simulink model "finalmodel1"  (R2024b)
(part 4 of 9)

ITS220Fyz2 | Innotech Solar ITS220Myz2 | Innotech Solar ITS220Nyz2 | Innotech Solar ITS215XXXX | Innotech Solar ITS220Eyz3 | Innotech Solar ITS220Fyz3 | Innotech Solar ITS220Myz3 | Innotech Solar ITS220Nyz3 | Innotech Solar x220 | Innotech Solar ITS225XXXX | Innotech Solar x225 | Innotech Solar ITS220Eyz4 | Innotech Solar ITS220Fyz4 | Innotech Solar ITS220Mxy4 | Innotech Solar ITS220Nxy4 | Innotech Solar ITS230XXXX | Innotech Solar x230 | Innotech Solar x235 | Innotech Solar x240 | Innotech Solar x245 | Innotech Solar ITS270Eyz1 | Innotech Solar ITS270Fyz1 | Innotech Solar ITS270Myz1 | Innotech Solar ITS270Nyz1 | Innotech Solar x250 | Innotech Solar x255 | Innotech Solar ITS270Eyz2 | Innotech Solar ITS270Fyz2 | Innotech Solar ITS270Myz2 | Innotech Solar ITS270Nyz2 | Innotech Solar x260 | Innotech Solar x265 | Innotech Solar ITS270Eyz3 | Innotech Solar ITS270Fyz3 | Innotech Solar ITS270Myz3 | Innotech Solar ITS270Nyz3 | Innovosolar International TEM165M | Innovosolar International TEM170M | Innovosolar International TEM175M | Innovosolar International TEM180M | Instalaciones Pevafersa IP-VA180 | Instalaciones Pevafersa IP-VAP210 | Instalaciones Pevafersa IP-220 GG | Instalaciones Pevafersa IP-225 GG | Instalaciones Pevafersa IP-230 GG | Instalaciones Pevafersa IP-VAP230 | Instalaciones Pevafersa IP-235 GG | Integrated Power IPC175M01 | Integrated Power IPC175M01-US | Integrated Power IPC175P01 | Integrated Power IPC175P01-US | Integrated Power IPC180M01 | Integrated Power IPC180M01-US | Integrated Power IPC180P01 | Integrated Power IPC180P01-US | Integrated Power IPC185M01 | Integrated Power IPC185M01-US | Integrated Power IPC185P01 | Integrated Power IPC185P01-US | Integrated Power IPC190P01 | Integrated Power IPC190P01-US | Integrated Power IPC200P01 | Integrated Power IPC200P01-US | Integrated Power IPC205P01 | Integrated Power IPC205P01-US | Integrated Power IPC210P01 | Integrated Power IPC210P01-US | Integrated Power IPC215P01 | Integrated Power IPC215P01-US | Integrated Power IPC220P01 | Integrated Power IPC220P01-US | Integrated Power IPC225P01 | Integrated Power IPC225P01-US | Integrated Power IPC230P01 | Integrated Power IPC230P01-US | Integrated Power IPC235P01 | Integrated Power IPC235P01-US | Integrated Power IPC240P01 | Integrated Power IPC240P01-US | Integrated Power IPC245P01 | Integrated Power IPC245P01-US | Integrated Power IPC250P01 | Integrated Power IPC250P01-US | Integrated Power IPC255P01 | Integrated Power IPC255P01-US | Integrated Power IPC260P01 | Integrated Power IPC260P01-US | Integrated Power IPC265P01 | Integrated Power IPC265P01-US | Integrated Power IPC270P01 | Integrated Power IPC270P01-US | Integrated Power IPC275P01 | Integrated Power IPC275P01-US | Integrated Power IPC280P01 | Integrated Power IPC280P01-US | Integrated Solar Technology STT-64M-B4U | Integrated Solar Technology STT-67M-B4U | Integrated Solar Technology STT-70M-B4U | Integrated Solar Technology STS-95M-B4U | Integrated Solar Technology STS-100M-B4U | Integrated Solar Technology STS-105M-B4U | Inventec Energy IECS-6P66-125 | Inventec Energy IECS-6M66-130 | Inventec Energy IECS-6P66-130 | Inventec Energy IECS-6M66-135 | Inventec Energy IECS-6P66-135 | Inventec Energy IECS-6M66-140 | Inventec Energy IECS-6P66-140 | Inventec Energy IECS-6M66-145 | Inventec Energy IECS-6P66-145 | Inventec Energy IECS-6P67-145 | Inventec Energy IECS-6M66-150 | Inventec Energy IECS-6M67-150 | Inventec Energy IECS-6P67-150 | Inventec Energy IECS-6M67-155 | Inventec Energy IECS-6P67-155 | Inventec Energy IECS-6M67-160 | Inventec Energy IECS-6P67-160 | Inventec Energy IECS-6M67-165 | Inventec Energy IECS-6P67-165 | Inventec Energy IECS-6P68-165 | Inventec Energy IECS-6M67-170 | Inventec Energy IECS-6M68-170 | Inventec Energy IECS-6P67-170 | Inventec Energy IECS-6P68-170 | Inventec Energy IECS-6M67-175 | Inventec Energy IECS-6M68-175 | Inventec Energy IECS-6P67-175 | Inventec Energy IECS-6P68-175 | Inventec Energy IECS-6M68-180 | Inventec Energy IECS-6M68-185 | Inventec Energy IECS-6P68-185 | Inventec Energy IECS-6M68-190 | Inventec Energy IECS-6P68-190 | Inventec Energy IECS-6P69-190 | Inventec Energy IECS-6M68-195 | Inventec Energy IECS-6P68-195 | Inventec Energy IECS-6P69-195 | Inventec Energy IECS-6M69-200 | Inventec Energy IECS-6P68-200 | Inventec Energy IECS-6P69-200 | Inventec Energy IECS-6M69-205 | Inventec Energy IECS-6P68-205 | Inventec Energy IECS-6P69-205 | Inventec Energy IECS-6M69-210 | Inventec Energy IECS-6P69-210 | Inventec Energy IECS-6P6A-210 | Inventec Energy IECS-6M6A-215 | Inventec Energy IECS-6P69-215 | Inventec Energy IECS-6P6A-215 | Inventec Energy IECS-6M6A-220 | Inventec Energy IECS-6P69-220 | Inventec Energy IECS-6P6A-220 | Inventec Energy IECS-6M6A-225 | Inventec Energy IECS-6P69-225 | Inventec Energy IECS-6P6A-225 | Inventec Energy IECS-6M6A-230 | Inventec Energy IECS-6P69-230 | Inventec Energy IECS-6P6A-230 | Inventec Energy IECS-6M6A-235 | Inventec Energy IECS-6P6A-235 | Inventec Energy IECS-6M6A-240 | Inventec Energy IECS-6P6A-240 | Inventec Energy IECS-6M6A-245 | Inventec Energy IECS-6P6A-245 | Inventec Energy IECS-6M6A-250 | Inventec Energy IECS-6P6A-250 | Inventec Energy IECS-6M6A-255 | Inventec Energy IECS-6P6A-255 | Inventec Energy IECS-6M6A-260 | Inventec Energy IECS-6M6A-265 | Inventec Energy IECS-6M6A-270 | Inventec Energy IECS-6M6A-275 | Inventec Energy IECS-6P6C-275 | Inventec Energy IECS-6P6C-280 | Inventec Energy IECS-6M6C-285 | Inventec Energy IECS-6P6C-285 | Inventec Energy IECS-6M6C-290 | Inventec Energy IECS-6P6C-290 | Inventec Energy IECS-6M6C-295 | Inventec Energy IECS-6P6C-295 | Inventec Energy IECS-6M6C-300 | Inventec Energy IECS-6P6C-300 | Inventec Energy IECS-6M6C-305 | Inventec Energy IECS-6M6C-310 | Inventec Energy IECS-6M6C-315 | Inventec Energy IECS-6M6C-320 | Inventec Energy IECS-6M6C-325 | Inventec Energy IECS-6M6C-330 | Isofoton IS-210/32 | Isofoton IS-215/32 | Isofoton IS-220/32 | Isofoton ISF-235 | Isofoton ISF-240 | Isofoton ISFP-240 Black | Isofoton ISFP-240 White | Isofoton ISF-245 | Isofoton ISF-245 Black | Isofoton ISF-245 Clear | Isofoton ISFP-245 Black | Isofoton ISFP-245 White | Isofoton ISFT-245 | Isofoton ISF-250 | Isofoton ISF-250 Black | Isofoton ISF-250 Clear | Isofoton ISFP-250 Black | Isofoton ISFP-250 White | Isofoton ISFT-250 | Isofoton ISF-255 | Isofoton ISF-255 Black | Isofoton ISF-255 Clear | Isofoton ISFP-255 Black | Isofoton ISFP-255 White | Isofoton ISFT-255 | Isofoton ISFP-260 Black | Isofoton ISFP-260 White | Isofoton ISFP-265 Black | Isofoton ISFP-265 White | Isofoton ISFP-270 Black | Isofoton ISFP-270 White | Itek Energy LLC iT-220 | Itek Energy LLC iT-225 | Itek Energy LLC iT-230 | Itek Energy LLC iT-235 | Itek Energy LLC iT-240 | Itek Energy LLC P18y250 | Itek Energy LLC S18y250 | Itek Energy LLC P18y255 | Itek Energy LLC S18y255 | Itek Energy LLC iT-260-HE | Itek Energy LLC P18y260 | Itek Energy LLC S18y260 | Itek Energy LLC iT-265-HE | Itek Energy LLC P18Y265 | Itek Energy LLC S18y265 | Itek Energy LLC iT-270-HE | Itek Energy LLC S19Y270 | Itek Energy LLC S79y270 | Itek Energy LLC iT-275-HE | Itek Energy LLC iT-275-SE | Itek Energy LLC P19Y275 | Itek Energy LLC S19y275 | Itek Energy LLC S79y275 | Itek Energy LLC iT-280-HE | Itek Energy LLC iT-280-SE | Itek Energy LLC S19y280 | Itek Energy LLC S59y280 | Itek Energy LLC S79y280 | Itek Energy LLC iT-285-HE | Itek Energy LLC iT-285-SE | Itek Energy LLC P19Y285 | Itek Energy LLC S19y285 | Itek Energy LLC S59y285 | Itek Energy LLC S79y285 | Itek Energy LLC iT-290-HE | Itek Energy LLC iT-290-SE | Itek Energy LLC P19Y290 | Itek Energy LLC S19y290 | Itek Energy LLC S59y290 | Itek Energy LLC S79Y290 | Itek Energy LLC iT-295-HE | Itek Energy LLC iT-295-SE | Itek Energy LLC P19Y295 | Itek Energy LLC S19Y295 | Itek Energy LLC S59Y295 | Itek Energy LLC S79Y295 | Itek Energy LLC iT-300-HE | Itek Energy LLC iT-300-SE | Itek Energy LLC P19Y300 | Itek Energy LLC S19Y300 | Itek Energy LLC S59Y300 | Itek Energy LLC S79Y300 | Itek Energy LLC iT-305-SE | Itek Energy LLC P19Y305 | Itek Energy LLC S19Y305 | Itek Energy LLC S59Y305 | Itek Energy LLC S79Y305 | Itek Energy LLC P19Y310 | Itek Energy LLC S19Y310 | Itek Energy LLC S59Y310 | Itek Energy LLC iT-335-SE-72 | Itek Energy LLC iT-340-SE-72 | Itek Energy LLC iT-345-SE-72 | Itek Energy LLC iT-350-SE-72 | Itek Energy LLC iT-355-SE-72 | Itek Energy LLC iT-360-SE-72 | Itek Energy LLC iT-365-SE-72 | Itek Energy LLC iT-370-SE-72 | Itek Energy LLC iT-375-SE-72 | JA Solar JAM5-72-165 | JA Solar JAM5-72-170 | JA Solar JAM5-72-175 | JA Solar JAM5(L)(BK)-72-180/SI | JA Solar JAM5(L)-72-180/SI | JA Solar JAM5-72-180 | JA Solar JAM5(L)(BK)-72-185/SI | JA Solar JAM5(L)-72-185/SI | JA Solar JAM5-72-185 | JA Solar JAM5(L)(BK)-72-190/SI | JA Solar JAM5(L)-72-190/SI | JA Solar JAM5-72-190 | JA Solar JAM5(L)(BK)-72-195/SI | JA Solar JAM5(L)-72-195/SI | JA Solar JAM5-72-195 | JA Solar JAM5(L)(BK)-72-200/SI | JA Solar JAM5(L)-72-200/SI | JA Solar JAM6-60-200 | JA Solar JAP6-60-200 | JA Solar JAM5(L)(BK)-72-205/SI | JA Solar JAM5(L)-72-205/SI | JA Solar JAM6-60-205 | JA Solar JAP6-60-205 | JA Solar JAM5(L)(BK)-72-210/SI | JA Solar JAM5(L)-72-210/SI | JA Solar JAM6-60-210 | JA Solar JAP6-60-210 | JA Solar JAM6-60-215 | JA Solar JAP6(BK)-60-215 | JA Solar JAM6-60-220 | JA Solar JAP6(BK)-60-220 | JA Solar JAM6-60-225 | JA Solar JAP6(BK)-60-225 | JA Solar JAP6-60-225/MP | JA Solar JAM6-60-230 | JA Solar JAP6(BK)-60-230 | JA Solar JAP6-60-230/MP | JA Solar JAM6-60-235 | JA Solar JAM6-60-235/SI | JA Solar JAP6(BK)-60-235 | JA Solar JAP6-60-235/MP | JA Solar JAM6-60-240 | JA Solar JAM6-60-240/SI | JA Solar JAP6(BK)-60-240 | JA Solar JAP6-60-240/MP | JA Solar JAM6-60-245/SI | JA Solar JAP6(BK)-60-245 | JA Solar JAP6-60-245 | JA Solar JAP6-60-245/3BB | JA Solar JAP6-60-245/MP | JA Solar JAM6-60-250/SI | JA Solar JAP6(BK)-60-250 | JA Solar JAP6-60-250 | JA Solar JAP6-60-250/3BB | JA Solar JAP6-60-250/MP | JA Solar JAP6-72-250 | JA Solar JAM6-60-255/SI | JA Solar JAM6-72-255 | JA Solar JAP6(k)-60-255/4BB | JA Solar JAP6-60-255/3BB | JA Solar JAP6-60-255/4BB | JA Solar JAP6-60-255/MP | JA Solar JAP6-72-255 | JA Solar JAM6-60-260/SI | JA Solar JAM6-72-260 | JA Solar JAP6(k)-60-260/4BB | JA Solar JAP6-60-260/3BB | JA Solar JAP6-60-260/4BB | JA Solar JAP6-60-260/4BB/RE | JA Solar JAP6-60-260/MP | JA Solar JAP6-72-260 | JA Solar JAM6(k)-60-265/4BB | JA Solar JAM6-60-265/SI | JA Solar JAM6-72-265 | JA Solar JAP6(BK)-72-265 | JA Solar JAP6(k)-60-265/4BB | JA Solar JAP6-60-265/3BB | JA Solar JAP6-60-265/4BB | JA Solar JAP6-60-265/4BB/RE | JA Solar JAM6(k)-60-270/4BB | JA Solar JAM6-60-270/SI | JA Solar JAM6-72-270 | JA Solar JAP6(BK)-72-270 | JA Solar JAP6(k)-60-270/4BB | JA Solar JAP6-60-270/3BB | JA Solar JAP6-60-270/4BB | JA Solar JAP6-60-270/4BB/RE | JA Solar JAM6(k)-60-275/4BB | JA Solar JAM6-60-275/SI | JA Solar JAM6-72-275 | JA Solar JAP6(BK)-72-275 | JA Solar JAP6(k)-60-275/4BB | JA Solar JAP6-60-275/3BB | JA Solar JAP6-60-275/4BB | JA Solar JAP6-60-275/4BB/RE | JA Solar JAP6-72-275/3BB | JA Solar JAM6(k)(BK)-60-280/PR | JA Solar JAM6(k)-60-280/4BB | JA Solar JAM6(k)-60-280/PR | JA Solar JAM60S01-280/PR | JA Solar JAM60S02-280/PR | JA Solar JAM6-60-280/SI | JA Solar JAM6-72-280 | JA Solar JAP6(BK)-72-280 | JA Solar JAP6(BK)-72-280/MP | JA Solar JAP6-60-280/4BB/RE | JA Solar JAP6-72-280/3BB | JA Solar JAP6-72-280/MP | JA Solar JAM6(BK)-72-285/SI | JA Solar JAM6(k)(BK)-60-285/PR | JA Solar JAM6(k)-60-285/4BB | JA Solar JAM6(k)-60-285/PR | JA Solar JAM60S01-285/PR | JA Solar JAM60S02-285/PR | JA Solar JAM6-72-285 | JA Solar JAM6-72-285/SI | JA Solar JAP6(BK)-72-285 | JA Solar JAP6(BK)-72-285/MP | JA Solar JAP6-72-285/3BB | JA Solar JAP6-72-285/MP | JA Solar JAM6(BK)-72-290/SI | JA Solar JAM6(k)(BK)-60-290/PR | JA Solar JAM6(k)-60-290/PR | JA Solar JAM60S01-290/PR | JA Solar JAM60S02-290/PR | JA Solar JAM6-72-290 | JA Solar JAM6-72-290/SI | JA Solar JAP6(BK)-72-290 | JA Solar JAP6(BK)-72-290/MP | JA Solar JAP6-72-290/3BB | JA Solar JAP6-72-290/MP | JA Solar JAM6(BK)-72-295/SI | JA Solar JAM6(k)(BK)-60-295/PR | JA Solar JAM6(k)-60-295/PR | JA Solar JAM60S01-295/PR | JA Solar JAM6-72-295 | JA Solar JAM6-72-295/SI | JA Solar JAP6(BK)-72-295 | JA Solar JAP6(BK)-72-295/MP | JA Solar JAP6-72-295 | JA Solar JAP6-72-295/3BB | JA Solar JAP6-72-295/MP | JA Solar JAM6(BK)-72-300/SI | JA Solar JAM6(k)(BK)-60-300/PR | JA Solar JAM6(k)-60-300/PR | JA Solar JAM60S01-300/PR | JA Solar JAM60S02-300/PR | JA Solar JAM6-72-300 | JA Solar JAM6-72-300/SI | JA Solar JAP6(BK)-72-300 | JA Solar JAP6(BK)-72-300/MP | JA Solar JAP6-72-300 | JA Solar JAP6-72-300/3BB | JA Solar JAP6-72-300/MP | JA Solar JAM6(BK)-72-305/SI | JA Solar JAM60S01-305/PR | JA Solar JAM6-72-305/SI | JA Solar JAP6(BK)-72-305/MP | JA Solar JAP6(k)-72-305/4BB | JA Solar JAP6-72-305 | JA Solar JAP6-72-305/3BB | JA Solar JAP6-72-305/4BB | JA Solar JAP6-72-305/4BB/RE | JA Solar JAP6-72-305/MP | JA Solar JAP72S01-305/SC | JA Solar JAM6(BK)-72-310/SI | JA Solar JAM6-72-310/SI | JA Solar JAP6(BK)-72-310/MP | JA Solar JAP6(k)-72-310/4BB | JA Solar JAP6-72-310 | JA Solar JAP6-72-310/3BB | JA Solar JAP6-72-310/4BB | JA Solar JAP6-72-310/4BB/RE | JA Solar JAP6-72-310/MP | JA Solar JAP72S01-310/SC | JA Solar JAM6(BK)-72-315/SI | JA Solar JAM6-72-315/SI | JA Solar JAP6(BK)-72-315/MP | JA Solar JAP6(k)-72-315/4BB | JA Solar JAP6-72-315 | JA Solar JAP6-72-315/3BB | JA Solar JAP6-72-315/4BB | JA Solar JAP6-72-315/4BB/RE | JA Solar JAP6-72-315/MP | JA Solar JAP72S01-315/SC | JA Solar JAM6(k)-72-320/4BB | JA Solar JAM6-72-320/SI | JA Solar JAP6(k)-72-320/4BB | JA Solar JAP6-72-320/3BB | JA Solar JAP6-72-320/4BB | JA Solar JAP6-72-320/4BB/RE | JA Solar JAP72S01-320/SC | JA Solar JAM6(k)-72-325/4BB | JA Solar JAM6-72-325/SI | JA Solar JAP6(k)-72-325/4BB | JA Solar JAP6-72-325/3BB | JA Solar JAP6-72-325/4BB | JA Solar JAP6-72-325/4BB/RE | JA Solar JAP72S01-325/SC | JA Solar JAM6(k)-72-330/4BB | JA Solar JAM6(k)-72-330/PR | JA Solar JAM6-72-330/SI | JA Solar JAP6-72-330/3BB | JA Solar JAP6-72-330/4BB | JA Solar JAP6-72-330/4BB/RE | JA Solar JAP72S01-330/SC | JA Solar JAM6(k)-72-335/4BB | JA Solar JAM6(k)-72-335/PR | JA Solar JAM6-72-335/SI | JA Solar JAM72S01-335/PR | JA Solar JAP6-72-335/4BB/RE | JA Solar JAM6(k)-72-340/4BB | JA Solar JAM6(k)-72-340/PR | JA Solar JAM72S01-340/PR | JA Solar JAM6(k)-72-345/PR | JA Solar JAM72S01-345/PR | JA Solar JAM6(k)-72-350/PR | JA Solar JAM72S01-350/PR | JA Solar JAM6(k)-72-355/PR | JA Solar JAM72S01-355/PR | JA Solar JAM6(k)-72-360/PR | JA Solar JAM72S01-360/PR | JA Solar JAM72S01-365/PR | Japan Solar (Infini Co._ Ltd) JS-170M-TCI72 | Japan Solar (Infini Co._ Ltd) JS-175M-CI72 | Japan Solar (Infini Co._ Ltd) JS-175M-TCI72 | Japan Solar (Infini Co._ Ltd) JS-180M-CI72 | Japan Solar (Infini Co._ Ltd) JS-180M-TCI72 | Japan Solar (Infini Co._ Ltd) JS-185M-CI72 | Japan Solar (Infini Co._ Ltd) JS-185M-TCI72 | Japan Solar (Infini Co._ Ltd) JS-190M-CI72 | Japan Solar (Infini Co._ Ltd) JS-190M-TCI72 | Japan Solar (Infini Co._ Ltd) JS-215M-CI54 | Japan Solar (Infini Co._ Ltd) JS-215M-CI54-BB | Japan Solar (Infini Co._ Ltd) JS-215M-TCI54 | Japan Solar (Infini Co._ Ltd) JS-215M-TCI54-BB | Japan Solar (Infini Co._ Ltd) JS-220M-CI54 | Japan Solar (Infini Co._ Ltd) JS-220M-CI54-BB | Japan Solar (Infini Co._ Ltd) JS-220M-CI60 | Japan Solar (Infini Co._ Ltd) JS-220M-TCI54 | Japan Solar (Infini Co._ Ltd) JS-220M-TCI54-BB | Japan Solar (Infini Co._ Ltd) JS-220M-TCI60 | Japan Solar (Infini Co._ Ltd) JS-220U-CI60 | Japan Solar (Infini Co._ Ltd) JS-220U-TCI60 | Japan Solar (Infini Co._ Ltd) JS-225M-CI54 | Japan Solar (Infini Co._ Ltd) JS-225M-CI54-BB | Japan Solar (Infini Co._ Ltd) JS-225M-CI60 | Japan Solar (Infini Co._ Ltd) JS-225M-TCI54 | Japan Solar (Infini Co._ Ltd) JS-225M-TCI54-BB | Japan Solar (Infini Co._ Ltd) JS-225M-TCI60 | Japan Solar (Infini Co._ Ltd) JS-225U-CI60 | Japan Solar (Infini Co._ Ltd) JS-225U-TCI60 | Japan Solar (Infini Co._ Ltd) JS-230M-CI60 | Japan Solar (Infini Co._ Ltd) JS-230M-TCI60 | Japan Solar (Infini Co._ Ltd) JS-230U-CI60 | Japan Solar (Infini Co._ Ltd) JS-230U-TCI60 | Japan Solar (Infini Co._ Ltd) JS-235M-CI60 | Japan Solar (Infini Co._ Ltd) JS-235M-CI60-BB | Japan Solar (Infini Co._ Ltd) JS-235M-TCI60 | Japan Solar (Infini Co._ Ltd) JS-235M-TCI60-BB | Japan Solar (Infini Co._ Ltd) JS-235U-CI60 | Japan Solar (Infini Co._ Ltd) JS-235U-CI60-BW | Japan Solar (Infini Co._ Ltd) JS-235U-TCI60-BW | Japan Solar (Infini Co._ Ltd) JS-240M-CI54 | Japan Solar (Infini Co._ Ltd) JS-240M-CI60 | Japan Solar (Infini Co._ Ltd) JS-240M-CI60-BB | Japan Solar (Infini Co._ Ltd) JS-240M-TCI54 | Japan Solar (Infini Co._ Ltd) JS-240M-TCI60 | Japan Solar (Infini Co._ Ltd) JS-240M-TCI60-BB | Japan Solar (Infini Co._ Ltd) JS-240U-CI60 | Japan Solar (Infini Co._ Ltd) JS-240U-CI60-BW | Japan Solar (Infini Co._ Ltd) JS-240U-TCI60 | Japan Solar (Infini Co._ Ltd) JS-240U-TCI60-BW | Japan Solar (Infini Co._ Ltd) JS-245M-CI60 | Japan Solar (Infini Co._ Ltd) JS-245M-CI60-BB | Japan Solar (Infini Co._ Ltd) JS-245M-CI60-BW | Japan Solar (Infini Co._ Ltd) JS-245M-TCI60 | Japan Solar (Infini Co._ Ltd) JS-245M-TCI60-BB | Japan Solar (Infini Co._ Ltd) JS-245M-TCI60-BW | Japan Solar (Infini Co._ Ltd) JS-245M-TCI72 | Japan Solar (Infini Co._ Ltd) JS-245U-CI60 | Japan Solar (Infini Co._ Ltd) JS-245U-CI60-BW | Japan Solar (Infini Co._ Ltd) JS-245U-TCI60 | Japan Solar (Infini Co._ Ltd) JS-245U-TCI60-BW | Japan Solar (Infini Co._ Ltd) JS-250M-CI60 | Japan Solar (Infini Co._ Ltd) JS-250M-CI60-BW | Japan Solar (Infini Co._ Ltd) JS-250M-TCI60 | Japan Solar (Infini Co._ Ltd) JS-250M-TCI60-BB | Japan Solar (Infini Co._ Ltd) JS-250M-TCI72 | Japan Solar (Infini Co._ Ltd) JS-250U-CI60 | Japan Solar (Infini Co._ Ltd) JS-250U-CI60-BW | Japan Solar (Infini Co._ Ltd) JS-250U-LI60 | Japan Solar (Infini Co._ Ltd) JS-250U-PI60 | Japan Solar (Infini Co._ Ltd) JS-250U-TCI60 | Japan Solar (Infini Co._ Ltd) JS-250U-TCI60-BW | Japan Solar (Infini Co._ Ltd) JS-255M-CI60 | Japan Solar (Infini Co._ Ltd) JS-255M-CI60-BW | Japan Solar (Infini Co._ Ltd) JS-255M-LI60 | Japan Solar (Infini Co._ Ltd) JS-255M-TCI60 | Japan Solar (Infini Co._ Ltd) JS-255M-TCI60-BB | Japan Solar (Infini Co._ Ltd) JS-255U-CI60 | Japan Solar (Infini Co._ Ltd) JS-255U-CI60-BW | Japan Solar (Infini Co._ Ltd) JS-255U-LI60 | Japan Solar (Infini Co._ Ltd) JS-255U-PI60 | Japan Solar (Infini Co._ Ltd) JS-255U-RI60 | Japan Solar (Infini Co._ Ltd) JS-255U-RJI60 | Japan Solar (Infini Co._ Ltd) JS-255U-TCI60 | Japan Solar (Infini Co._ Ltd) JS-255U-TCI60-BW | Japan Solar (Infini Co._ Ltd) JS-260M-CI60 | Japan Solar (Infini Co._ Ltd) JS-260M-CI60-BW | Japan Solar (Infini Co._ Ltd) JS-260M-LI60 | Japan Solar (Infini Co._ Ltd) JS-260M-PI60 | Japan Solar (Infini Co._ Ltd) JS-260M-TCI60 | Japan Solar (Infini Co._ Ltd) JS-260M-TCI60-BB | Japan Solar (Infini Co._ Ltd) JS-260U-CI60 | Japan Solar (Infini Co._ Ltd) JS-260U-LI60 | Japan Solar (Infini Co._ Ltd) JS-260U-PI60 | Japan Solar (Infini Co._ Ltd) JS-260U-RI60 | Japan Solar (Infini Co._ Ltd) JS-260U-RJI60 | Japan Solar (Infini Co._ Ltd) JS-260U-TCI60 | Japan Solar (Infini Co._ Ltd) JS-265M-CI60 | Japan Solar (Infini Co._ Ltd) JS-265M-CI60-BW | Japan Solar (Infini Co._ Ltd) JS-265M-CI72 | Japan Solar (Infini Co._ Ltd) JS-265M-LI60 | Japan Solar (Infini Co._ Ltd) JS-265M-PI60 | Japan Solar (Infini Co._ Ltd) JS-265M-TCI60 | Japan Solar (Infini Co._ Ltd) JS-265M-TCI60-BB | Japan Solar (Infini Co._ Ltd) JS-265M-TCI72 | Japan Solar (Infini Co._ Ltd) JS-265U-LI60 | Japan Solar (Infini Co._ Ltd) JS-265U-PI60 | Japan Solar (Infini Co._ Ltd) JPS-270P-60-A | Japan Solar (Infini Co._ Ltd) JS-270M-CI60 | Japan Solar (Infini Co._ Ltd) JS-270M-CI72 | Japan Solar (Infini Co._ Ltd) JS-270M-LI60 | Japan Solar (Infini Co._ Ltd) JS-270M-PI60 | Japan Solar (Infini Co._ Ltd) JS-270M-TCI60 | Japan Solar (Infini Co._ Ltd) JS-270M-TCI72 | Japan Solar (Infini Co._ Ltd) JS-270U-LI60 | Japan Solar (Infini Co._ Ltd) JS-270U-PI60 | Japan Solar (Infini Co._ Ltd) JPS-275P-60-A | Japan Solar (Infini Co._ Ltd) JS-275M-CI60 | Japan Solar (Infini Co._ Ltd) JS-275M-CI72 | Japan Solar (Infini Co._ Ltd) JS-275M-LI60 | Japan Solar (Infini Co._ Ltd) JS-275M-PI60 | Japan Solar (Infini Co._ Ltd) JS-275M-TCI60 | Japan Solar (Infini Co._ Ltd) JS-275M-TCI72 | Japan Solar (Infini Co._ Ltd) JS-275U-CI72 | Japan Solar (Infini Co._ Ltd) JS-275U-PI60 | Japan Solar (Infini Co._ Ltd) JS-275U-TCI72 | Japan Solar (Infini Co._ Ltd) JS-280M-60-BB | Japan Solar (Infini Co._ Ltd) JS-280M-CI60 | Japan Solar (Infini Co._ Ltd) JS-280M-CI72 | Japan Solar (Infini Co._ Ltd) JS-280M-CI72-BB | Japan Solar (Infini Co._ Ltd) JS-280M-LI60 | Japan Solar (Infini Co._ Ltd) JS-280M-PI60 | Japan Solar (Infini Co._ Ltd) JS-280M-TCI60 | Japan Solar (Infini Co._ Ltd) JS-280M-TCI72 | Japan Solar (Infini Co._ Ltd) JS-280M-TCI72-BB | Japan Solar (Infini Co._ Ltd) JS-280U-CI72 | Japan Solar (Infini Co._ Ltd) JS-280U-PI60 | Japan Solar (Infini Co._ Ltd) JS-280U-TCI72 | Japan Solar (Infini Co._ Ltd) JS-285M-60 | Japan Solar (Infini Co._ Ltd) JS-285M-60-BB | Japan Solar (Infini Co._ Ltd) JS-285M-CI72 | Japan Solar (Infini Co._ Ltd) JS-285M-CI72-BB | Japan Solar (Infini Co._ Ltd) JS-285M-LI60 | Japan Solar (Infini Co._ Ltd) JS-285M-PI60 | Japan Solar (Infini Co._ Ltd) JS-285M-TCI72 | Japan Solar (Infini Co._ Ltd) JS-285M-TCI72-BB | Japan Solar (Infini Co._ Ltd) JS-285U-CI72 | Japan Solar (Infini Co._ Ltd) JS-285U-PI60 | Japan Solar (Infini Co._ Ltd) JS-285U-TCI72 | Japan Solar (Infini Co._ Ltd) JS-290M-60 | Japan Solar (Infini Co._ Ltd) JS-290M-60-BB | Japan Solar (Infini Co._ Ltd) JS-290M-CI72 | Japan Solar (Infini Co._ Ltd) JS-290M-CI72-BB | Japan Solar (Infini Co._ Ltd) JS-290M-PI60 | Japan Solar (Infini Co._ Ltd) JS-290M-TCI72 | Japan Solar (Infini Co._ Ltd) JS-290M-TCI72-BB | Japan Solar (Infini Co._ Ltd) JS-290U-CI72 | Japan Solar (Infini Co._ Ltd) JS-290U-TCI72 | Japan Solar (Infini Co._ Ltd) JS-295M-60 | Japan Solar (Infini Co._ Ltd) JS-295M-60-BB | Japan Solar (Infini Co._ Ltd) JS-295M-CI72 | Japan Solar (Infini Co._ Ltd) JS-295M-CI72-BB | Japan Solar (Infini Co._ Ltd) JS-295M-PI60 | Japan Solar (Infini Co._ Ltd) JS-295M-TCI72 | Japan Solar (Infini Co._ Ltd) JS-295M-TCI72-BB | Japan Solar (Infini Co._ Ltd) JS-295U-PI72 | Japan Solar (Infini Co._ Ltd) JS-295U-TCI72 | Japan Solar (Infini Co._ Ltd) JPS-300M-60-A | Japan Solar (Infini Co._ Ltd) JPS-300M-60-A-BB | Japan Solar (Infini Co._ Ltd) JS-300M-60 | Japan Solar (Infini Co._ Ltd) JS-300M-CI72 | Japan Solar (Infini Co._ Ltd) JS-300M-TCI72 | Japan Solar (Infini Co._ Ltd) JS-300U-LI72 | Japan Solar (Infini Co._ Ltd) JS-300U-PI72 | Japan Solar (Infini Co._ Ltd) JS-300U-RI72 | Japan Solar (Infini Co._ Ltd) JS-300U-TCI72 | Japan Solar (Infini Co._ Ltd) JS-305M-CI72 | Japan Solar (Infini Co._ Ltd) JS-305M-TCI72 | Japan Solar (Infini Co._ Ltd) JS-305U-LI72 | Japan Solar (Infini Co._ Ltd) JS-305U-PI72 | Japan Solar (Infini Co._ Ltd) JS-305U-RI72 | Japan Solar (Infini Co._ Ltd) JS-305U-TCI72 | Japan Solar (Infini Co._ Ltd) JS-310M-CI72 | Japan Solar (Infini Co._ Ltd) JS-310M-LI72 | Japan Solar (Infini Co._ Ltd) JS-310M-TCI72 | Japan Solar (Infini Co._ Ltd) JS-310U-LI72 | Japan Solar (Infini Co._ Ltd) JS-310U-PI72 | Japan Solar (Infini Co._ Ltd) JS-310U-RI72 | Japan Solar (Infini Co._ Ltd) JS-310U-TCI72 | Japan Solar (Infini Co._ Ltd) JS-315M-CI72 | Japan Solar (Infini Co._ Ltd) JS-315M-LI72 | Japan Solar (Infini Co._ Ltd) JS-315M-PI72 | Japan Solar (Infini Co._ Ltd) JS-315M-TCI72 | Japan Solar (Infini Co._ Ltd) JS-315U-LI72 | Japan Solar (Infini Co._ Ltd) JS-315U-PI72 | Japan Solar (Infini Co._ Ltd) JS-315U-RI72 | Japan Solar (Infini Co._ Ltd) JS-315U-TCI72 | Japan Solar (Infini Co._ Ltd) JS-320M-CI72 | Japan Solar (Infini Co._ Ltd) JS-320M-LI72 | Japan Solar (Infini Co._ Ltd) JS-320M-PI72 | Japan Solar (Infini Co._ Ltd) JS-320M-TCI72 | Japan Solar (Infini Co._ Ltd) JS-320U-LI72 | Japan Solar (Infini Co._ Ltd) JS-320U-PI72 | Japan Solar (Infini Co._ Ltd) JS-325M-CI72 | Japan Solar (Infini Co._ Ltd) JS-325M-LI72 | Japan Solar (Infini Co._ Ltd) JS-325M-PI72 | Japan Solar (Infini Co._ Ltd) JS-325M-TCI72 | Japan Solar (Infini Co._ Ltd) JS-325U-LI72 | Japan Solar (Infini Co._ Ltd) JS-325U-PI72 | Japan Solar (Infini Co._ Ltd) JS-330M-CI72 | Japan Solar (Infini Co._ Ltd) JS-330M-LI72 | Japan Solar (Infini Co._ Ltd) JS-330M-PI72 | Japan Solar (Infini Co._ Ltd) JS-330M-TCI72 | Japan Solar (Infini Co._ Ltd) JS-330U-PI72 | Japan Solar (Infini Co._ Ltd) JS-335M-LI72 | Japan Solar (Infini Co._ Ltd) JS-335M-PI72 | Japan Solar (Infini Co._ Ltd) JS-335U-PI72 | Japan Solar (Infini Co._ Ltd) JS-340M-PI72 | Japan Solar (Infini Co._ Ltd) JS-340U-PI72 | Japan Solar (Infini Co._ Ltd) JS-345M-PI72 | Japan Solar (Infini Co._ Ltd) JS-350M-PI72 | Japan Solar (Infini Co._ Ltd) JPS-355M-72-A | Japan Solar (Infini Co._ Ltd) JS-355M-PI72 | Japan Solar (Infini Co._ Ltd) JPS-360M-72-A | Japan Solar (Infini Co._ Ltd) JS-360M-PI72 | Japan Solar Factory JB250P-60 | Japan Solar Factory JB255P-60 | Japan Solar Factory JB260M-60 | Japan Solar Factory JB260P-60 | Japan Solar Factory JB265M-60 | Japan Solar Factory JB265P-60 | Japan Solar Factory JB270M-60 | Japan Solar Factory JB270P-60 | Japan Solar Factory JB275M-60 | Japan Solar Factory JB280M-60 | Japan Solar Factory JB300P-72 | Japan Solar Factory JB305P-72 | Japan Solar Factory JB310M-72 | Japan Solar Factory JB310P-72 | Japan Solar Factory JB315M-72 | Japan Solar Factory JB315P-72 | Japan Solar Factory JB320M-72 | Japan Solar Factory JB320P-72 | Japan Solar Factory JB325M-72 | Japan Solar Factory JB325P-72 | Japan Solar Factory JB330M-72 | Japan Solar Factory JB335M-72 | Jetion Science & Technology Co JT250PLg | Jetion Science & Technology Co JT255PLg | Jetion Science & Technology Co JT260PLg | Jetion Science & Technology Co JT265PLg | Jetion Science & Technology Co JT270PLg | Jetion Science & Technology Co JT300PMg | Jetion Science & Technology Co JT305PMg | Jetion Science & Technology Co JT310PMg | Jetion Science & Technology Co JT315PMg | Jetion Science & Technology Co JT320PMg | Jetion Solar (China) JT175SAb | Jetion Solar (China) JT175SAb(Black) | Jetion Solar (China) JT180SAb | Jetion Solar (China) JT180SAb(Black) | Jetion Solar (China) JT185SAb | Jetion Solar (China) JT185SAb(Black) | Jetion Solar (China) JT190SAb | Jetion Solar (China) JT195SAb | Jetion Solar (China) JT220PCe | Jetion Solar (China) JT220PCe(Black) | Jetion Solar (China) JT225PCe | Jetion Solar (China) JT225PCe(Black) | Jetion Solar (China) JT230PCe | Jetion Solar (China) JT230PCe(Black) | Jetion Solar (China) JT230SCc | Jetion Solar (China) JT230SCc(Black) | Jetion Solar (China) JT235PCe | Jetion Solar (China) JT235PCe(Black) | Jetion Solar (China) JT235SCc | Jetion Solar (China) JT235SCc(Black) | Jetion Solar (China) JT240PCe | Jetion Solar (China) JT240PCe(Black) | Jetion Solar (China) JT240SCc | Jetion Solar (China) JT240SCc(Black) | Jetion Solar (China) JT245SCc | Jetion Solar (China) JT245SCc(Black) | Jetion Solar (China) JT250PPg | Jetion Solar (China) JT250SCc | Jetion Solar (China) JT255PPg | Jetion Solar (China) JT260PPg | Jetion Solar (China) JT265PPg | Jetion Solar (China) JT270PAe | Jetion Solar (China) JT270PAe(Black) | Jetion Solar (China) JT270PPg | Jetion Solar (China) JT270SAc | Jetion Solar (China) JT270SAc(Black) | Jetion Solar (China) JT275PAe | Jetion Solar (China) JT275PAe(Black) | Jetion Solar (China) JT275SAc | Jetion Solar (China) JT275SAc(Black) | Jetion Solar (China) JT280PAe | Jetion Solar (China) JT280PAe(Black) | Jetion Solar (China) JT280SAc | Jetion Solar (China) JT280SAc(Black) | Jetion Solar (China) JT285PAe | Jetion Solar (China) JT285PAe(Black) | Jetion Solar (China) JT285SAc | Jetion Solar (China) JT285SAc(Black) | Jetion Solar (China) JT290PAe | Jetion Solar (China) JT290PAe(Black) | Jetion Solar (China) JT290SAc | Jetion Solar (China) JT290SAc(Black) | Jetion Solar (China) JT300PAg | Jetion Solar (China) JT305PAg | Jetion Solar (China) JT310PAg | Jetion Solar (China) JT315PAg | Jetion Solar (China) JT320PAg | Jiangsu Aide Solar Energy Technology AD160M5-Aa | Jiangsu Aide Solar Energy Technology AD165M5-Aa | Jiangsu Aide Solar Energy Technology AD170M5-Aa | Jiangsu Aide Solar Energy Technology AD175M5-Aa | Jiangsu Aide Solar Energy Technology AD180M5-Aa | Jiangsu Aide Solar Energy Technology AD185M5-Aa | Jiangsu Aide Solar Energy Technology AD190M5-Aa | Jiangsu Aide Solar Energy Technology AD190P6-Ac | Jiangsu Aide Solar Energy Technology AD195M5-Aa | Jiangsu Aide Solar Energy Technology AD195P6-Ac | Jiangsu Aide Solar Energy Technology AD200M5-Aa | Jiangsu Aide Solar Energy Technology AD200P6-Ac | Jiangsu Aide Solar Energy Technology AD205P6-Ac | Jiangsu Aide Solar Energy Technology AD210P6-Ac | Jiangsu Aide Solar Energy Technology AD210P6-Bc | Jiangsu Aide Solar Energy Technology AD215P6-Ab | Jiangsu Aide Solar Energy Technology AD220P6-Ab | Jiangsu Aide Solar Energy Technology AD220P6-Bb | Jiangsu Aide Solar Energy Technology AD225P6-Ab | Jiangsu Aide Solar Energy Technology AD230M6-Ab | Jiangsu Aide Solar Energy Technology AD230P6-Ab | Jiangsu Aide Solar Energy Technology AD230P6-Bb | Jiangsu Aide Solar Energy Technology AD235M6-Ab | Jiangsu Aide Solar Energy Technology AD235P6-Ab | Jiangsu Aide Solar Energy Technology AD235P6-Bb | Jiangsu Aide Solar Energy Technology AD240M6-Ab | Jiangsu Aide Solar Energy Technology AD240P6-Ab | Jiangsu Aide Solar Energy Technology AD240P6-Bb | Jiangsu Aide Solar Energy Technology AD245M6-Ab | Jiangsu Aide Solar Energy Technology AD245P6-Ab | Jiangsu Aide Solar Energy Technology AD250M6-Ab | Jiangsu Aide Solar Energy Technology AD250P6-Ab | Jiangsu Aide Solar Energy Technology AD255M6-Ab | Jiangsu Aide Solar Energy Technology AD255P6-Ab | Jiangsu Aide Solar Energy Technology AD260M6-Ab | Jiangsu Aide Solar Energy Technology AD260P6-Ab | Jiangsu Aide Solar Energy Technology AD265M6-Ab | Jiangsu Aide Solar Energy Technology AD275M6-Aa | Jiangsu Aide Solar Energy Technology AD275P6-Aa | Jiangsu Aide Solar Energy Technology AD280M6-Aa | Jiangsu Aide Solar Energy Technology AD280P6-Aa | Jiangsu Aide Solar Energy Technology AD285M6-Aa | Jiangsu Aide Solar Energy Technology AD285P6-Aa | Jiangsu Aide Solar Energy Technology AD290M6-Aa | Jiangsu Aide Solar Energy Technology AD290P6-Aa | Jiangsu Aide Solar Energy Technology AD295M6-Aa | Jiangsu Aide Solar Energy Technology AD295P6-Aa | Jiangsu Aide Solar Energy Technology AD300M6-Aa | Jiangsu Aide Solar Energy Technology AD300P6-Aa | Jiangsu Aide Solar Energy Technology AD305M6-Aa | Jiangsu Aide Solar Energy Technology AD305P6-Aa | Jiangsu Aide Solar Energy Technology AD310M6-Aa | Jiangsu Aide Solar Energy Technology AD310P6-Aa | Jiangsu Aide Solar Energy Technology AD315M6-Aa | Jiangsu Best Solar High-Tech BEST-170D-24 | Jiangsu Best Solar High-Tech BEST-175D-24 | Jiangsu Best Solar High-Tech BEST-180D-24 | Jiangsu Best Solar High-Tech BEST-190P-18 | Jiangsu Best Solar High-Tech BEST-200P-18 | Jiangsu Best Solar High-Tech BEST-210P-18 | Jiangsu Best Solar High-Tech BEST-210P-20 | Jiangsu Best Solar High-Tech BEST-220D-20 | Jiangsu Best Solar High-Tech BEST-220P-20 | Jiangsu Best Solar High-Tech BEST-230P-20 | Jiangsu Best Solar High-Tech BEST-260P-24 | Jiangsu Best Solar High-Tech BEST-270P-24 | Jiangsu Best Solar High-Tech BEST-280P-24 | Jiangsu Green Power PV GPM175-A-72 | Jiangsu Green Power PV GPM175-B-48 | Jiangsu Green Power PV GPM175P-B-48 | Jiangsu Green Power PV GPM180-A-72 | Jiangsu Green Power PV GPM180-B-48 | Jiangsu Green Power PV GPM180P-B-48 | Jiangsu Green Power PV GPM185-A-72 | Jiangsu Green Power PV GPM185-B-48 | Jiangsu Green Power PV GPM185P-B-48 | Jiangsu Green Power PV GPM190-B-54 | Jiangsu Green Power PV GPM190P-B-54 | Jiangsu Green Power PV GPM195-B-54 | Jiangsu Green Power PV GPM195P-B-54 | Jiangsu Green Power PV GPM200-B-54 | Jiangsu Green Power PV GPM200P-B-54 | Jiangsu Green Power PV GPM205-B-54 | Jiangsu Green Power PV GPM205P-B-54 | Jiangsu Green Power PV GPM210-B-54 | Jiangsu Green Power PV GPM210P-B-54 | Jiangsu Green Power PV GPM210P-B-60 | Jiangsu Green Power PV GPM215P-B-60 | Jiangsu Green Power PV GPM220-B-60 | Jiangsu Green Power PV GPM220P-B-60 | Jiangsu Green Power PV GPM225-B-60 | Jiangsu Green Power PV GPM225P-B-60 | Jiangsu Green Power PV GPM230-B-60 | Jiangsu Green Power PV GPM230P-B-60 | Jiangsu Green Power PV GPM235-B-60 | Jiangsu Green Power PV GPM240-B-60 | Jiangsu JiaSheng Photovoltaic Technology JS140M36-12V | Jiangsu JiaSheng Photovoltaic Technology JS140P36-12V | Jiangsu JiaSheng Photovoltaic Technology JS145M36-12V | Jiangsu JiaSheng Photovoltaic Technology JS145P36-12V | Jiangsu JiaSheng Photovoltaic Technology JS180D72-24V | Jiangsu JiaSheng Photovoltaic Technology JS185D72-24V | Jiangsu JiaSheng Photovoltaic Technology JS190D72-24V | Jiangsu JiaSheng Photovoltaic Technology JS195D72-24V | Jiangsu JiaSheng Photovoltaic Technology JS220P60-24V | Jiangsu JiaSheng Photovoltaic Technology JS225P60-24V | Jiangsu JiaSheng Photovoltaic Technology JS230M60-24V | Jiangsu JiaSheng Photovoltaic Technology JS230P60-24V | Jiangsu JiaSheng Photovoltaic Technology JS235M60-24V | Jiangsu JiaSheng Photovoltaic Technology JS235P60-24V | Jiangsu JiaSheng Photovoltaic Technology JS240M60-24V | Jiangsu JiaSheng Photovoltaic Technology JS240P60-24V | Jiangsu JiaSheng Photovoltaic Technology JS245M60-24V | Jiangsu JiaSheng Photovoltaic Technology JS250M60-24V | Jiangsu JiaSheng Photovoltaic Technology JS255M60-24V | Jiangsu JiaSheng Photovoltaic Technology JS255P72-24V | Jiangsu JiaSheng Photovoltaic Technology JS260M60-24V | Jiangsu JiaSheng Photovoltaic Technology JS260M72-24V | Jiangsu JiaSheng Photovoltaic Technology JS260P72-24V | Jiangsu JiaSheng Photovoltaic Technology JS265M72-24V | Jiangsu JiaSheng Photovoltaic Technology JS265P72-24V | Jiangsu JiaSheng Photovoltaic Technology JS270M72-24V | Jiangsu JiaSheng Photovoltaic Technology JS270P72-24V | Jiangsu JiaSheng Photovoltaic Technology JS275M72-24V | Jiangsu JiaSheng Photovoltaic Technology JS275P72-24V | Jiangsu JiaSheng Photovoltaic Technology JS280M72-24V | Jiangsu JiaSheng Photovoltaic Technology JS280P72-24V | Jiangsu JiaSheng Photovoltaic Technology JS290M72-24V | Jiangsu JiaSheng Photovoltaic Technology JS290P72-24V | Jiangsu JiaSheng Photovoltaic Technology JS300M72-24V | Jiangsu JiaSheng Photovoltaic Technology JS300P72-24V | Jiangsu Prefersolar Photovoltaic PS-175M | Jiangsu Prefersolar Photovoltaic PS-180M | Jiangsu Prefersolar Photovoltaic PS-185M | Jiangsu Prefersolar Photovoltaic PS-230M | Jiangsu Prefersolar Photovoltaic PS-235M | Jiangsu Prefersolar Photovoltaic PS-240M | Jiangsu Prefersolar Photovoltaic PS-245M | Jiangsu Prefersolar Photovoltaic PS-250M | Jiangsu Runda PV RS185M-72 | Jiangsu Runda PV RS190M-72 | Jiangsu Runda PV RS215P-60 | Jiangsu Runda PV RS220P-60 | Jiangsu Runda PV RS225P-60 | Jiangsu Runda PV RS230M-96 | Jiangsu Runda PV RS230P-60 | Jiangsu Runda PV RS235M-96 | Jiangsu Runda PV RS235P-60 | Jiangsu Runda PV RS240M-96 | Jiangsu Runda PV RS245M-96 | Jiangsu Runda PV RS250M-96 | Jiangsu Sainty Machinery GES-M165 | Jiangsu Sainty Machinery GES-5M170 | Jiangsu Sainty Machinery GES-M170 | Jiangsu Sainty Machinery GES-5M175 | Jiangsu Sainty Machinery GES-M175 | Jiangsu Sainty Machinery GES-5M180 | Jiangsu Sainty Machinery GES-M180 | Jiangsu Sainty Machinery GES-5M185 | Jiangsu Sainty Machinery GES-5M190 | Jiangsu Sainty Machinery GES-6M190 | Jiangsu Sainty Machinery GES-5M195 | Jiangsu Sainty Machinery GES-6M195 | Jiangsu Sainty Machinery GES-6M200 | Jiangsu Sainty Machinery GES-P200 | Jiangsu Sainty Machinery GES-6M205 | Jiangsu Sainty Machinery GES-6M210 | Jiangsu Sainty Machinery GES-P210 | Jiangsu Sainty Machinery GES-6M220 | Jiangsu Sainty Machinery GES-P220 | Jiangsu Sainty Machinery GES-6M225 | Jiangsu Sainty Machinery GES-6P225 | Jiangsu Sainty Machinery GES-5M230 | Jiangsu Sainty Machinery GES-6M230 | Jiangsu Sainty Machinery GES-6P230 | Jiangsu Sainty Machinery GES-P230 | Jiangsu Sainty Machinery GES-5M235 | Jiangsu Sainty Machinery GES-6M235 | Jiangsu Sainty Machinery GES-6P235 | Jiangsu Sainty Machinery GES-5M240 | Jiangsu Sainty Machinery GES-6M240 | Jiangsu Sainty Machinery GES-6P240 | Jiangsu Sainty Machinery GES-5M245 | Jiangsu Sainty Machinery GES-6M245 | Jiangsu Sainty Machinery GES-6P245 | Jiangsu Sainty Machinery GES-5M250 | Jiangsu Sainty Machinery GES-6M250 | Jiangsu Sainty Machinery GES-6P250 | Jiangsu Sainty Machinery GES-P250 | Jiangsu Sainty Machinery GES-5M255 | Jiangsu Sainty Machinery GES-6M255 | Jiangsu Sainty Machinery GES-6P255 | Jiangsu Sainty Machinery GES-6M260 | Jiangsu Sainty Machinery GES-6P260 | Jiangsu Sainty Machinery GES-P260 | Jiangsu Sainty Machinery GES-6M265 | Jiangsu Sainty Machinery GES-6P265 | Jiangsu Sainty Machinery GES-6M270 | Jiangsu Sainty Machinery GES-6P270 | Jiangsu Sainty Machinery GES-P270 | Jiangsu Sainty Machinery GES-6M275 | Jiangsu Sainty Machinery GES-6P275 | Jiangsu Sainty Machinery GES-6M280 | Jiangsu Sainty Machinery GES-6P280 | Jiangsu Sainty Machinery GES-P280 | Jiangsu Sainty Machinery GES-6M285 | Jiangsu Sainty Machinery GES-6P285 | Jiangsu Sainty Machinery GES-6M290 | Jiangsu Sainty Machinery GES-6P290 | Jiangsu Sainty Machinery GES-6M295 | Jiangsu Sainty Machinery GES-6P295 | Jiangsu Sainty Machinery GES-6M300 | Jiangsu Sainty Machinery GES-6P300 | Jiangsu Sainty Machinery GES-6M305 | Jiangsu Sainty Machinery GES-6P305 | Jiangsu Sainty Machinery GES-6M310 | Jiangsu Sainty Machinery GES-6M315 | Jiangsu Shunda PV-Tech SDM-170/(165)-72M | Jiangsu Shunda PV-Tech SDM-170/(170)-72M | Jiangsu Shunda PV-Tech SDM-170/(175)-72M | Jiangsu Shunda PV-Tech SDM-170/(180)-72M | Jiangsu Shunda PV-Tech SDM-170/(185)-72M | Jiangsu SunLink PV Technology SL180-24M170 | Jiangsu SunLink PV Technology SL180-24M175 | Jiangsu SunLink PV Technology SL180-24M180 | Jiangsu SunLink PV Technology SL180-24M185 | Jiangsu SunLink PV Technology SL180-24M190 | Jiangsu SunLink PV Technology SL180-24M195 | Jiangsu SunLink PV Technology SL220-20M200 | Jiangsu SunLink PV Technology SL220-20P200 | Jiangsu SunLink PV Technology SL220-20M205 | Jiangsu SunLink PV Technology SL220-20P205 | Jiangsu SunLink PV Technology SL220-20M210 | Jiangsu SunLink PV Technology SL220-20P210 | Jiangsu SunLink PV Technology SL220-20M215 | Jiangsu SunLink PV Technology SL220-20P215 | Jiangsu SunLink PV Technology SL220-20M220 | Jiangsu SunLink PV Technology SL220-20P220 | Jiangsu SunLink PV Technology SL240-32M220 | Jiangsu SunLink PV Technology SL220-20M225 | Jiangsu SunLink PV Technology SL220-20P225 | Jiangsu SunLink PV Technology SL240-32M225 | Jiangsu SunLink PV Technology SL220-20M230 | Jiangsu SunLink PV Technology SL220-20P230 | Jiangsu SunLink PV Technology SL240-32M230 | Jiangsu SunLink PV Technology SL220-20M235 | Jiangsu SunLink PV Technology SL220-20P235 | Jiangsu SunLink PV Technology SL240-32M235 | Jiangsu SunLink PV Technology SL220-20M240 | Jiangsu SunLink PV Technology SL220-20P240 | Jiangsu SunLink PV Technology SL240-32M240 | Jiangsu SunLink PV Technology SL220-20M245 | Jiangsu SunLink PV Technology SL240-32M245 | Jiangsu SunLink PV Technology SL220-20M250 | Jiangsu SunLink PV Technology SL240-32M250 | Jiangsu SunLink PV Technology SL220-20M255 | Jiangsu SunLink PV Technology SL240-32M255 | Jiangsu SunLink PV Technology SL220-20M260 | Jiangsu SunLink PV Technology SL280-24M260 | Jiangsu SunLink PV Technology SL280-24P260 | Jiangsu SunLink PV Technology SL280-24M265 | Jiangsu SunLink PV Technology SL280-24P265 | Jiangsu SunLink PV Technology SL280-24M270 | Jiangsu SunLink PV Technology SL280-24P270 | Jiangsu SunLink PV Technology SL280-24M275 | Jiangsu SunLink PV Technology SL280-24P275 | Jiangsu SunLink PV Technology SL280-24M280 | Jiangsu SunLink PV Technology SL280-24P280 | Jiangsu SunLink PV Technology SL280-24M285 | Jiangsu SunLink PV Technology SL280-24P285 | Jiangsu SunLink PV Technology SL280-24M290 | Jiangsu SunLink PV Technology SL280-24P290 | Jiangsu SunLink PV Technology SL280-24M295 | Jiangsu SunLink PV Technology SL280-24P295 | Jiangsu Wanfeng PV WF175M-01E | Jiangsu Wanfeng PV WF180M-01E | Jiangsu Wanfeng PV WF185M-01E | Jiangsu Wanfeng PV WF200P-02B | Jiangsu Wanfeng PV WF205P-02B | Jiangsu Wanfeng PV WF210P-02B | Jiangsu Wanfeng PV WF215P-02B | Jiangsu Wanfeng PV WF220P-02B | Jiangsu Wanfeng PV WF225P-02B | Jiangsu Wanfeng PV WF230P-02B | Jiangsu Wanfeng PV WF240P-02A | Jiangsu Wanfeng PV WF245P-02A | Jiangsu Wanfeng PV WF250P-02A | Jiangsu Wanfeng PV WF255P-02A | Jiangsu Wanfeng PV WF260P-02A | Jiangsu Wanfeng PV WF265P-02A | Jiangsu Wanfeng PV WF270P-02A | Jiangsu Wanfeng PV WF275P-02A | Jiangsu Wanfeng PV WF280P-02A | Jiangxi Best Solar High-Tech BEST-170D-24 | Jiangxi Best Solar High-Tech BEST-175D-24 | Jiangxi Best Solar High-Tech BEST-180D-24 | Jiangxi Best Solar High-Tech BEST-190P-18 | Jiangxi Best Solar High-Tech BEST-200P-18 | Jiangxi Best Solar High-Tech BEST-210P-18 | Jiangxi Best Solar High-Tech BEST-210P-20 | Jiangxi Best Solar High-Tech BEST-220D-20 | Jiangxi Best Solar High-Tech BEST-220P-20 | Jiangxi Best Solar High-Tech BEST-230P-20 | Jiangxi Best Solar High-Tech BEST-260P-24 | Jiangxi Best Solar High-Tech BEST-270P-24 | Jiangxi Best Solar High-Tech BEST-280P-24 | Jiangyin Hareon Power HR-115W/17V | Jiangyin Hareon Power HR-120W/17V | Jiangyin Hareon Power HR-125W/17V | Jiangyin Hareon Power HR-160W/24V | Jiangyin Hareon Power HR-165W/24V | Jiangyin Hareon Power HR-170W/24V | Jiangyin Hareon Power HR-175W/24V | Jiangyin Hareon Power HR-180W/24V | Jiangyin Hareon Power HR-185W/24V | Jiangyin Hareon Power HR-190W/24V | Jiangyin Hareon Power HR-195W/24V | Jiangyin Hareon Power HR-200W/18V | Jiangyin Hareon Power HR-200W/24V | Jiangyin Hareon Power HR-205W/18V | Jiangyin Hareon Power HR-210W/18V | Jiangyin Hareon Power HR-215W/18V | Jiangyin Hareon Power HR220D6P-3 | Jiangyin Hareon Power HR-220W/18V | Jiangyin Hareon Power HR225D6P-3 | Jiangyin Hareon Power HR-225P-18/Bb | Jiangyin Hareon Power HR-225P-18/Bbp | Jiangyin Hareon Power HR-225W/18V | Jiangyin Hareon Power HR230D6P-3 | Jiangyin Hareon Power HR-230P-18/Bb | Jiangyin Hareon Power HR-230P-18/Bbp | Jiangyin Hareon Power HR-230W/18V | Jiangyin Hareon Power HR235D6P-3 | Jiangyin Hareon Power HR-235P-18/Bb | Jiangyin Hareon Power HR-235P-18/Bbp | Jiangyin Hareon Power HR-235W/18V | Jiangyin Hareon Power HR-240P-18/Bb | Jiangyin Hareon Power HR-240P-18/Bbp | Jiangyin Hareon Power HR-240P-AC/Bb | Jiangyin Hareon Power HR-240P-AC/BbP | Jiangyin Hareon Power HR-240W/18V | Jiangyin Hareon Power HR-245P-18/Bb | Jiangyin Hareon Power HR-245P-18/Bbp | Jiangyin Hareon Power HR-245P-AC/Bb | Jiangyin Hareon Power HR-245P-AC/BbP | Jiangyin Hareon Power HR-250-18/Cb | Jiangyin Hareon Power HR-250-AC/Cb | Jiangyin Hareon Power HR-250P-18/Bb | Jiangyin Hareon Power HR-250P-18/Bbp | Jiangyin Hareon Power HR-250P-AC/Bb | Jiangyin Hareon Power HR-250P-AC/BbP | Jiangyin Hareon Power HRA-250P-18/Bb | Jiangyin Hareon Power HR-255-18/Cb | Jiangyin Hareon Power HR-255-AC/Cb | Jiangyin Hareon Power HR-255P-18/Bb | Jiangyin Hareon Power HR-255P-18/Bbp | Jiangyin Hareon Power HR-255P-AC/Bb | Jiangyin Hareon Power HR-255P-AC/BbP | Jiangyin Hareon Power HRA-255P-18/Bb | Jiangyin Hareon Power HR-260-18/Cb | Jiangyin Hareon Power HR-260-AC/Cb | Jiangyin Hareon Power HR-260P-18/Bb | Jiangyin Hareon Power HR-260P-18/Bbp | Jiangyin Hareon Power HR-260P-AC/Bb | Jiangyin Hareon Power HR-260P-AC/BbP | Jiangyin Hareon Power HRA-260P-18/Bb | Jiangyin Hareon Power HR-265-18/Cb | Jiangyin Hareon Power HR-265-AC/Cb | Jiangyin Hareon Power HR-265P-18/Bb | Jiangyin Hareon Power HR-265P-18/Bbp | Jiangyin Hareon Power HRA-265P-18/Bb-1 | Jiangyin Hareon Power HR-270-18/Cb | Jiangyin Hareon Power HR-270-AC/Cb | Jiangyin Hareon Power HR-270P-24/Ba | Jiangyin Hareon Power HR-270P-24/Bap | Jiangyin Hareon Power HRA-270-18/Cb | Jiangyin Hareon Power HRA-270-19/Cb | Jiangyin Hareon Power HR-275P-24/Ba | Jiangyin Hareon Power HR-275P-24/Bap | Jiangyin Hareon Power HR-280P-24/Ba | Jiangyin Hareon Power HR-280P-24/Bap | Jiangyin Hareon Power HRA-280-18/Cb-1 | Jiangyin Hareon Power HR-285P-24/Ba | Jiangyin Hareon Power HR-285P-24/Bap | Jiangyin Hareon Power HRA-285-18/Cb-1 | Jiangyin Hareon Power HR-290P-24/Ba | Jiangyin Hareon Power HR-290P-24/Bap | Jiangyin Hareon Power HR-295-24/Ca | Jiangyin Hareon Power HR-295P-24/Ba | Jiangyin Hareon Power HR-295P-24/Bap | Jiangyin Hareon Power HRA-295-18/Cb-1 | Jiangyin Hareon Power HR-300-24/Ca | Jiangyin Hareon Power HR-300P-24/Ba | Jiangyin Hareon Power HR-300P-24/Bap | Jiangyin Hareon Power HRA-300-18/Cb-1 | Jiangyin Hareon Power HRA-300P-24/Ba | Jiangyin Hareon Power HR-305-24/Ca | Jiangyin Hareon Power HR-305P-24/Ba | Jiangyin Hareon Power HR-305P-24/Bap | Jiangyin Hareon Power HRA-305P-24/Ba | Jiangyin Hareon Power HR-310-24/Ca | Jiangyin Hareon Power HR-310P-24/Ba | Jiangyin Hareon Power HR-310P-24/Bap | Jiangyin Hareon Power HRA-310P-24/Ba | Jiangyin Hareon Power HR-315-24/Ca | Jiangyin Hareon Power HR-315P-24/Ba | Jiangyin Hareon Power HR-315P-24/Bap | Jiangyin Hareon Power HRA-315-24/Ca | Jiangyin Hareon Power HRA-315P-24/Ba | Jiangyin Hareon Power HR-320P-24/Ba | Jiangyin Hareon Power HR-320P-24/Bap | Jiangyin Hareon Power HRA-320-24/Ca | Jiangyin Hareon Power HRA-320P-24/Ba-1 | Jiangyin Hareon Power HRA-335-24/Ca-1 | Jiangyin Hareon Power HRA-340-24/Ca-1 | Jiangyin Hareon Power HRA-350-24/Ca-1 | Jiangyin Hareon Power HRA-355-24/Ca-1 | Jiangyin Jetion Science and Technology JT210PCe | Jiangyin Jetion Science and Technology JT215PCe | Jiawei Solarchina (Shenzhen) JW-G2300/MD6660P-1 | Jiawei Solarchina (Shenzhen) JW-G2300/QC6660P-1 | Jingao Solar JAM5(L)-175 | Jingao Solar JAM5(L)-180 | Jingao Solar JAM5(L)-185 | Jingao Solar JAM6-200 | Jingao Solar JAP6-200 | Jingao Solar JAM6-205 | Jingao Solar JAP6-205 | Jingao Solar JAM6-210 | Jingao Solar JAP6-210 | Jingao Solar JAM6-215 | Jingao Solar JAP6-215 | Jingao Solar JAM6-220 | Jingao Solar JAP6-220 | Jingao Solar JAM6-225 | Jingao Solar JAP6-225 | Jingao Solar JAM6-230 | Jingao Solar JAP6-230 | Jingao Solar JAM6-235 | Jingao Solar JAP6-235 | Jingao Solar JAM6-240 | Jingao Solar JAP6-240 | Jinko Solar Co._ Ltd JKM170M-72B | Jinko Solar Co._ Ltd JKM175M-72 | Jinko Solar Co._ Ltd JKM175M-72B | Jinko Solar Co._ Ltd JKM180M-72 | Jinko Solar Co._ Ltd JKM180M-72B | Jinko Solar Co._ Ltd JKM185M-72 | Jinko Solar Co._ Ltd JKM185M-72B | Jinko Solar Co._ Ltd JKM190M-72 | Jinko Solar Co._ Ltd JKM190M-72B | Jinko Solar Co._ Ltd JKM195M-72 | Jinko Solar Co._ Ltd JKM195M-72B | Jinko Solar Co._ Ltd JKM200M-60B | Jinko Solar Co._ Ltd JKM200M-72 | Jinko Solar Co._ Ltd JKM200M-72B | Jinko Solar Co._ Ltd JKM200P-60B | Jinko Solar Co._ Ltd JKM205M-60B | Jinko Solar Co._ Ltd JKM205M-72 | Jinko Solar Co._ Ltd JKM205M-72B | Jinko Solar Co._ Ltd JKM205P-60B | Jinko Solar Co._ Ltd JKM210M-60B | Jinko Solar Co._ Ltd JKM210P-60B | Jinko Solar Co._ Ltd JKM215M-60B | Jinko Solar Co._ Ltd JKM215P-60B | Jinko Solar Co._ Ltd JKM220M-60 | Jinko Solar Co._ Ltd JKM220M-60B | Jinko Solar Co._ Ltd JKM220P-60 | Jinko Solar Co._ Ltd JKM220P-60B | Jinko Solar Co._ Ltd JKM225M-60 | Jinko Solar Co._ Ltd JKM225M-60B | Jinko Solar Co._ Ltd JKM225P-60 | Jinko Solar Co._ Ltd JKM225P-60B | Jinko Solar Co._ Ltd JKM230M-60 | Jinko Solar Co._ Ltd JKM230M-60B | Jinko Solar Co._ Ltd JKM230P-60 | Jinko Solar Co._ Ltd JKM230P-60B | Jinko Solar Co._ Ltd JKM235M-60 | Jinko Solar Co._ Ltd JKM235M-60B | Jinko Solar Co._ Ltd JKM235P-60 | Jinko Solar Co._ Ltd JKM235P-60B | Jinko Solar Co._ Ltd JKM240M-60 | Jinko Solar Co._ Ltd JKM240M-60B | Jinko Solar Co._ Ltd JKM240P-60 | Jinko Solar Co._ Ltd JKM240P-60B | Jinko Solar Co._ Ltd JKM240PP-60B | Jinko Solar Co._ Ltd JKM245M-60 | Jinko Solar Co._ Ltd JKM245M-60B | Jinko Solar Co._ Ltd JKM245P-60 | Jinko Solar Co._ Ltd JKM245P-60B | Jinko Solar Co._ Ltd JKM245PP-60(Plus) | Jinko Solar Co._ Ltd JKM245PP-60B | Jinko Solar Co._ Ltd JKMS245P-60 | Jinko Solar Co._ Ltd JKMS245PP-60 | Jinko Solar Co._ Ltd JKM250M-60 | Jinko Solar Co._ Ltd JKM250M-72B | Jinko Solar Co._ Ltd JKM250P-60 | Jinko Solar Co._ Ltd JKM250P-60B | Jinko Solar Co._ Ltd JKM250P-60-J4 | Jinko Solar Co._ Ltd JKM250P-60-V | Jinko Solar Co._ Ltd JKM250P-72 | Jinko Solar Co._ Ltd JKM250P-72B | Jinko Solar Co._ Ltd JKM250PP-60 | Jinko Solar Co._ Ltd JKM250PP-60(Plus) | Jinko Solar Co._ Ltd JKM250PP-60B | Jinko Solar Co._ Ltd JKM250PP-60-J4 | Jinko Solar Co._ Ltd JKM250PP-60-V | Jinko Solar Co._ Ltd JKMS250P-60 | Jinko Solar Co._ Ltd JKMS250PP-60 | Jinko Solar Co._ Ltd JKM255M-60 | Jinko Solar Co._ Ltd JKM255M-72B | Jinko Solar Co._ Ltd JKM255M-96 | Jinko Solar Co._ Ltd JKM255P-60 | Jinko Solar Co._ Ltd JKM255P-60B | Jinko Solar Co._ Ltd JKM255P-60-J4 | Jinko Solar Co._ Ltd JKM255P-60-V | Jinko Solar Co._ Ltd JKM255P-72 | Jinko Solar Co._ Ltd JKM255P-72B | Jinko Solar Co._ Ltd JKM255PP-60 | Jinko Solar Co._ Ltd JKM255PP-60(Plus) | Jinko Solar Co._ Ltd JKM255PP-60B | Jinko Solar Co._ Ltd JKM255PP-60-J4 | Jinko Solar Co._ Ltd JKM255PP-60-V | Jinko Solar Co._ Ltd JKMS255P-60 | Jinko Solar Co._ Ltd JKMS255PP-60 | Jinko Solar Co._ Ltd JKM260M-60B | Jinko Solar Co._ Ltd JKM260M-72B | Jinko Solar Co._ Ltd JKM260M-96 | Jinko Solar Co._ Ltd JKM260P-60 | Jinko Solar Co._ Ltd JKM260P-60B | Jinko Solar Co._ Ltd JKM260P-60-J4 | Jinko Solar Co._ Ltd JKM260P-60-V | Jinko Solar Co._ Ltd JKM260P-72 | Jinko Solar Co._ Ltd JKM260P-72B | Jinko Solar Co._ Ltd JKM260PP-60 | Jinko Solar Co._ Ltd JKM260PP-60(Plus) | Jinko Solar Co._ Ltd JKM260PP-60B | Jinko Solar Co._ Ltd JKM260PP-60-J4 | Jinko Solar Co._ Ltd JKM260PP-60-V | Jinko Solar Co._ Ltd JKMS260M-60 | Jinko Solar Co._ Ltd JKMS260M-60B-EP | Jinko Solar Co._ Ltd JKMS260P-60 | Jinko Solar Co._ Ltd JKMS260PP-60 | Jinko Solar Co._ Ltd JKM265M-60B | Jinko Solar Co._ Ltd JKM265M-72B | Jinko Solar Co._ Ltd JKM265M-96 | Jinko Solar Co._ Ltd JKM265P-60 | Jinko Solar Co._ Ltd JKM265P-60B | Jinko Solar Co._ Ltd JKM265P-60-J4 | Jinko Solar Co._ Ltd JKM265P-60-V | Jinko Solar Co._ Ltd JKM265P-72 | Jinko Solar Co._ Ltd JKM265P-72B | Jinko Solar Co._ Ltd JKM265PP-60 | Jinko Solar Co._ Ltd JKM265PP-60(Plus) | Jinko Solar Co._ Ltd JKM265PP-60B | Jinko Solar Co._ Ltd JKM265PP-60-J4 | Jinko Solar Co._ Ltd JKM265PP-60-V | Jinko Solar Co._ Ltd JKMS265M-60 | Jinko Solar Co._ Ltd JKMS265M-60B-EP | Jinko Solar Co._ Ltd JKMS265P-60 | Jinko Solar Co._ Ltd JKMS265PP-60 | Jinko Solar Co._ Ltd JKM270M-60B | Jinko Solar Co._ Ltd JKM270M-60-V | Jinko Solar Co._ Ltd JKM270M-72 | Jinko Solar Co._ Ltd JKM270M-72B | Jinko Solar Co._ Ltd JKM270M-96 | Jinko Solar Co._ Ltd JKM270P-60 | Jinko Solar Co._ Ltd JKM270P-60-J4 | Jinko Solar Co._ Ltd JKM270P-60-V | Jinko Solar Co._ Ltd JKM270P-72 | Jinko Solar Co._ Ltd JKM270P-72B | Jinko Solar Co._ Ltd JKM270PP-60 | Jinko Solar Co._ Ltd JKM270PP-60-J4 | Jinko Solar Co._ Ltd JKM270PP-60-V | Jinko Solar Co._ Ltd JKMS270M-60 | Jinko Solar Co._ Ltd JKMS270M-60B-EP | Jinko Solar Co._ Ltd JKMS270M-60-J4 | Jinko Solar Co._ Ltd JKM275M-60 | Jinko Solar Co._ Ltd JKM275M-60B | Jinko Solar Co._ Ltd JKM275M-60B-J4 | Jinko Solar Co._ Ltd JKM275M-60-J4 | Jinko Solar Co._ Ltd JKM275M-60-V | Jinko Solar Co._ Ltd JKM275M-72 | Jinko Solar Co._ Ltd JKM275M-72B | Jinko Solar Co._ Ltd JKM275M-96 | Jinko Solar Co._ Ltd JKM275P-60 | Jinko Solar Co._ Ltd JKM275P-72 | Jinko Solar Co._ Ltd JKM275P-72B | Jinko Solar Co._ Ltd JKM275PP-60 | Jinko Solar Co._ Ltd JKM275PP-60H | Jinko Solar Co._ Ltd JKM275PP-60H-V | Jinko Solar Co._ Ltd JKM275PP-60-J4 | Jinko Solar Co._ Ltd JKM275PP-60-V | Jinko Solar Co._ Ltd JKMS275M-60 | Jinko Solar Co._ Ltd JKMS275M-60B-EP | Jinko Solar Co._ Ltd JKMS275M-60-EP | Jinko Solar Co._ Ltd JKMS275M-60-J4 | Jinko Solar Co._ Ltd JKMS275PP-60 | Jinko Solar Co._ Ltd JKMS275PP-60-J4 | Jinko Solar Co._ Ltd JKM280M-60 | Jinko Solar Co._ Ltd JKM280M-60B | Jinko Solar Co._ Ltd JKM280M-60B-J4 | Jinko Solar Co._ Ltd JKM280M-60H | Jinko Solar Co._ Ltd JKM280M-60HB | Jinko Solar Co._ Ltd JKM280M-60HB-V | Jinko Solar Co._ Ltd JKM280M-60H-V | Jinko Solar Co._ Ltd JKM280M-60-J4 | Jinko Solar Co._ Ltd JKM280M-60-V | Jinko Solar Co._ Ltd JKM280M-72 | Jinko Solar Co._ Ltd JKM280M-72B | Jinko Solar Co._ Ltd JKM280M-96 | Jinko Solar Co._ Ltd JKM280P-60 | Jinko Solar Co._ Ltd JKM280P-72 | Jinko Solar Co._ Ltd JKM280P-72B | Jinko Solar Co._ Ltd JKM280PP-60 | Jinko Solar Co._ Ltd JKM280PP-60H | Jinko Solar Co._ Ltd JKM280PP-60H-V | Jinko Solar Co._ Ltd JKM280PP-60-J4 | Jinko Solar Co._ Ltd JKM280PP-60-V | Jinko Solar Co._ Ltd JKMS280M-60 | Jinko Solar Co._ Ltd JKMS280M-60B-EP | Jinko Solar Co._ Ltd JKMS280M-60-EP | Jinko Solar Co._ Ltd JKMS280M-60-J4 | Jinko Solar Co._ Ltd JKM285M-60 | Jinko Solar Co._ Ltd JKM285M-60B | Jinko Solar Co._ Ltd JKM285M-60B-J4 | Jinko Solar Co._ Ltd JKM285M-60H | Jinko Solar Co._ Ltd JKM285M-60HB | Jinko Solar Co._ Ltd JKM285M-60HB-V | Jinko Solar Co._ Ltd JKM285M-60H-V | Jinko Solar Co._ Ltd JKM285M-60-J4 | Jinko Solar Co._ Ltd JKM285M-60-V | Jinko Solar Co._ Ltd JKM285M-72 | Jinko Solar Co._ Ltd JKM285M-72B | Jinko Solar Co._ Ltd JKM285P-60 | Jinko Solar Co._ Ltd JKM285P-72 | Jinko Solar Co._ Ltd JKM285P-72B | Jinko Solar Co._ Ltd JKM285PP-60 | Jinko Solar Co._ Ltd JKM285PP-60H | Jinko Solar Co._ Ltd JKM285PP-60H-V | Jinko Solar Co._ Ltd JKM285PP-60-J4 | Jinko Solar Co._ Ltd JKM285PP-60-V | Jinko Solar Co._ Ltd JKMS285M-60 | Jinko Solar Co._ Ltd JKMS285M-60B-EP | Jinko Solar Co._ Ltd JKMS285M-60-EP | Jinko Solar Co._ Ltd JKMS285M-60-J4 | Jinko Solar Co._ Ltd JKM290M-60 | Jinko Solar Co._ Ltd JKM290M-60B | Jinko Solar Co._ Ltd JKM290M-60B-J4 | Jinko Solar Co._ Ltd JKM290M-60H | Jinko Solar Co._ Ltd JKM290M-60HB | Jinko Solar Co._ Ltd JKM290M-60HB-V | Jinko Solar Co._ Ltd JKM290M-60H-V | Jinko Solar Co._ Ltd JKM290M-60-J4 | Jinko Solar Co._ Ltd JKM290M-60-V | Jinko Solar Co._ Ltd JKM290M-72 | Jinko Solar Co._ Ltd JKM290M-72B | Jinko Solar Co._ Ltd JKM290P-60 | Jinko Solar Co._ Ltd JKM290P-72 | Jinko Solar Co._ Ltd JKM290P-72B | Jinko Solar Co._ Ltd JKM290PP-60 | Jinko Solar Co._ Ltd JKM290PP-60-J4 | Jinko Solar Co._ Ltd JKM290PP-60-V | Jinko Solar Co._ Ltd JKM290PP-72(Plus) | Jinko Solar Co._ Ltd JKM290PP-72B | Jinko Solar Co._ Ltd JKMS290M-60 | Jinko Solar Co._ Ltd JKMS290M-60B-EP | Jinko Solar Co._ Ltd JKMS290M-60-EP | Jinko Solar Co._ Ltd JKMS290M-60-J4 | Jinko Solar Co._ Ltd JKMS290M-72 | Jinko Solar Co._ Ltd JKMS290P-72 | Jinko Solar Co._ Ltd JKMS290PP-72 | Jinko Solar Co._ Ltd JKM295M-60 | Jinko Solar Co._ Ltd JKM295M-60B | Jinko Solar Co._ Ltd JKM295M-60B-J4 | Jinko Solar Co._ Ltd JKM295M-60H | Jinko Solar Co._ Ltd JKM295M-60HB | Jinko Solar Co._ Ltd JKM295M-60HB-V | Jinko Solar Co._ Ltd JKM295M-60H-V | Jinko Solar Co._ Ltd JKM295M-60-J4 | Jinko Solar Co._ Ltd JKM295M-60-V | Jinko Solar Co._ Ltd JKM295M-72 | Jinko Solar Co._ Ltd JKM295M-72B | Jinko Solar Co._ Ltd JKM295P-72 | Jinko Solar Co._ Ltd JKM295P-72B | Jinko Solar Co._ Ltd JKM295PP-72 | Jinko Solar Co._ Ltd JKM295PP-72(Plus) | Jinko Solar Co._ Ltd JKM295PP-72B | Jinko Solar Co._ Ltd JKMS295M-60B-EP | Jinko Solar Co._ Ltd JKMS295M-60-EP | Jinko Solar Co._ Ltd JKMS295M-72 | Jinko Solar Co._ Ltd JKMS295P-72 | Jinko Solar Co._ Ltd JKMS295PP-72 | Jinko Solar Co._ Ltd JKM300M-60 | Jinko Solar Co._ Ltd JKM300M-60B | Jinko Solar Co._ Ltd JKM300M-60BL | Jinko Solar Co._ Ltd JKM300M-60HB-V | Jinko Solar Co._ Ltd JKM300M-60-V | Jinko Solar Co._ Ltd JKM300M-72 | Jinko Solar Co._ Ltd JKM300M-72B | Jinko Solar Co._ Ltd JKM300P-72 | Jinko Solar Co._ Ltd JKM300P-72B | Jinko Solar Co._ Ltd JKM300PP-72 | Jinko Solar Co._ Ltd JKM300PP-72(Plus) | Jinko Solar Co._ Ltd JKM300PP-72B | Jinko Solar Co._ Ltd JKMS300M-60-EP | Jinko Solar Co._ Ltd JKMS300M-72 | Jinko Solar Co._ Ltd JKMS300P-72 | Jinko Solar Co._ Ltd JKMS300PP-72 | Jinko Solar Co._ Ltd JKM305M-60 | Jinko Solar Co._ Ltd JKM305M-60B | Jinko Solar Co._ Ltd JKM305M-60BL | Jinko Solar Co._ Ltd JKM305M-60HB-V | Jinko Solar Co._ Ltd JKM305M-60H-V | Jinko Solar Co._ Ltd JKM305M-60L | Jinko Solar Co._ Ltd JKM305M-60-V | Jinko Solar Co._ Ltd JKM305M-72 | Jinko Solar Co._ Ltd JKM305M-72B | Jinko Solar Co._ Ltd JKM305P-72 | Jinko Solar Co._ Ltd JKM305P-72B | Jinko Solar Co._ Ltd JKM305P-72-J4 | Jinko Solar Co._ Ltd JKM305P-72-V | Jinko Solar Co._ Ltd JKM305PP-72 | Jinko Solar Co._ Ltd JKM305PP-72(Plus) | Jinko Solar Co._ Ltd JKM305PP-72B | Jinko Solar Co._ Ltd JKM305PP-72-J4 | Jinko Solar Co._ Ltd JKM305PP-72-V | Jinko Solar Co._ Ltd JKMS305M-72 | Jinko Solar Co._ Ltd JKMS305P-72 | Jinko Solar Co._ Ltd JKMS305PP-72 | Jinko Solar Co._ Ltd JKM310M-60 | Jinko Solar Co._ Ltd JKM310M-60B | Jinko Solar Co._ Ltd JKM310M-60BL | Jinko Solar Co._ Ltd JKM310M-60HB-V | Jinko Solar Co._ Ltd JKM310M-60L | Jinko Solar Co._ Ltd JKM310M-72 | Jinko Solar Co._ Ltd JKM310M-72B | Jinko Solar Co._ Ltd JKM310P-72 | Jinko Solar Co._ Ltd JKM310P-72B | Jinko Solar Co._ Ltd JKM310P-72-J4 | Jinko Solar Co._ Ltd JKM310P-72-V | Jinko Solar Co._ Ltd JKM310PP-72 | Jinko Solar Co._ Ltd JKM310PP-72(Plus) | Jinko Solar Co._ Ltd JKM310PP-72B | Jinko Solar Co._ Ltd JKM310PP-72-J4 | Jinko Solar Co._ Ltd JKM310PP-72-V | Jinko Solar Co._ Ltd JKMS310M-72 | Jinko Solar Co._ Ltd JKMS310P-72 | Jinko Solar Co._ Ltd JKMS310PP-72 | Jinko Solar Co._ Ltd JKM315M-60 | Jinko Solar Co._ Ltd JKM315M-60B | Jinko Solar Co._ Ltd JKM315M-60BL | Jinko Solar Co._ Ltd JKM315M-60HB | Jinko Solar Co._ Ltd JKM315M-60L | Jinko Solar Co._ Ltd JKM315M-72B | Jinko Solar Co._ Ltd JKM315P-72 | Jinko Solar Co._ Ltd JKM315P-72B | Jinko Solar Co._ Ltd JKM315P-72-J4 | Jinko Solar Co._ Ltd JKM315P-72-V | Jinko Solar Co._ Ltd JKM315PP-72 | Jinko Solar Co._ Ltd JKM315PP-72(Plus) | Jinko Solar Co._ Ltd JKM315PP-72B | Jinko Solar Co._ Ltd JKM315PP-72-J4 | Jinko Solar Co._ Ltd JKM315PP-72-V | Jinko Solar Co._ Ltd JKMS315M-72 | Jinko Solar Co._ Ltd JKMS315P-72 | Jinko Solar Co._ Ltd JKMS315PP-72 | Jinko Solar Co._ Ltd JKM320M-60 | Jinko Solar Co._ Ltd JKM320M-60B | Jinko Solar Co._ Ltd JKM320M-60BL | Jinko Solar Co._ Ltd JKM320M-60HB | Jinko Solar Co._ Ltd JKM320M-60HB-V | Jinko Solar Co._ Ltd JKM320M-60L | Jinko Solar Co._ Ltd JKM320M-72B | Jinko Solar Co._ Ltd JKM320P-72 | Jinko Solar Co._ Ltd JKM320P-72B | Jinko Solar Co._ Ltd JKM320P-72-J4 | Jinko Solar Co._ Ltd JKM320P-72-V | Jinko Solar Co._ Ltd JKM320PP-72 | Jinko Solar Co._ Ltd JKM320PP-72(Plus) | Jinko Solar Co._ Ltd JKM320PP-72B | Jinko Solar Co._ Ltd JKM320PP-72-J4 | Jinko Solar Co._ Ltd JKM320PP-72-V | Jinko Solar Co._ Ltd JKMS320M-72 | Jinko Solar Co._ Ltd JKMS320P-72 | Jinko Solar Co._ Ltd JKMS320PP-72 | Jinko Solar Co._ Ltd JKMS320PP-72-J4 | Jinko Solar Co._ Ltd JKM325M-60BL | Jinko Solar Co._ Ltd JKM325M-60L | Jinko Solar Co._ Ltd JKM325M-72 | Jinko Solar Co._ Ltd JKM325M-72-J4 | Jinko Solar Co._ Ltd JKM325P-72 | Jinko Solar Co._ Ltd JKM325P-72-J4 | Jinko Solar Co._ Ltd JKM325P-72-V | Jinko Solar Co._ Ltd JKM325PP-72 | Jinko Solar Co._ Ltd JKM325PP-72-J4 | Jinko Solar Co._ Ltd JKM325PP-72-V | Jinko Solar Co._ Ltd JKMS325M-72 | Jinko Solar Co._ Ltd JKMS325M-72-J4 | Jinko Solar Co._ Ltd JKMS325PP-72 | Jinko Solar Co._ Ltd JKMS325PP-72-J4 | Jinko Solar Co._ Ltd JKM330M-60L | Jinko Solar Co._ Ltd JKM330M-72 | Jinko Solar Co._ Ltd JKM330M-72-J4 | Jinko Solar Co._ Ltd JKM330M-72-V | Jinko Solar Co._ Ltd JKM330P-72 | Jinko Solar Co._ Ltd JKM330P-72-J4 | Jinko Solar Co._ Ltd JKM330P-72-V | Jinko Solar Co._ Ltd JKM330PP-72 | Jinko Solar Co._ Ltd JKM330PP-72H | Jinko Solar Co._ Ltd JKM330PP-72H-V | Jinko Solar Co._ Ltd JKM330PP-72-J4 | Jinko Solar Co._ Ltd JKM330PP-72-V | Jinko Solar Co._ Ltd JKMS330M-72 | Jinko Solar Co._ Ltd JKMS330M-72-J4 | Jinko Solar Co._ Ltd JKMS330PP-72 | Jinko Solar Co._ Ltd JKMS330PP-72-J4 | Jinko Solar Co._ Ltd JKM335M-72 | Jinko Solar Co._ Ltd JKM335M-72B | Jinko Solar Co._ Ltd JKM335M-72B-J4 | Jinko Solar Co._ Ltd JKM335M-72H | Jinko Solar Co._ Ltd JKM335M-72HB | Jinko Solar Co._ Ltd JKM335M-72HB-V | Jinko Solar Co._ Ltd JKM335M-72H-V | Jinko Solar Co._ Ltd JKM335M-72-J4 | Jinko Solar Co._ Ltd JKM335M-72-V | Jinko Solar Co._ Ltd JKM335P-72 | Jinko Solar Co._ Ltd JKM335PP-72 | Jinko Solar Co._ Ltd JKM335PP-72H-V | Jinko Solar Co._ Ltd JKM335PP-72-J4 | Jinko Solar Co._ Ltd JKM335PP-72-V | Jinko Solar Co._ Ltd JKMS335M-72 | Jinko Solar Co._ Ltd JKMS335M-72-J4 | Jinko Solar Co._ Ltd JKM340M-72 | Jinko Solar Co._ Ltd JKM340M-72B | Jinko Solar Co._ Ltd JKM340M-72B-J4 | Jinko Solar Co._ Ltd JKM340M-72H | Jinko Solar Co._ Ltd JKM340M-72HB | Jinko Solar Co._ Ltd JKM340M-72HB-V | Jinko Solar Co._ Ltd JKM340M-72H-V | Jinko Solar Co._ Ltd JKM340M-72-J4 | Jinko Solar Co._ Ltd JKM340M-72-V | Jinko Solar Co._ Ltd JKM340PP-72H-V | Jinko Solar Co._ Ltd JKM340PP-72-V | Jinko Solar Co._ Ltd JKMS340M-72 | Jinko Solar Co._ Ltd JKMS340M-72-J4 | Jinko Solar Co._ Ltd JKM340P-72 | Jinko Solar Co._ Ltd JKM340PP-72 | Jinko Solar Co._ Ltd JKM340PP-72-J4 | Jinko Solar Co._ Ltd JKM345M-72 | Jinko Solar Co._ Ltd JKM345M-72B | Jinko Solar Co._ Ltd JKM345M-72B-J4 | Jinko Solar Co._ Ltd JKM345M-72H | Jinko Solar Co._ Ltd JKM345M-72HB | Jinko Solar Co._ Ltd JKM345M-72HB-V | Jinko Solar Co._ Ltd JKM345M-72H-V | Jinko Solar Co._ Ltd JKM345M-72-J4 | Jinko Solar Co._ Ltd JKM345M-72-V | Jinko Solar Co._ Ltd JKM345P-72 | Jinko Solar Co._ Ltd JKM345PP-72 | Jinko Solar Co._ Ltd JKM345PP-72-J4 | Jinko Solar Co._ Ltd JKM345PP-72-V | Jinko Solar Co._ Ltd JKMS345M-72 | Jinko Solar Co._ Ltd JKMS345M-72-J4 | Jinko Solar Co._ Ltd JKM350M-72 | Jinko Solar Co._ Ltd JKM350M-72B | Jinko Solar Co._ Ltd JKM350M-72B-J4 | Jinko Solar Co._ Ltd JKM350M-72HB | Jinko Solar Co._ Ltd JKM350M-72HB-V | Jinko Solar Co._ Ltd JKM350M-72H-V | Jinko Solar Co._ Ltd JKM350M-72-J4 | Jinko Solar Co._ Ltd JKM350M-72-V | Jinko Solar Co._ Ltd JKM350P-72 | Jinko Solar Co._ Ltd JKM350PP-72 | Jinko Solar Co._ Ltd JKM350PP-72-J4 | Jinko Solar Co._ Ltd JKM350PP-72-V | Jinko Solar Co._ Ltd JKMS350M-72 | Jinko Solar Co._ Ltd JKMS350M-72-J4 | Jinko Solar Co._ Ltd JKM355M-72 | Jinko Solar Co._ Ltd JKM355M-72B | Jinko Solar Co._ Ltd JKM355M-72B-J4 | Jinko Solar Co._ Ltd JKM355M-72HB | Jinko Solar Co._ Ltd JKM355M-72HB-V | Jinko Solar Co._ Ltd JKM355M-72H-V | Jinko Solar Co._ Ltd JKM355M-72-J4 | Jinko Solar Co._ Ltd JKM355M-72-V | Jinko Solar Co._ Ltd JKMS355M-72 | Jinko Solar Co._ Ltd JKMS355M-72-J4 | Jinko Solar Co._ Ltd JKM360M-72 | Jinko Solar Co._ Ltd JKM360M-72HB | Jinko Solar Co._ Ltd JKM360M-72HB-V | Jinko Solar Co._ Ltd JKM360M-72H-V | Jinko Solar Co._ Ltd JKM360M-72-V | Jinko Solar Co._ Ltd JKM365M-72 | Jinko Solar Co._ Ltd JKM365M-72-V | Jinko Solar Co._ Ltd JKM370M-72 | Jinko Solar Co._ Ltd JKM370M-72L-V | Jinko Solar Co._ Ltd JKM370M-72-V | Jinko Solar Co._ Ltd JKM375M-72 | Jinko Solar Co._ Ltd JKM375M-72HB-V | Jinko Solar Co._ Ltd JKM375M-72H-V | Jinko Solar Co._ Ltd JKM375M-72L-V | Jinko Solar Co._ Ltd JKM375M-72-V | Jinko Solar Co._ Ltd JKM380M-72 | Jinko Solar Co._ Ltd JKM380M-72L-V | Jinko Solar Co._ Ltd JKM380M-72-V | Jinko Solar Co._ Ltd JKM385M-72L-V | Jinko Solar Co._ Ltd JKM385M-72-V | Jinko Solar Co._ Ltd JKM390M-72HL | Jinko Solar Co._ Ltd JKM390M-72HL-V | Jinko Solar Co._ Ltd JKM390M-72L-V | Jinko Solar Co._ Ltd JKM395M-72HL | Jinko Solar Co._ Ltd JKM395M-72HL-V | Jinko Solar Co._ Ltd JKM395M-72L-V | Jinko Solar Co._ Ltd JKM400M-72HL | Jinko Solar Co._ Ltd JKM400M-72HL-V | Jinko Solar Co._ Ltd JKM400M-72L-V | Jinneng Clean Energy Technology JNMP60-245 | Jinneng Clean Energy Technology JNMM60-250 | Jinneng Clean Energy Technology JNMP60-250 | Jinneng Clean Energy Technology JNMM60-255 | Jinneng Clean Energy Technology JNMP60-255 | Jinneng Clean Energy Technology JNMM60-260 | Jinneng Clean Energy Technology JNMP60-260 | Jinneng Clean Energy Technology JNMM60-265 | Jinneng Clean Energy Technology JNMP60-265 | Jinneng Clean Energy Technology JNMM60-270 | Jinneng Clean Energy Technology JNMP72-295 | Jinneng Clean Energy Technology JNMP72-300 | Jinneng Clean Energy Technology JNMM72-305 | Jinneng Clean Energy Technology JNMP72-305 | Jinneng Clean Energy Technology JNMM72-310 | Jinneng Clean Energy Technology JNMP72-310 | Jinneng Clean Energy Technology JNMM72-315 | Jinneng Clean Energy Technology JNMP72-315 | Jinneng Clean Energy Technology JNMM72-320 | Jinneng Clean Energy Technology JNMP72-320 | Jinneng Clean Energy Technology JNMM72-325 | Jinneng Clean Energy Technology JNMP72-325 | Jinneng Clean Energy Technology JNMM72-330 | Jinneng Clean Energy Technology JNMM72-335 | Jinzhou Jinmao Photovoltaic Technology JMPV-5M/36-85 | Jinzhou Jinmao Photovoltaic Technology JMPV-5M/36-90 | Jinzhou Jinmao Photovoltaic Technology JMPV-5M/36-95 | Jinzhou Jinmao Photovoltaic Technology JMPV-5M/72-165 | Jinzhou Jinmao Photovoltaic Technology JMPV-5M/72-170 | Jinzhou Jinmao Photovoltaic Technology JMPV-5M/72-175 | Jinzhou Jinmao Photovoltaic Technology JMPV-5M/72-180 | Jinzhou Jinmao Photovoltaic Technology JMPV-5M/72-185 | Jinzhou Jinmao Photovoltaic Technology JMPV-5M/72-190 | JSPV JSMP2404 | JSPV JSMP2454 | JSPV JSMM2504 | JSPV JSMP2504 | JSPV JSMP250A | JSPV JSMM2554 | JSPV JSMP255A | JSPV JSMM2604 | JSPV JSMP260A | JSPV JSMP265A | JSPV JSMP270A | JSPV JSMP3003 | JSPV JSMP305A | JSPV JSMP310A | JSPV JSMP315A | JSPV JSMP320A | Juli New Energy JLS155M | Juli New Energy JLS160M | Juli New Energy JLS165M | Juli New Energy JLS170M | Juli New Energy JLS175M | Juli New Energy JLS180M | Juli New Energy JLS200M | Juli New Energy JLS205M | Juli New Energy JLS210M | Juli New Energy JLS215P | Juli New Energy JLS220P | Juli New Energy JLS225P | Juli New Energy JLS230P | Juli New Energy JLS60P240WH(156) | Juli New Energy JLS60P245WH(156) | Juli New Energy JLS60M250WH(156) | Juli New Energy JLS60P250WH(156) | Juli New Energy JLS60M255WH(156) | Juli New Energy JLS60P255WH(156) | Juli New Energy JLS60M260WH(156) | Juli New Energy JLS60P260WH(156) | Juli New Energy JLS60M265WH(156) | Juli New Energy JLS72P290WH(156) | Juli New Energy JLS72P295WH(156) | Juli New Energy JLS72M300WH(156) | Juli New Energy JLS72P300WH(156) | Juli New Energy JLS72M305WH(156) | Juli New Energy JLS72P305WH(156) | Juli New Energy JLS72M310WH(156) | Juli New Energy JLS72P310WH(156) | Juli New Energy JLS72M315WH(156) | Juli New Energy JLS72M320WH(156) | Jumao Photonic (Xiamen) JMP-85W-S5-G | Jumao Photonic (Xiamen) JMP-160W-S5-G | Jumao Photonic (Xiamen) JMP-170W-S5-G | Jumao Photonic (Xiamen) JMP-210W-M6-G | Jumao Photonic (Xiamen) JMP-215W-M6-G | Jumao Photonic (Xiamen) JMP-220W-M6-G | Jumao Photonic (Xiamen) JMP-225W-M6-G | Jumao Photonic (Xiamen) JMP-230W-M6-G | Kaneka G-SA060 | Kaneka GSA221 | Kaneka U-SA105 | Kaneka U-SA110 | KD Solar KD-20012A2 | KD Solar KD-20013A2 | KD Solar KD-20512A2 | KD Solar KD-20513A2 | KD Solar KD-21012A2 | KD Solar KD-21013A2 | KD Solar KD-21512A2 | KD Solar KD-21513A2 | KD Solar KD-22012A2 | KD Solar KD-22013A2 | KD Solar KD-22512A2 | KD Solar KD-22513A2 | KD Solar KD-23012A2 | KD Solar KD-23013A2 | KD Solar KD-23512A2 | KD Solar KD-24012A2 | Kenmec Mechanical Engineering TKSE-13001 | Kenmec Mechanical Engineering TKSE-13501 | Kenmec Mechanical Engineering TKSE-14001 | Kenmec Mechanical Engineering TKSD-15001 | Kenmec Mechanical Engineering TKSD-15501 | Kenmec Mechanical Engineering TKSD-16001 | Kenmec Mechanical Engineering TKSD-16501 | Kenmec Mechanical Engineering TKSC-17001 | Kenmec Mechanical Engineering TKSC-17501 | Kenmec Mechanical Engineering TKSC-18001 | Kenmec Mechanical Engineering TKSC-18501 | Kenmec Mechanical Engineering TKSC-19001 | Kenmec Mechanical Engineering TKSB-20001 | Kenmec Mechanical Engineering TKSB-20501 | Kenmec Mechanical Engineering TKSB-21001 | Kenmec Mechanical Engineering TKSB-21501 | Kenmec Mechanical Engineering TKSA-22001 | Kenmec Mechanical Engineering TKSB-22001 | Kenmec Mechanical Engineering TKSA-22501 | Kenmec Mechanical Engineering TKSA-23001 | Kenmec Mechanical Engineering TKSA-23501 | Kenmec Mechanical Engineering TKSA-24001 | Kenmec Mechanical Engineering TKSA-24501 | Kenmec Mechanical Engineering TKSA-25001 | Kenmec Mechanical Engineering TKSG-25001 | Kenmec Mechanical Engineering TKSA-25501 | Kenmec Mechanical Engineering TKSG-25501 | Kenmec Mechanical Engineering TKSA-26001 | Kenmec Mechanical Engineering TKSG-26001 | Kenmec Mechanical Engineering TKSG-26501 | Kenmec Mechanical Engineering TKSG-27001 | Kenmec Mechanical Engineering TKSG-27501 | Kenmec Mechanical Engineering TKSG-28001 | Kenmec Mechanical Engineering TKSG-28501 | Kenmec Mechanical Engineering TKSG-29001 | Kenmec Mechanical Engineering TKSG-29501 | Kenmec Mechanical Engineering TKSG-30001 | Kenmec Mechanical Engineering TKSG-30501 | Kenmec Mechanical Engineering TKSG-31001 | Kenmec Mechanical Engineering TKSG-31501 | Kenmos Photovoltaic aTT-50W-02 | Kinve Solar Power KV170-72M | Kinve Solar Power KV175-72M | Kinve Solar Power KV180-72M | KISCO S91E | KISCO S92E | KISCO S93E | KISCO S94E | KISCO S95E | KISCO S96E | KISCO S97E | KISCO S98E | KISCO S99E | KISCO S100E | KISCO S101E | KISCO GETWATT 224P-A1U | KISCO GETWATT 225P-A1U | KISCO GETWATT 226P-A1U | KISCO GETWATT 227P-A1U | KISCO GETWATT 228P-A1U | KISCO GETWATT 229P-A1U | KISCO GETWATT 230P-A1U | KISCO GETWATT 231P-A1U | KISCO GETWATT 232P-A1U | KISCO GETWATT 233P-A1U | KISCO GETWATT 234P-A1U | KISCO GETWATT 235P-A1U | KISCO GETWATT 236P-A1U | KISCO GETWATT 237P-A1U | KISCO GETWATT 238M-A1U | KISCO GETWATT 238P-A1U | KISCO GETWATT 239M-A1U | KISCO GETWATT 239P-A1U | KISCO GETWATT 240M-A1U | KISCO GETWATT 240M-C1U | KISCO GETWATT 240P-A1U | KISCO GETWATT 241M-A1U | KISCO GETWATT 241M-C1U | KISCO GETWATT 241P-A1U | KISCO GETWATT 242M-A1U | KISCO GETWATT 242M-C1U | KISCO GETWATT 242P-A1U | KISCO GETWATT 243M-A1U | KISCO GETWATT 243M-C1U | KISCO GETWATT 243P-A1U | KISCO GETWATT 244M-A1U | KISCO GETWATT 244M-C1U | KISCO GETWATT 244P-A1U | KISCO GETWATT 245M-A1U | KISCO GETWATT 245M-C1U | KISCO GETWATT 245P-A1U | KISCO GETWATT 246M-A1U | KISCO GETWATT 246M-C1U | KISCO GETWATT 247M-A1U | KISCO GETWATT 247M-C1U | KISCO GETWATT 248M-A1U | KISCO GETWATT 248M-C1U | KISCO GETWATT 249M-A1U | KISCO GETWATT 249M-C1U | KISCO GETWATT 250M-A1U | KISCO GETWATT 250M-C1U | KISCO GETWATT 251M-A1U | KISCO GETWATT 251M-C1U | KISCO GETWATT 252M-A1U | KISCO GETWATT 252M-C1U | KISCO GETWATT 253M-A1U | KISCO GETWATT 253M-C1U | KISCO GETWATT 254M-A1U | KISCO GETWATT 254M-C1U | KISCO GETWATT 255M-A1U | KISCO GETWATT 255M-C1U | KISCO GETWATT 256M-A1U | KISCO GETWATT 257M-A1U | KISCO GETWATT 258M-A1U | KISCO GETWATT 259M-A1U | KISCO GETWATT 260M-A1U | KISCO GETWATT 261M-A1U | KISCO GETWATT 262M-A1U | Konca Solar Cell KC5M-170a | Konca Solar Cell KC5M-175a | Konca Solar Cell KC5M-180a | Konca Solar Cell KC6P-215b | Konca Solar Cell KC6P-220b | Konca Solar Cell KC6P-225b | Konca Solar Cell KC6P-230b | Konca Solar Cell KC6P-235b | Kosol Hiramrut Energies KE225 | Kosol Hiramrut Energies KE230 | Kosol Hiramrut Energies KE235 | Kosol Hiramrut Energies KE240 | Kosol Hiramrut Energies KE245 | Kosol Hiramrut Energies KE250 | Kyocera Solar SU53BU | Kyocera Solar KC130GT | Kyocera Solar KC130TM | Kyocera Solar KD130GX-L | Kyocera Solar KD130GX-LFBS | Kyocera Solar KD130GX-LP | Kyocera Solar KD135GX-L | Kyocera Solar KD135GX-LFBS | Kyocera Solar KD135GX-LP | Kyocera Solar KD135GX-LPU | Kyocera Solar KD140GX-LFBS | Kyocera Solar KC175GT | Kyocera Solar KD180GX-L | Kyocera Solar KD180GX-LFBS | Kyocera Solar KD180GX-LP | Kyocera Solar KD185GX-LFBS | Kyocera Solar KD185GX-LPU | Kyocera Solar KD190GX-LFBS | Kyocera Solar KC200GT | Kyocera Solar KD200GX-LPU | Kyocera Solar KD205GX-L | Kyocera Solar KD205GX-LFBS | Kyocera Solar KD205GX-LP | Kyocera Solar KD205GX-LPU | Kyocera Solar KD210GX-L | Kyocera Solar KD210GX-LFBS | Kyocera Solar KD210GX-LP | Kyocera Solar KD210GX-LPU | Kyocera Solar KD215GX-LFBS | Kyocera Solar KD215GX-LPU | Kyocera Solar KD220GX-LFBS | Kyocera Solar KD225GX-LFB | Kyocera Solar KD225GX-LFBS | Kyocera Solar KD225GX-LPB | Kyocera Solar KD230GX-LFB | Kyocera Solar KD230GX-LPB | Kyocera Solar KD235GX-LFB | Kyocera Solar KD235GX-LPB | Kyocera Solar KD240GX-LFB | Kyocera Solar KD240GX-LFB2 | Kyocera Solar KD240GX-LPB | Kyocera Solar KD240GX-LPB2 | Kyocera Solar KD245GX-LFB | Kyocera Solar KD245GX-LFB2 | Kyocera Solar KD245GX-LPB | Kyocera Solar KD245GX-LPB2 | Kyocera Solar KU245-6BCA | Kyocera Solar KD250GX-LFB | Kyocera Solar KD250GX-LFB2 | Kyocera Solar KD250GX-LFB3 | Kyocera Solar KD250GX-LPB | Kyocera Solar KD250GX-LPB2 | Kyocera Solar KD250GX-LPB3 | Kyocera Solar KU250-6BCA | Kyocera Solar KU250-6BPA | Kyocera Solar KU250-6ZPE | Kyocera Solar KD255GX-LFB2 | Kyocera Solar KD255GX-LFB3 | Kyocera Solar KD255GX-LFM | Kyocera Solar KD255GX-LPB2 | Kyocera Solar KD255GX-LPB3 | Kyocera Solar KD255GX-LPM | Kyocera Solar KU255-6BCA | Kyocera Solar KU255-6BPA | Kyocera Solar KU255-6MCA | Kyocera Solar KU255-6MCB | Kyocera Solar KU255-6MPA | Kyocera Solar KU255-6MPB | Kyocera Solar KU255-6XCA | Kyocera Solar KU255-6XPA | Kyocera Solar KU255-6ZCA | Kyocera Solar KU255-6ZPA | Kyocera Solar KU255-6ZPB | Kyocera Solar KU255-6ZPE | Kyocera Solar KD260GX-LFB2 | Kyocera Solar KD260GX-LFM | Kyocera Solar KD260GX-LPB2 | Kyocera Solar KD260GX-LPM | Kyocera Solar KU260-6BCA | Kyocera Solar KU260-6BPA | Kyocera Solar KU260-6MCA | Kyocera Solar KU260-6MCB | Kyocera Solar KU260-6MPA | Kyocera Solar KU260-6MPB | Kyocera Solar KU260-6XCA | Kyocera Solar KU260-6XPA | Kyocera Solar KU260-6ZCA | Kyocera Solar KU260-6ZPA | Kyocera Solar KU260-6ZPB | Kyocera Solar KU260-6ZPC | Kyocera Solar KU260-6ZPE | Kyocera Solar KD265GX-LFB2 | Kyocera Solar KD265GX-LFM | Kyocera Solar KD265GX-LPB2 | Kyocera Solar KD265GX-LPM | Kyocera Solar KU265-6BCA | Kyocera Solar KU265-6BPA | Kyocera Solar KU265-6MCA | Kyocera Solar KU265-6MCB | Kyocera Solar KU265-6MPA | Kyocera Solar KU265-6MPB | Kyocera Solar KU265-6XCA | Kyocera Solar KU265-6XPA | Kyocera Solar KU265-6ZCA | Kyocera Solar KU265-6ZPA | Kyocera Solar KU265-6ZPB | Kyocera Solar KU265-6ZPC | Kyocera Solar KU265-6ZPE | Kyocera Solar KD270GX-LFB2 | Kyocera Solar KD270GX-LFM | Kyocera Solar KD270GX-LPB2 | Kyocera Solar KD270GX-LPM | Kyocera Solar KU270-6BCA | Kyocera Solar KU270-6BPA | Kyocera Solar KU270-6MCA | Kyocera Solar KU270-6MCB | Kyocera Solar KU270-6MPA | Kyocera Solar KU270-6MPB | Kyocera Solar KU270-6XCA | Kyocera Solar KU270-6XPA | Kyocera Solar KU270-6ZCA | Kyocera Solar KU270-6ZPA | Kyocera Solar KU270-6ZPB | Kyocera Solar KU270-6ZPC | Kyocera Solar KU270-6ZPE | Kyocera Solar KD300GX-LFB | Kyocera Solar KD300GX-LPB | Kyocera Solar KD305GX-LFB | Kyocera Solar KD305GX-LPB | Kyocera Solar KD310GX-LFB | Kyocera Solar KD310GX-LPB | Kyocera Solar KD315GX-LFB | Kyocera Solar KD315GX-LPB | Kyocera Solar KU315-7ZCA | Kyocera Solar KU315-7ZPA | Kyocera Solar KD320GX-LFB | Kyocera Solar KD320GX-LPB | Kyocera Solar KU320-7ZCA | Kyocera Solar KU320-7ZPA | Kyocera Solar KU320-8BCA | Kyocera Solar KD325GX-LFB | Kyocera Solar KD325GX-LPB | Kyocera Solar KU325-7ZCA | Kyocera Solar KU325-7ZPA | Kyocera Solar KU325-8BCA | Kyocera Solar KU325-8BPA | Kyocera Solar KD330GX-LFB | Kyocera Solar KD330GX-LPB | Kyocera Solar KU330-7ZCA | Kyocera Solar KU330-7ZPA | Kyocera Solar KU330-8BCA | Kyocera Solar KU330-8BPA | Kyocera Solar KD335GX-LFB | Kyocera Solar KD335GX-LPB | Kyocera Solar KU335-7ZCA | Kyocera Solar KU335-7ZPA | Kyocera Solar KU335-8BCA | Kyocera Solar KU335-8BPA | Kyocera Solar KD340GX-LFB | Kyocera Solar KU340-8BCA | Kyung Won KWL-210 S | Kyung Won KWL-220 S | Kyung Won KWL-230 S | Kyung Won KWL-240 S | Kyung Won KWL-250 S | LDK Solar LDK-170D-24 | LDK Solar LDK-175D-24 | LDK Solar LDK-180D-24 | LDK Solar LDK-180P-24(S) | LDK Solar LDK-185P-24(S) | LDK Solar LDK-190D-24(S) | LDK Solar LDK-190P-18 | LDK Solar LDK-190P-24(S) | LDK Solar LDK-195D-24(S) | LDK Solar LDK-200D-24(S) | LDK Solar LDK-200P-18 | LDK Solar LDK-210P-18 | LDK Solar LDK-210P-20 | LDK Solar LDK-220D-20 | LDK Solar LDK-220P-20 | LDK Solar LDK-225P-20 | LDK Solar LDK-230D-20 | LDK Solar LDK-230P-20 | LDK Solar LDK-235D-20 | LDK Solar LDK-235P-20 | LDK Solar LDK-240P-20 | LDK Solar LDK-245P-20 | LDK Solar LDK245PABB | LDK Solar LDK245PABW | LDK Solar LDK245PAFB | LDK Solar LDK245PAFW | LDK Solar LDK-250P-20 | LDK Solar LDK250PABB | LDK Solar LDK250PABW | LDK Solar LDK250PAFB | LDK Solar LDK250PAFW | LDK Solar LDK-255D-20 | LDK Solar LDK-255P-20 | LDK Solar LDK255PABB | LDK Solar LDK255PABW | LDK Solar LDK255PAFB | LDK Solar LDK255PAFW | LDK Solar LDK-260P-24 | LDK Solar LDK260PABB | LDK Solar LDK260PABW | LDK Solar LDK260PAFB | LDK Solar LDK260PAFW | LDK Solar LDK-270P-24 | LDK Solar LDK-275P-24 | LDK Solar LDK-280P-24 | LDK Solar LDK-285P-24 | LDK Solar LDK-290P-24 | LDK Solar LDK-295P-24 | LERRI Solar Technology Co. LR6-72-315M | LERRI Solar Technology Co. LR6-72-320M | LERRI Solar Technology Co. LR6-72-325M | LERRI Solar Technology Co. LR6-72-330M | LERRI Solar Technology Co. LR6-72-335M | LERRI Solar Technology Co. LR6-72-340M | LERRI Solar Technology Co. LR6-72-345M | LG Electronics Inc. LG210P1C-G2 | LG Electronics Inc. LG210P1W-G1 | LG Electronics Inc. LG215P1C-G2 | LG Electronics Inc. LG215P1W | LG Electronics Inc. LG215P1W-G1 | LG Electronics Inc. LG220M1C-G2 | LG Electronics Inc. LG220P1C-G2 | LG Electronics Inc. LG220P1W | LG Electronics Inc. LG220P1W-G1 | LG Electronics Inc. LG220R1C-G2 | LG Electronics Inc. LG220R1W-G2 | LG Electronics Inc. LG225M1C-G2 | LG Electronics Inc. LG225P1C-G2 | LG Electronics Inc. LG225P1W | LG Electronics Inc. LG225P1W-G1 | LG Electronics Inc. LG225R1C-G2 | LG Electronics Inc. LG225R1W-G2 | LG Electronics Inc. LG230M1C-G2 | LG Electronics Inc. LG230N8K-G4 | LG Electronics Inc. LG230P1C-G2 | LG Electronics Inc. LG230P1W | LG Electronics Inc. LG230P1W-G1 | LG Electronics Inc. LG230R1C-G2 | LG Electronics Inc. LG230R1W-G2 | LG Electronics Inc. LG235M1C-G2 | LG Electronics Inc. LG235N8K-G4 | LG Electronics Inc. LG235P1W | LG Electronics Inc. LG235R1C-G2 | LG Electronics Inc. LG235R1W-G2 | LG Electronics Inc. LG240M1C-G2 | LG Electronics Inc. LG240N8K-G4 | LG Electronics Inc. LG240R1C-G2 | LG Electronics Inc. LG240R1W-G2 | LG Electronics Inc. LG240S1C-G2 | LG Electronics Inc. LG240S1K-G3 | LG Electronics Inc. LG245M1C-G2 | LG Electronics Inc. LG245M1W-G2 | LG Electronics Inc. LG245N8K-G4 | LG Electronics Inc. LG245S1C-G2 | LG Electronics Inc. LG245S1C-G3 | LG Electronics Inc. LG245S1K-G3 | LG Electronics Inc. LG250N8K-G4 | LG Electronics Inc. LG250S1C-G2 | LG Electronics Inc. LG250S1C-G3 | LG Electronics Inc. LG250S1K-A3 | LG Electronics Inc. LG250S1K-B3 | LG Electronics Inc. LG250S1K-G3 | LG Electronics Inc. LG255S1C-A3 | LG Electronics Inc. LG255S1C-B3 | LG Electronics Inc. LG255S1C-G2 | LG Electronics Inc. LG255S1C-G3 | LG Electronics Inc. LG255S1K-A3 | LG Electronics Inc. LG255S1K-B3 | LG Electronics Inc. LG255S1K-G3 | LG Electronics Inc. LG255S1W-A3 | LG Electronics Inc. LG255S1W-B3 | LG Electronics Inc. LG260N9K-G4 | LG Electronics Inc. LG260S1C-A3 | LG Electronics Inc. LG260S1C-B3 | LG Electronics Inc. LG260S1C-G2 | LG Electronics Inc. LG260S1C-G3 | LG Electronics Inc. LG260S1K-A3 | LG Electronics Inc. LG260S1K-B3 | LG Electronics Inc. LG260S1K-G3 | LG Electronics Inc. LG260S1W-A3 | LG Electronics Inc. LG260S1W-B3 | LG Electronics Inc. LG260S1W-G2 | LG Electronics Inc. LG260S1W-G3 | LG Electronics Inc. LG265N9K-G4 | LG Electronics Inc. LG265S1C-A3 | LG Electronics Inc. LG265S1C-B3 | LG Electronics Inc. LG265S1C-G3 | LG Electronics Inc. LG265S1K-A3 | LG Electronics Inc. LG265S1K-B3 | LG Electronics Inc. LG265S1W-A3 | LG Electronics Inc. LG265S1W-B3 | LG Electronics Inc. LG265S1W-G3 | LG Electronics Inc. LG270N1C-G3 | LG Electronics Inc. LG270N1W-G3 | LG Electronics Inc. LG270N9K-G4 | LG Electronics Inc. LG270S1C-A3 | LG Electronics Inc. LG270S1C-B3 | LG Electronics Inc. LG270S1C-G3 | LG Electronics Inc. LG270S1C-G4 | LG Electronics Inc. LG270S1C-L4 | LG Electronics Inc. LG270S1K-B3 | LG Electronics Inc. LG270S1W-A3 | LG Electronics Inc. LG270S1W-B3 | LG Electronics Inc. LG270S1W-G3 | LG Electronics Inc. LG270S1W-G4 | LG Electronics Inc. LG270S1W-L4 | LG Electronics Inc. LG275N1C-G3 | LG Electronics Inc. LG275N1K-A3 | LG Electronics Inc. LG275N1K-B3 | LG Electronics Inc. LG275N1W-G3 | LG Electronics Inc. LG275N9K-G4 | LG Electronics Inc. LG275S1C-B3 | LG Electronics Inc. LG275S1C-G4 | LG Electronics Inc. LG275S1C-L4 | LG Electronics Inc. LG275S1K-B3 | LG Electronics Inc. LG275S1W-B3 | LG Electronics Inc. LG275S1W-G4 | LG Electronics Inc. LG275S1W-L4 | LG Electronics Inc. LG280N1C-G3 | LG Electronics Inc. LG280N1K-A3 | LG Electronics Inc. LG280N1K-B3 | LG Electronics Inc. LG280N1W-G3 | LG Electronics Inc. LG280N9K-G4 | LG Electronics Inc. LG280S1C-A5 | LG Electronics Inc. LG280S1C-B3 | LG Electronics Inc. LG280S1C-G4 | LG Electronics Inc. LG280S1C-L4 | LG Electronics Inc. LG280S1W-A5 | LG Electronics Inc. LG280S1W-B3 | LG Electronics Inc. LG280S1W-G4 | LG Electronics Inc. LG280S1W-L4 | LG Electronics Inc. LG285N1C-A3 | LG Electronics Inc. LG285N1C-B3 | LG Electronics Inc. LG285N1C-G3 | LG Electronics Inc. LG285N1K-A3 | LG Electronics Inc. LG285N1K-B3 | LG Electronics Inc. LG285N1W-A3 | LG Electronics Inc. LG285N1W-B3 | LG Electronics Inc. LG285N1W-G3 | LG Electronics Inc. LG285S1C-A5 | LG Electronics Inc. LG285S1C-G4 | LG Electronics Inc. LG285S1C-L4 | LG Electronics Inc. LG285S1W-A5 | LG Electronics Inc. LG285S1W-G4 | LG Electronics Inc. LG285S1W-L4 | LG Electronics Inc. LG290N1C-A3 | LG Electronics Inc. LG290N1C-B3 | LG Electronics Inc. LG290N1C-G3 | LG Electronics Inc. LG290N1K-A3 | LG Electronics Inc. LG290N1K-B3 | LG Electronics Inc. LG290N1K-Z4 | LG Electronics Inc. LG290N1T-A4 | LG Electronics Inc. LG290N1W-A3 | LG Electronics Inc. LG290N1W-B3 | LG Electronics Inc. LG290N1W-G3 | LG Electronics Inc. LG290S1C-A5 | LG Electronics Inc. LG290S1C-G4 | LG Electronics Inc. LG290S1C-L4 | LG Electronics Inc. LG290S1W-A5 | LG Electronics Inc. LG290S1W-G4 | LG Electronics Inc. LG290S1W-L4 | LG Electronics Inc. LG295A1C-B3 | LG Electronics Inc. LG295A1W-B3 | LG Electronics Inc. LG295N1C-A3 | LG Electronics Inc. LG295N1C-B3 | LG Electronics Inc. LG295N1C-G3 | LG Electronics Inc. LG295N1C-G4 | LG Electronics Inc. LG295N1K-A3 | LG Electronics Inc. LG295N1K-B3 | LG Electronics Inc. LG295N1K-G4 | LG Electronics Inc. LG295N1K-Z4 | LG Electronics Inc. LG295N1T-A4 | LG Electronics Inc. LG295N1W-A3 | LG Electronics Inc. LG295N1W-B3 | LG Electronics Inc. LG295N1W-G3 | LG Electronics Inc. LG295N1W-G4 | LG Electronics Inc. LG295S1C-A5 | LG Electronics Inc. LG295S1C-G4 | LG Electronics Inc. LG295S1W-A5 | LG Electronics Inc. LG295S1W-G4 | LG Electronics Inc. LG300A1C-B3 | LG Electronics Inc. LG300A1W-B3 | LG Electronics Inc. LG300N1C-A3 | LG Electronics Inc. LG300N1C-B3 | LG Electronics Inc. LG300N1C-G3 | LG Electronics Inc. LG300N1C-G4 | LG Electronics Inc. LG300N1C-Z4 | LG Electronics Inc. LG300N1K-G4 | LG Electronics Inc. LG300N1K-Z4 | LG Electronics Inc. LG300N1T-A4 | LG Electronics Inc. LG300N1W-A3 | LG Electronics Inc. LG300N1W-B3 | LG Electronics Inc. LG300N1W-G3 | LG Electronics Inc. LG300N1W-G4 | LG Electronics Inc. LG300S1C-A5 | LG Electronics Inc. LG300S1W-A5 | LG Electronics Inc. LG305A1C-B3 | LG Electronics Inc. LG305A1W-B3 | LG Electronics Inc. LG305N1C-B3 | LG Electronics Inc. LG305N1C-G4 | LG Electronics Inc. LG305N1C-Z4 | LG Electronics Inc. LG305N1K-G4 | LG Electronics Inc. LG305N1K-Z4 | LG Electronics Inc. LG305N1T-A4 | LG Electronics Inc. LG305N1T-A5 | LG Electronics Inc. LG305N1W-B3 | LG Electronics Inc. LG305N1W-G4 | LG Electronics Inc. LG305S1C-A5 | LG Electronics Inc. LG305S1W-A5 | LG Electronics Inc. LG310N1C-B3 | LG Electronics Inc. LG310N1C-G4 | LG Electronics Inc. LG310N1C-Z4 | LG Electronics Inc. LG310N1K-A5 | LG Electronics Inc. LG310N1K-G4 | LG Electronics Inc. LG310N1K-Z4 | LG Electronics Inc. LG310N1T-A4 | LG Electronics Inc. LG310N1T-A5 | LG Electronics Inc. LG310N1W-B3 | LG Electronics Inc. LG310N1W-G4 | LG Electronics Inc. LG315E1K-A5 | LG Electronics Inc. LG315N1C-G4 | LG Electronics Inc. LG315N1C-Z4 | LG Electronics Inc. LG315N1K-A5 | LG Electronics Inc. LG315N1K-G4 | LG Electronics Inc. LG315N1K-V5 | LG Electronics Inc. LG315N1K-Z4 | LG Electronics Inc. LG315N1T-A4 | LG Electronics Inc. LG315N1T-A5 | LG Electronics Inc. LG315N1W-G4 | LG Electronics Inc. LG320E1K-A5 | LG Electronics Inc. LG320N1C-A5 | LG Electronics Inc. LG320N1C-G4 | LG Electronics Inc. LG320N1C-Z4 | LG Electronics Inc. LG320N1C-Z5 | LG Electronics Inc. LG320N1K-A5 | LG Electronics Inc. LG320N1K-G4 | LG Electronics Inc. LG320N1K-V5 | LG Electronics Inc. LG320N1K-Z4 | LG Electronics Inc. LG320N1T-A5 | LG Electronics Inc. LG320N1W-A5 | LG Electronics Inc. LG320N1W-G4 | LG Electronics Inc. LG320S2C-G4 | LG Electronics Inc. LG320S2W-G4 | LG Electronics Inc. LG325E1C-A5 | LG Electronics Inc. LG325E1K-A5 | LG Electronics Inc. LG325N1C-A5 | LG Electronics Inc. LG325N1C-G4 | LG Electronics Inc. LG325N1C-V5 | LG Electronics Inc. LG325N1C-Z4 | LG Electronics Inc. LG325N1C-Z5 | LG Electronics Inc. LG325N1K-A5 | LG Electronics Inc. LG325N1K-V5 | LG Electronics Inc. LG325N1T-A5 | LG Electronics Inc. LG325N1W-A5 | LG Electronics Inc. LG325N1W-G4 | LG Electronics Inc. LG325N1W-V5 | LG Electronics Inc. LG325S2C-G4 | LG Electronics Inc. LG325S2W-G4 | LG Electronics Inc. LG330E1C-A5 | LG Electronics Inc. LG330N1C-A5 | LG Electronics Inc. LG330N1C-V5 | LG Electronics Inc. LG330N1C-Z4 | LG Electronics Inc. LG330N1C-Z5 | LG Electronics Inc. LG330N1K-A5 | LG Electronics Inc. LG330N1T-A5 | LG Electronics Inc. LG330N1W-A5 | LG Electronics Inc. LG330N1W-V5 | LG Electronics Inc. LG330Q1K-A5 | LG Electronics Inc. LG330S2C-G4 | LG Electronics Inc. LG330S2W-G4 | LG Electronics Inc. LG333N1C-A5 | LG Electronics Inc. LG333N1W-A5 | LG Electronics Inc. LG335E1C-A5 | LG Electronics Inc. LG335N1C-A5 | LG Electronics Inc. LG335N1C-V5 | LG Electronics Inc. LG335N1C-Z5 | LG Electronics Inc. LG335N1K-A5 | LG Electronics Inc. LG335N1T-A5 | LG Electronics Inc. LG335N1W-A5 | LG Electronics Inc. LG335N1W-V5 | LG Electronics Inc. LG335Q1K-A5 | LG Electronics Inc. LG335S2C-G4 | LG Electronics Inc. LG335S2W-G4 | LG Electronics Inc. LG340N1C-A5 | LG Electronics Inc. LG340N1C-V5 | LG Electronics Inc. LG340N1C-Z5 | LG Electronics Inc. LG340N1W-A5 | LG Electronics Inc. LG340N1W-V5 | LG Electronics Inc. LG340Q1C-A5 | LG Electronics Inc. LG340Q1K-A5 | LG Electronics Inc. LG340S2C-G4 | LG Electronics Inc. LG340S2W-A5 | LG Electronics Inc. LG340S2W-G4 | LG Electronics Inc. LG345N1C-A5 | LG Electronics Inc. LG345N1C-Z5 | LG Electronics Inc. LG345N1W-A5 | LG Electronics Inc. LG345Q1C-A5 | LG Electronics Inc. LG345Q1K-A5 | LG Electronics Inc. LG345S2C-G4 | LG Electronics Inc. LG345S2W-A5 | LG Electronics Inc. LG345S2W-G4 | LG Electronics Inc. LG350N2C-B3 | LG Electronics Inc. LG350N2T-A4 | LG Electronics Inc. LG350N2W-B3 | LG Electronics Inc. LG350Q1C-A5 | LG Electronics Inc. LG350Q1K-A5 | LG Electronics Inc. LG350S2W-A5 | LG Electronics Inc. LG355A1C-A5 | LG Electronics Inc. LG355N2C-B3 | LG Electronics Inc. LG355N2T-A4 | LG Electronics Inc. LG355N2W-B3 | LG Electronics Inc. LG355Q1C-A5 | LG Electronics Inc. LG355Q1K-A5 | LG Electronics Inc. LG355S2W-A5 | LG Electronics Inc. LG360A1C-A5 | LG Electronics Inc. LG360N2C-B3 | LG Electronics Inc. LG360N2C-G4 | LG Electronics Inc. LG360N2K-G4 | LG Electronics Inc. LG360N2T-A4 | LG Electronics Inc. LG360N2W-B3 | LG Electronics Inc. LG360N2W-G4 | LG Electronics Inc. LG360Q1C-A5 | LG Electronics Inc. LG360Q1K-A5 | LG Electronics Inc. LG360S2W-A5 | LG Electronics Inc. LG365A1C-A5 | LG Electronics Inc. LG365N2C-B3 | LG Electronics Inc. LG365N2C-G4 | LG Electronics Inc. LG365N2K-G4 | LG Electronics Inc. LG365N2T-A4 | LG Electronics Inc. LG365N2W-B3 | LG Electronics Inc. LG365N2W-G4 | LG Electronics Inc. LG365Q1C-A5 | LG Electronics Inc. LG365S2W-A5 | LG Electronics Inc. LG370A1C-A5 | LG Electronics Inc. LG370N2C-B3 | LG Electronics Inc. LG370N2C-G4 | LG Electronics Inc. LG370N2K-G4 | LG Electronics Inc. LG370N2T-A4 | LG Electronics Inc. LG370N2T-A5 | LG Electronics Inc. LG370N2W-B3 | LG Electronics Inc. LG370N2W-G4 | LG Electronics Inc. LG370Q1C-A5 | LG Electronics Inc. LG370S2W-A5 | LG Electronics Inc. LG375N2C-B3 | LG Electronics Inc. LG375N2C-G4 | LG Electronics Inc. LG375N2K-A5 | LG Electronics Inc. LG375N2K-G4 | LG Electronics Inc. LG375N2T-A4 | LG Electronics Inc. LG375N2T-A5 | LG Electronics Inc. LG375N2W-B3 | LG Electronics Inc. LG375N2W-G4 | LG Electronics Inc. LG380N2C-A5 | LG Electronics Inc. LG380N2C-G4 | LG Electronics Inc. LG380N2K-A5 | LG Electronics Inc. LG380N2K-G4 | LG Electronics Inc. LG380N2T-A4 | LG Electronics Inc. LG380N2T-A5 | LG Electronics Inc. LG380N2W-A5 | LG Electronics Inc. LG380N2W-G4 | LG Electronics Inc. LG385N2C-A5 | LG Electronics Inc. LG385N2C-G4 | LG Electronics Inc. LG385N2K-A5 | LG Electronics Inc. LG385N2T-A5 | LG Electronics Inc. LG385N2W-A5 | LG Electronics Inc. LG385N2W-G4 | LG Electronics Inc. LG390N2C-A5 | LG Electronics Inc. LG390N2K-A5 | LG Electronics Inc. LG390N2T-A5 | LG Electronics Inc. LG390N2W-A5 | LG Electronics Inc. LG390N2W-V5 | LG Electronics Inc. LG395N2C-A5 | LG Electronics Inc. LG395N2K-A5 | LG Electronics Inc. LG395N2T-A5 | LG Electronics Inc. LG395N2W-A5 | LG Electronics Inc. LG395N2W-V5 | LG Electronics Inc. LG400N2C-A5 | LG Electronics Inc. LG400N2K-A5 | LG Electronics Inc. LG400N2T-A5 | LG Electronics Inc. LG400N2W-A5 | LG Electronics Inc. LG400N2W-V5 | LG Electronics Inc. LG405N2C-A5 | LG Electronics Inc. LG405N2K-A5 | LG Electronics Inc. LG405N2W-A5 | LG Electronics Inc. LG405N2W-V5 | LG Electronics Inc. LG410N2C-A5 | LG Electronics Inc. LG410N2W-A5 | Lifeline Energy LL60B-245-P3 | Lifeline Energy LFUS-250M | Lifeline Energy LL60B-250-P3 | Lifeline Energy LL60C-250-P3 | Lifeline Energy LF60C-255-M3 | Lifeline Energy LL60B-255-P3 | Lifeline Energy LL60C-255-P3 | Lifeline Energy LF60C-260-M3 | Lifeline Energy LL60B-260-P3 | Lifeline Energy LL60C-260-P3 | Lifeline Energy LF60C-265-M3 | Lifeline Energy LL60B-265-P3 | Lifeline Energy LL60C-265-P3 | Lifeline Energy LF60C-270-M3 | Lifeline Energy LL60B-270-P3 | Lifeline Energy LL60C-270-P3 | Lifeline Energy LFUS-300M | Lifeline Energy LL72C-300-P3 | Lifeline Energy LL72C-305-P3 | Lifeline Energy LL72C-310-P3 | Lifeline Energy LL72C-315-P3 | Lifeline Energy LL72C-320-P3 | Lifeline Energy LL72C-325-P3 | Lifeline Energy LL72C-330-P3 | Lifeline Energy International LF-165WP | Lifeline Energy International LF-170WP | Lifeline Energy International LLE-5M170 | Lifeline Energy International LF-175WP | Lifeline Energy International LLE-5M175 | Lifeline Energy International LF-180WP | Lifeline Energy International LLE-5M180 | Lifeline Energy International LLE-5M185 | Lifeline Energy International LLE-5M190 | Lifeline Energy International LLE-5M195 | Lifeline Energy International LF-200WP | Lifeline Energy International LLE-6M205 | Lifeline Energy International LF-210WP | Lifeline Energy International LLE-6M210 | Lifeline Energy International LF-220WP | Lifeline Energy International LLE-6M220 | Lifeline Energy International LLE-6M225 | Lifeline Energy International LF-230WP | Lifeline Energy International LLE-6M230 | Lifeline Energy International LLE-6M235 | Lifeline Energy International LLE-6M240 | Lifeline Energy International LLE-6M245 | Lifeline Energy International LF-250WP | Lifeline Energy International LLE-6M250 | Lifeline Energy International LLE-6M255 | Lifeline Energy International LLE-6P255 | Lifeline Energy International LF-260WP | Lifeline Energy International LLE-6M260 | Lifeline Energy International LLE-6P260 | Lifeline Energy International LLE-6P265 | Lifeline Energy International LF-270WP | Lifeline Energy International LLE-6P270 | Lifeline Energy International LLE-6P275 | Lifeline Energy International LF-280WP | Lifeline Energy International LLE-6M280 | Lifeline Energy International LLE-6P280 | Lifeline Energy International LLE-6M285 | Lifeline Energy International LLE-6P285 | Lifeline Energy International LLE-6M290 | Lifeline Energy International LLE-6P290 | Lifeline Energy International LLE-6M295 | Lifeline Energy International LLE-6M300 | Lifeline Energy International LLE-6M305 | Lifeline Energy International LLE-6M310 | Lifeline Energy International LLE-6M315 | Lifeline Energy USA LFUS-200-p | Lifeline Energy USA LFUS-205-p | Lightway Green New Energy LW165(23)P1310x990 | Lightway Green New Energy LW170(23)P1310x990 | Lightway Green New Energy LW175(23)P1310x990 | Lightway Green New Energy LW180(23)P1310x990 | Lightway Green New Energy LW185(23)P1310x990 | Lightway Green New Energy LW190(23)P1310x990 | Lightway Green New Energy LW200(29)P1650x990 | Lightway Green New Energy LW205(29)P1650x990 | Lightway Green New Energy LW210(29)P1650x990 | Lightway Green New Energy LW215(29)P1650x990 | Lightway Green New Energy LW220(29)P1650x990 | Lightway Green New Energy LW225(29)P1650x990 | Lightway Green New Energy LW230(29)P1650x990 | Lightway Green New Energy LW235(29)P1650x990 | Lightway Green New Energy LW240(29)P1640x990 | Lightway Green New Energy LW240(29)P1650x990 | Lightway Green New Energy LW245(29)P1640x990 | Lightway Green New Energy LW245(29)P1650x990 | Lightway Green New Energy LW250(29)P1640x990 | Lightway Green New Energy LW250(29)P1650x990 | Lightway Green New Energy LW255(29)P1640x990 | Lightway Green New Energy LW255(29)P1650x990 | Lightway Green New Energy LW260(29)P1640x990 | Lightway Green New Energy LW260(29)P1650x990 | Lightway Green New Energy LW265(29)P1640x990 | Lightway Green New Energy LW265(29)P1650x990 | Lightway Green New Energy LW280(35)P1970x990 | Lightway Green New Energy LW285(35)P1970x990 | Lightway Green New Energy LW290(35)P1960x990 | Lightway Green New Energy LW290(35)P1970x990 | Lightway Green New Energy LW295(35)P1960x990 | Lightway Green New Energy LW295(35)P1970x990 | Lightway Green New Energy LW300(35)P1960x990 | Lightway Green New Energy LW300(35)P1970x990 | Lightway Green New Energy LW305(35)P1960x990 | Lightway Green New Energy LW305(35)P1970x990 | Lightway Green New Energy LW310(35)P1960x990 | Lightway Green New Energy LW310(35)P1970x990 | Lightway Green New Energy LW315(35)P1960x990 | Lightway Green New Energy LW315(35)P1970x990 | Ligitek Photovoltaic LG052BB00 | Ligitek Photovoltaic LM175AA00 | Ligitek Photovoltaic LM175BB00 | Ligitek Photovoltaic LM180AA00 | Ligitek Photovoltaic LM180BB00 | Ligitek Photovoltaic LM185AA00 | Ligitek Photovoltaic LM185BB00 | Ligitek Photovoltaic LM210BB00 | Ligitek Photovoltaic LM215BB00 | Ligitek Photovoltaic LM220BB00 | Ligitek Photovoltaic LM225BB00 | Ligitek Photovoltaic LM230BB00 | Ligitek Photovoltaic LM235BB00 | Ligitek Photovoltaic LM240BB00 | Ligitek Photovoltaic LM265BB02 | Ligitek Photovoltaic LM270BB02 | Ligitek Photovoltaic LM275BB02 | Ligitek Photovoltaic LM280BB02 | Ligitek Photovoltaic LM285BB02 | LONGi Green Energy Technology Co._ Ltd. LR6-60-270M | LONGi Green Energy Technology Co._ Ltd. LR6-60-275M | LONGi Green Energy Technology Co._ Ltd. LR6-60-280M | LONGi Green Energy Technology Co._ Ltd. LR6-60PB-280M | LONGi Green Energy Technology Co._ Ltd. LR6-60PE-280M | LONGi Green Energy Technology Co._ Ltd. LR6-60-285M | LONGi Green Energy Technology Co._ Ltd. LR6-60PB-285M | LONGi Green Energy Technology Co._ Ltd. LR6-60PE-285M | LONGi Green Energy Technology Co._ Ltd. LR6-60-290M | LONGi Green Energy Technology Co._ Ltd. LR6-60PB-290M | LONGi Green Energy Technology Co._ Ltd. LR6-60PE-290M | LONGi Green Energy Technology Co._ Ltd. LR6-60-295M | LONGi Green Energy Technology Co._ Ltd. LR6-60PB-295M | LONGi Green Energy Technology Co._ Ltd. LR6-60PE-295M | LONGi Green Energy Technology Co._ Ltd. LR6-60PB-300M | LONGi Green Energy Technology Co._ Ltd. LR6-60PE-300M | LONGi Green Energy Technology Co._ Ltd. LR6-60PE-305M | LONGi Green Energy Technology Co._ Ltd. LR6-72-320M | LONGi Green Energy Technology Co._ Ltd. LR6-72HV-320M | LONGi Green Energy Technology Co._ Ltd. LR6-72-325M | LONGi Green Energy Technology Co._ Ltd. LR6-72HV-325M | LONGi Green Energy Technology Co._ Ltd. LR6-72-330M | LONGi Green Energy Technology Co._ Ltd. LR6-72HV-330M | LONGi Green Energy Technology Co._ Ltd. LR6-72-335M | LONGi Green Energy Technology Co._ Ltd. LR6-72HV-335M | LONGi Green Energy Technology Co._ Ltd. LR6-72-340M | LONGi Green Energy Technology Co._ Ltd. LR6-72HV-340M | LONGi Green Energy Technology Co._ Ltd. LR6-72PE-340M | LONGi Green Energy Technology Co._ Ltd. LR6-72PH-340M | LONGi Green Energy Technology Co._ Ltd. LR6-72-345M | LONGi Green Energy Technology Co._ Ltd. LR6-72HV-345M | LONGi Green Energy Technology Co._ Ltd. LR6-72PE-345M | LONGi Green Energy Technology Co._ Ltd. LR6-72PH-345M | LONGi Green Energy Technology Co._ Ltd. LR6-72BP-350M | LONGi Green Energy Technology Co._ Ltd. LR6-72HV-350M | LONGi Green Energy Technology Co._ Ltd. LR6-72PE-350M | LONGi Green Energy Technology Co._ Ltd. LR6-72PH-350M | LONGi Green Energy Technology Co._ Ltd. LR6-72BP-355M | LONGi Green Energy Technology Co._ Ltd. LR6-72PE-355M | LONGi Green Energy Technology Co._ Ltd. LR6-72PH-355M | LONGi Green Energy Technology Co._ Ltd. LR6-72BP-360M | LONGi Green Energy Technology Co._ Ltd. LR6-72PE-360M | LONGi Green Energy Technology Co._ Ltd. LR6-72PH-360M | LONGi Green Energy Technology Co._ Ltd. LR6-72BP-365M | LONGi Green Energy Technology Co._ Ltd. LR6-72PE-365M | LONGi Green Energy Technology Co._ Ltd. LR6-72PH-365M | LONGi Green Energy Technology Co._ Ltd. LR6-72BP-370M | LONGi Green Energy Technology Co._ Ltd. LR6-72PE-370M | LONGi Green Energy Technology Co._ Ltd. LR6-72PH-370M | LONGi Green Energy Technology Co._ Ltd. LR6-72PH-375M | LS Industrial Systems PVM S228 | LS Industrial Systems PVM S229 | LS Industrial Systems PVM S230 | LS Industrial Systems PVM S231 | LS Industrial Systems PVM S232 | LS Industrial Systems PVM S233 | LS Industrial Systems PVM S234 | LS Industrial Systems PVM S235 | LS Industrial Systems PVM S236 | LS Industrial Systems PVM S237 | LS Industrial Systems PVM S238 | LS Industrial Systems PVM S239 | LS Industrial Systems PVM S240 | LS Industrial Systems PVM S241 | LS Industrial Systems PVM S242 | LS Industrial Systems PVM S243 | LS Industrial Systems PVM S244 | LS Industrial Systems PVM S245 | Lubi Electronics LE18P230 | Lubi Electronics LE18P240 | Lubi Electronics LE18P250 | Lucky Power Technology LPS-6P6A-220-B | Lucky Power Technology LPS-6P6A-225-B | Lucky Power Technology LPS-6P6A-230-B | Lucky Power Technology LPS-6P6A-235-B | Lucky Power Technology LPS-6P6A-240-B | LUMA Resources LRSS | Lumeta LEF028B | Lumeta LES028B | Lumeta LPP-165 | Lumeta LPP-170 | Lumeta LPP-175 | Lumeta LPP-175T | Lumeta LPP-180 | Lumeta LPP-180T | Lumeta LPP-185T | Lumeta LPP-190T | Lumeta LPP-195T | Lumeta LPP400A | Lumos LS175-72M-J | Lumos LSX175-72M-B | Lumos LSX175-72M-C | Lumos LSX175-72M-W | Lumos LS180-72M-J | Lumos LSX180-72M-B | Lumos LSX180-72M-C | Lumos LSX180-72M-W | Lumos LS185-72M | Lumos LS185-72M-J | Lumos LSX185-72M-B | Lumos LSX185-72M-C | Lumos LSX185-72M-W | Lumos LS190-72M | Lumos LS190-72M-J | Lumos LSX190-72M-B | Lumos LSX190-72M-C | Lumos LSX190-72M-W | Lumos LS195-72M-B | Lumos LS195-72M-J | Lumos LSX195-72M-B | Lumos LSX195-72M-C | Lumos LSX195-72M-W | Lumos LS200-72M-B | Lumos LS200-72M-J | Lumos LSX200-72M-B | Lumos LSX200-72M-C | Lumos LSX200-72M-W | Lumos LS205-72M-J | Lumos SST215-54M | Lumos SST215-54M-BB | Lumos LS220-60M | Lumos LS220-60M-J | Lumos LS220-60P-J | Lumos SST220-54M | Lumos SST220-54M-BB | Lumos SST220-60P | Lumos LS225-60M | Lumos LS225-60M-J | Lumos LS225-60P-J | Lumos LSX225-60M-B | Lumos LSX225-60M-C | Lumos LSX225-60M-W | Lumos SST225-54M | Lumos SST225-54M-BB | Lumos SST225-60P | Lumos LS230-60M | Lumos LS230-60M-J | Lumos LS230-60P-J | Lumos LSX230-60M-B | Lumos LSX230-60M-C | Lumos LSX230-60M-W | Lumos SST230-60P | Lumos LCX235-60M-B | Lumos LCX235-60M-C | Lumos LS235-60M | Lumos LS235-60M-J | Lumos LS235-60P-J | Lumos LS235PB | Lumos LS235PC | Lumos LSX235-60M-B | Lumos LSX235-60M-C | Lumos LSX235-60M-W | Lumos SST235-60M-BB | Lumos SST235-60P | Lumos LCX240-60M-B | Lumos LCX240-60M-C | Lumos LS240-60M | Lumos LS240-60M-B | Lumos LS240-60M-J | Lumos LS240-60P-B | Lumos LS240-60P-J | Lumos LS240PB | Lumos LS240PC | Lumos LSX240-60M-B | Lumos LSX240-60M-C | Lumos LSX240-60M-W | Lumos SST240-60M-BB | Lumos SST240-60P | Lumos LCX245-60M-B | Lumos LCX245-60M-C | Lumos LS245-60M | Lumos LS245-60M-A1 | Lumos LS245-60M-J | Lumos LS245-60P-J | Lumos LS245-60P-SF | Lumos LS245-60P-SFS | Lumos LS245PB | Lumos LS245PC | Lumos LSX245-60M-B | Lumos LSX245-60M-C | Lumos LSX245-60M-W | Lumos SST245-60M-BB | Lumos LCX250-60M-C | Lumos LS250-60M | Lumos LS250-60M-A1 | Lumos LS250-60M-B | Lumos LS250-60M-J | Lumos LS250-60P-SF | Lumos LS250-60P-SFS | Lumos LS250-72P-J | Lumos LSX250-60M-B | Lumos LSX250-60M-C | Lumos LSX250-60M-W | Lumos LCX255-60M-C | Lumos LS255-60P-SF | Lumos LS255-60P-SFS | Lumos LS255-72P-J | Lumos LSX255-60M-B | Lumos LSX255-60M-C | Lumos GSX260-60M | Lumos LCX260-60M-C | Lumos LS260-60M-SF | Lumos LS260-60M-SFS | Lumos LS260-60P-SF | Lumos LS260-60P-SFS | Lumos LS260-72P-J | Lumos LSX260-60M-C | Lumos LS265-60M-SF | Lumos LS265-60M-SFS | Lumos LS265-60P-SF | Lumos LS265-60P-SFS | Lumos LS265-72M | Lumos LS265-72P-J | Lumos GSX270-60M | Lumos LS270-60M-SF | Lumos LS270-60M-SFS | Lumos LS270-72M | Lumos LS270-72M-J | Lumos LS270-72P-J | Lumos GSX275-60M | Lumos LS275-60M-SF | Lumos LS275-60M-SFS | Lumos LS275-72M | Lumos LS275-72M-J | Lumos LS275-72P | Lumos LS275-72P-J | Lumos GSX280-60M | Lumos LS280-60M-SF | Lumos LS280-60M-SFS | Lumos LS280-72M | Lumos LS280-72M-J | Lumos LS280-72P | Lumos LS280-72P-B | Lumos LS280-72P-J | Lumos LSX280-60M-C | Lumos SST280-72M-BB | Lumos GSX285-60M | Lumos LS285-60M-SF | Lumos LS285-60M-SFS | Lumos LS285-72M | Lumos LS285-72M-J | Lumos LS285-72P | Lumos LS285-72P-J | Lumos LSX285-60M-C | Lumos SST285-72M-BB | Lumos GSX290-60M | Lumos LS290-72M | Lumos LS290-72M-B | Lumos LS290-72M-J | Lumos LS290-72P | Lumos LS290-72P-J | Lumos LS290-72P-SF | Lumos LS290-72P-SFS | Lumos LSX290-60M-C | Lumos SST290-72M-BB | Lumos GSX295-60M | Lumos LS295-72M | Lumos LS295-72M-A1 | Lumos LS295-72M-J | Lumos LS295-72P-J | Lumos LS295-72P-SF | Lumos LS295-72P-SFS | Lumos LSX295-60M-C | Lumos SST295-72M-BB | Lumos GSX300-60M | Lumos LS300-72M | Lumos LS300-72M-A1 | Lumos LS300-72M-B | Lumos LS300-72M-J | Lumos LS300-72P-SF | Lumos LS300-72P-SFS | Lumos LSX300-60M-C | Lumos GSX305-60M | Lumos LS305-72M-B | Lumos LS305-72M-J | Lumos LS305-72P-SF | Lumos LS305-72P-SFS | Lumos LSX305-60M-C | Lumos LS310-72P-SF | Lumos LS310-72P-SFS | Lumos LS315-72M-SF | Lumos LS315-72M-SFS | Lumos LS315-72P-SF | Lumos LS315-72P-SFS | Lumos LS320-72M-SF | Lumos LS320-72M-SFS | Lumos LS320-72P-SF | Lumos LS320-72P-SFS | Lumos LS325-72M-SF | Lumos LS325-72M-SFS | Lumos LS330-72M-SF | Lumos LS330-72M-SFS | Lumos LS335-72M-SF | Lumos LS335-72M-SFS | Lumos GSX340-72M | Lumos GSX345-72M | Lumos GSX350-72M | Lumos GSX355-72M | Lumos GSX360-72M | Lumos GSX365-72M | Luxco LXP-3J240W | Luxco LXP-3J245W | Luxco LXP-3J250W | Luxco LXP-3J255W | Luxco LXP-3J260W | Luxco LXP-2L270T | Luxco LXP-2L275T | Luxco LXP-2L280T | Luxco LXP-2L285T | Luxco LXP-3L285W | Luxco LXP-3L290W | Luxco LXP-3L295W | Luxco LXP-3L300W | Luxor Solar Solo Line 140M | Luxor Solar Solo Line 140P | Luxor Solar Solo Line 145M | Luxor Solar Solo Line 145P | Luxor Solar LX-180M/125-72+ | Luxor Solar LX-185M/125-72+ | Luxor Solar LX-190M/125-72+ | Luxor Solar LX-195M/125-72+ | Luxor Solar LX-220P/156-60+ | Luxor Solar LX-225P/156-60+ | Luxor Solar LX-230M/156-60+ | Luxor Solar LX-230P/156-60+ | Luxor Solar LX-235M/156-60+ | Luxor Solar LX-235P/156-60+ | Luxor Solar LX-240M/156-60+ | Luxor Solar LX-240P/156-60+ | Luxor Solar LX-245M/156-60+ | Luxor Solar LX-250M/156-60+ | Luxor Solar LX-255M/156-60+ | Luxor Solar LX-260M/156-60+ | Luxor Solar LX-260M/156-72+ | Luxor Solar LX-260P/156-72+ | Luxor Solar LX-265M/156-60+ | Luxor Solar LX-265M/156-72+ | Luxor Solar LX-265P/156-72+ | Luxor Solar LX-270M/156-60+ | Luxor Solar LX-270M/156-72+ | Luxor Solar LX-270P/156-72+ | Luxor Solar LX-275M/156-60+ | Luxor Solar LX-275M/156-72+ | Luxor Solar LX-275P/156-72+ | Luxor Solar LX-280M/156-60+ | Luxor Solar LX-280M/156-72+ | Luxor Solar LX-280P/156-72+ | Luxor Solar LX-285M/156-60+ | Luxor Solar LX-290M/156-72+ | Luxor Solar LX-290P/156-72+ | Luxor Solar LX-300M/156-72+ | Luxor Solar LX-300P/156-72+ | Luxor Solar LX-320M/156-72+ | Luxor Solar LX-325M/156-72+ | Luxor Solar LX-330M/156-72+ | Luxor Solar LX-335M/156-72+ | Mage Solar Powertec Plus 180/5 ME | Mage Solar Powertec Plus 185/5 MH | Mage Solar Powertec Plus 185/5MJB | Mage Solar 190/5 MR | Mage Solar Powertec Plus 190/5MH | Mage Solar Powertec Plus 190/5MI | Mage Solar Powertec Plus 195/5MH | Mage Solar Powertec Plus 200/5MH | Mage Solar Powertec Plus 220/6 PH | Mage Solar Powertec Plus 220/6PI | Mage Solar Powertec Plus 225/6PH | Mage Solar Powertec Plus 230/6MI | Mage Solar Powertec Plus 230/6MO | Mage Solar Powertec Plus 230/6PE | Mage Solar Powertec Plus 230/6PF | Mage Solar Powertec Plus 230/6PH | Mage Solar Powertec Plus 230/6PI | Mage Solar Powertec Plus 230/6PJ | Mage Solar Powertec Plus 230/6PO | Mage Solar 235/6 PR | Mage Solar Powertec Plus 235/6MF | Mage Solar Powertec Plus 235/6MI | Mage Solar Powertec Plus 235/6MO | Mage Solar Powertec Plus 235/6PE | Mage Solar Powertec Plus 235/6PH | Mage Solar Powertec Plus 235/6PJ | Mage Solar Powertec Plus 235/6PO | Mage Solar POWERTEC Plus 240 / 6 PL US | Mage Solar POWERTEC Plus 240 / 6 PL US AC | Mage Solar Powertec Plus 240/6MF | Mage Solar Powertec Plus 240/6MI | Mage Solar Powertec Plus 240/6MO | Mage Solar Powertec Plus 240/6PE | Mage Solar Powertec Plus 240/6PH | Mage Solar Powertec Plus 240/6PJ | Mage Solar Powertec Plus 240/6PO | Mage Solar 245/5 MR | Mage Solar POWERTEC Plus 245 / 6 PL US AC | Mage Solar POWERTEC Plus 245 / 6PL US | Mage Solar Powertec Plus 245/6 PL | Mage Solar 250/5 MR | Mage Solar POWERTEC Plus 250 / 6 MN US | Mage Solar Powertec Plus 250/6 MH | Mage Solar Powertec Plus 250/6 ML | Mage Solar Powertec Plus 250/6 PL | Mage Solar Powertec Plus 255/6 PL | Mage Solar Powertec Plus 275/6 PL | Mage Solar Powertec Plus 280/6 PL | Mage Solar Powertec Plus 285/6 PL | Mage Solar Powertec Plus 290/6 PL | Mage Solar Powertec Plus 290/6-72 PH | Mage Solar Powertec Plus 295/6 PL | Mage Solar Powertec Plus 300/6-72 MH | Mage Solar USA Powertec Plus 190/5 MH-US | Mage Solar USA Powertec Plus 195/5MH-US | Mage Solar USA Powertec Plus 230/6 PH-US | Mage Solar USA Powertec Plus 230/6 PL | Mage Solar USA Powertec Plus 235/6 ML | Mage Solar USA Powertec Plus 235/6 PL | Mage Solar USA Powertec Plus 235/6PH-US | Mage Solar USA Powertec Plus 240/6 ML | Mage Solar USA Powertec Plus 240/6 PL | Mage Solar USA Powertec Plus 240/6 PNS | Mage Solar USA Powertec Plus 245/6 ML | Mage Solar USA Powertec Plus 245/6 MNBS | Mage Solar USA Powertec Plus 250/6 MNBS | Mage Solar USA Powertec Plus 250/6 MNCS | Mage Solar USA Powertec Plus 250/6 MNS | Mage Solar USA Powertec Plus 250/6 PL US | Mage Solar USA Powertec Plus 250/6 PL US AC | Mage Solar USA Powertec Plus 255/6 ML | Mage Solar USA Powertec Plus 290 / 6-72 PH | Mage Solar USA Powertec Plus 300/6 PL | Malaysian Solar Resources MYS-60P/B3/CF-235 | Malaysian Solar Resources MYS-60P/B3/CF-240 | Malaysian Solar Resources MYS-60P/B3/CF-245 | Martifer Solar MTS225P | MCV Technologies MCV-180 | MCV Technologies MCV-185 | MCV Technologies MCV-190 | MCV Technologies MCV-220 | MCV Technologies MCV-225 | MCV Technologies MCV-230 | MCV Technologies MCV-235 | MCV Technologies MCV-240 | MCV Technologies MCV-265 | MCV Technologies MCV-270 | MCV Technologies MCV-275 | MCV Technologies MCV-280 | MCV Technologies MCV-285 | MEMC Singapore MEMC-M230ACA-20 | MEMC Singapore MEMC-M230AMA-20 | MEMC Singapore MEMC-M230LCA-20 | MEMC Singapore MEMC-M230LMA-20 | MEMC Singapore MEMC-M235ACA-20 | MEMC Singapore MEMC-M235AMA-20 | MEMC Singapore MEMC-M240ACA-20 | MEMC Singapore MEMC-M240ACC-20 | MEMC Singapore MEMC-M240ACC-21 | MEMC Singapore MEMC-M240AIC-20 | MEMC Singapore MEMC-M240AIC-21 | MEMC Singapore MEMC-M240AMA-20 | MEMC Singapore MEMC-M240AMC-20 | MEMC Singapore MEMC-M240AMC-21 | MEMC Singapore MEMC-M240LCA-20 | MEMC Singapore MEMC-M240LCC-20 | MEMC Singapore MEMC-M240LCC-21 | MEMC Singapore MEMC-M240LIC-20 | MEMC Singapore MEMC-M240LIC-21 | MEMC Singapore MEMC-M240LMA-20 | MEMC Singapore MEMC-M240LMC-20 | MEMC Singapore MEMC-M240LMC-21 | MEMC Singapore MEMC-M245ACA-20 | MEMC Singapore MEMC-M245ACC-20 | MEMC Singapore MEMC-M245ACC-21 | MEMC Singapore MEMC-M245AIC-20 | MEMC Singapore MEMC-M245AIC-21 | MEMC Singapore MEMC-M245AMA-20 | MEMC Singapore MEMC-M245AMC-20 | MEMC Singapore MEMC-M245AMC-21 | MEMC Singapore MEMC-M245LCC-20 | MEMC Singapore MEMC-M245LCC-21 | MEMC Singapore MEMC-M245LIC-20 | MEMC Singapore MEMC-M245LIC-21 | MEMC Singapore MEMC-M245LMC-20 | MEMC Singapore MEMC-M245LMC-21 | MEMC Singapore SE-M245KZC-2Y | MEMC Singapore MEMC-M250ACA-20 | MEMC Singapore MEMC-M250ACC-20 | MEMC Singapore MEMC-M250ACC-21 | MEMC Singapore MEMC-M250AIC-20 | MEMC Singapore MEMC-M250AIC-21 | MEMC Singapore MEMC-M250AMA-20 | MEMC Singapore MEMC-M250AMC-20 | MEMC Singapore MEMC-M250AMC-21 | MEMC Singapore MEMC-M250LCA-20 | MEMC Singapore MEMC-M250LCC-20 | MEMC Singapore MEMC-M250LCC-21 | MEMC Singapore MEMC-M250LIC-20 | MEMC Singapore MEMC-M250LIC-21 | MEMC Singapore MEMC-M250LMA-20 | MEMC Singapore MEMC-M250LMC-20 | MEMC Singapore MEMC-M250LMC-21 | MEMC Singapore SE-M250KZC-2Y | MEMC Singapore MEMC-M255ACA-20 | MEMC Singapore MEMC-M255ACC-20 | MEMC Singapore MEMC-M255ACC-21 | MEMC Singapore MEMC-M255AIC-20 | MEMC Singapore MEMC-M255AIC-21 | MEMC Singapore MEMC-M255AMA-20 | MEMC Singapore MEMC-M255AMC-20 | MEMC Singapore MEMC-M255AMC-21 | MEMC Singapore MEMC-M255LCA-20 | MEMC Singapore MEMC-M255LCC-20 | MEMC Singapore MEMC-M255LCC-21 | MEMC Singapore MEMC-M255LIC-20 | MEMC Singapore MEMC-M255LIC-21 | MEMC Singapore MEMC-M255LMA-20 | MEMC Singapore MEMC-M255LMC-20 | MEMC Singapore MEMC-M255LMC-21 | MEMC Singapore SE-M255KZC-2Y | MEMC Singapore MEMC-M260ACA-20 | MEMC Singapore MEMC-M260ACC-20 | MEMC Singapore MEMC-M260ACC-21 | MEMC Singapore MEMC-M260AIC-20 | MEMC Singapore MEMC-M260AIC-21 | MEMC Singapore MEMC-M260AMA-20 | MEMC Singapore MEMC-M260AMC-20 | MEMC Singapore MEMC-M260AMC-21 | MEMC Singapore MEMC-M260LCA-20 | MEMC Singapore MEMC-M260LCC-20 | MEMC Singapore MEMC-M260LCC-21 | MEMC Singapore MEMC-M260LIC-20 | MEMC Singapore MEMC-M260LIC-21 | MEMC Singapore MEMC-M260LMA-20 | MEMC Singapore MEMC-M260LMC-20 | MEMC Singapore MEMC-M260LMC-21 | MEMC Singapore SE-M260KZC-2Y | MEMC Singapore MEMC-P270ACA | MEMC Singapore MEMC-P270ACC-21 | MEMC Singapore MEMC-P270ACC-25 | MEMC Singapore MEMC-P270ACC-26 | MEMC Singapore MEMC-P270AIC-20 | MEMC Singapore MEMC-P270AIC-24 | MEMC Singapore MEMC-P270AMA | MEMC Singapore MEMC-P270AMA-20 | MEMC Singapore MEMC-P270AMC-20 | MEMC Singapore MEMC-P270AMC-24 | MEMC Singapore MEMC-P270BCA-20 | MEMC Singapore MEMC-P270BCA-21 | MEMC Singapore MEMC-P270BCC-21 | MEMC Singapore MEMC-P270BCC-25 | MEMC Singapore MEMC-P270BCC-26 | MEMC Singapore MEMC-P270BCC-27 | MEMC Singapore MEMC-P270BMA-20 | MEMC Singapore MEMC-P270BMC-20 | MEMC Singapore MEMC-P270BMC-24 | MEMC Singapore MEMC-P270BMC-25 | MEMC Singapore MEMC-P270BMC-26 | MEMC Singapore MEMC-P270BMC-27 | MEMC Singapore MEMC-M275ACA-20 | MEMC Singapore MEMC-M275ACA-21 | MEMC Singapore MEMC-M275AMA-20 | MEMC Singapore MEMC-M275BCA-20 | MEMC Singapore MEMC-M275BCA-21 | MEMC Singapore MEMC-M275BMA-20 | MEMC Singapore MEMC-P275ACA | MEMC Singapore MEMC-P275ACA-20 | MEMC Singapore MEMC-P275ACA-21 | MEMC Singapore MEMC-P275ACC-21 | MEMC Singapore MEMC-P275ACC-25 | MEMC Singapore MEMC-P275ACC-26 | MEMC Singapore MEMC-P275AIC-20 | MEMC Singapore MEMC-P275AIC-24 | MEMC Singapore MEMC-P275AMA | MEMC Singapore MEMC-P275AMA-20 | MEMC Singapore MEMC-P275AMC-20 | MEMC Singapore MEMC-P275AMC-24 | MEMC Singapore MEMC-P275BCA-20 | MEMC Singapore MEMC-P275BCA-21 | MEMC Singapore MEMC-P275BCC-21 | MEMC Singapore MEMC-P275BCC-25 | MEMC Singapore MEMC-P275BCC-26 | MEMC Singapore MEMC-P275BCC-27 | MEMC Singapore MEMC-P275BMA-20 | MEMC Singapore MEMC-P275BMC-20 | MEMC Singapore MEMC-P275BMC-24 | MEMC Singapore MEMC-P275BMC-25 | MEMC Singapore MEMC-P275BMC-26 | MEMC Singapore MEMC-P275BMC-27 | MEMC Singapore MEMC-M280ACA-20 | MEMC Singapore MEMC-M280ACA-21 | MEMC Singapore MEMC-M280AMA-20 | MEMC Singapore MEMC-M280BCA-20 | MEMC Singapore MEMC-M280BCA-21 | MEMC Singapore MEMC-M280BMA-20 | MEMC Singapore MEMC-P280ACA | MEMC Singapore MEMC-P280ACA-20 | MEMC Singapore MEMC-P280ACA-21 | MEMC Singapore MEMC-P280ACC-21 | MEMC Singapore MEMC-P280ACC-25 | MEMC Singapore MEMC-P280ACC-26 | MEMC Singapore MEMC-P280AIC-20 | MEMC Singapore MEMC-P280AIC-24 | MEMC Singapore MEMC-P280AMA | MEMC Singapore MEMC-P280AMA-20 | MEMC Singapore MEMC-P280AMC-20 | MEMC Singapore MEMC-P280AMC-24 | MEMC Singapore MEMC-P280BCA-20 | MEMC Singapore MEMC-P280BCA-21 | MEMC Singapore MEMC-P280BCC-21 | MEMC Singapore MEMC-P280BCC-25 | MEMC Singapore MEMC-P280BCC-26 | MEMC Singapore MEMC-P280BCC-27 | MEMC Singapore MEMC-P280BMA-20 | MEMC Singapore MEMC-P280BMC-20 | MEMC Singapore MEMC-P280BMC-24 | MEMC Singapore MEMC-P280BMC-25 | MEMC Singapore MEMC-P280BMC-26 | MEMC Singapore MEMC-P280BMC-27 | MEMC Singapore MEMC-P280BZC-3Y | MEMC Singapore MEMC-M285ACA-20 | MEMC Singapore MEMC-M285ACA-21 | MEMC Singapore MEMC-M285AMA-20 | MEMC Singapore MEMC-M285BCA-20 | MEMC Singapore MEMC-M285BCA-21 | MEMC Singapore MEMC-M285BMA-20 | MEMC Singapore MEMC-P285ACA | MEMC Singapore MEMC-P285ACA-20 | MEMC Singapore MEMC-P285ACA-21 | MEMC Singapore MEMC-P285ACC-21 | MEMC Singapore MEMC-P285ACC-25 | MEMC Singapore MEMC-P285ACC-26 | MEMC Singapore MEMC-P285AIC-20 | MEMC Singapore MEMC-P285AIC-24 | MEMC Singapore MEMC-P285AMA | MEMC Singapore MEMC-P285AMA-20 | MEMC Singapore MEMC-P285AMC-20 | MEMC Singapore MEMC-P285AMC-24 | MEMC Singapore MEMC-P285BCA-20 | MEMC Singapore MEMC-P285BCA-21 | MEMC Singapore MEMC-P285BCC-21 | MEMC Singapore MEMC-P285BCC-25 | MEMC Singapore MEMC-P285BCC-26 | MEMC Singapore MEMC-P285BCC-27 | MEMC Singapore MEMC-P285BMA-20 | MEMC Singapore MEMC-P285BMC-20 | MEMC Singapore MEMC-P285BMC-24 | MEMC Singapore MEMC-P285BMC-25 | MEMC Singapore MEMC-P285BMC-26 | MEMC Singapore MEMC-P285BMC-27 | MEMC Singapore MEMC-P285BZC-3Y | MEMC Singapore MEMC-M290ACA-20 | MEMC Singapore MEMC-M290ACA-21 | MEMC Singapore MEMC-M290ACC-24 | MEMC Singapore MEMC-M290ACC-27 | MEMC Singapore MEMC-M290AEC-24 | MEMC Singapore MEMC-M290AEC-27 | MEMC Singapore MEMC-M290AMA-20 | MEMC Singapore MEMC-M290AMC-24 | MEMC Singapore MEMC-M290AMC-27 | MEMC Singapore MEMC-M290BCA-20 | MEMC Singapore MEMC-M290BCA-21 | MEMC Singapore MEMC-M290BCC-24 | MEMC Singapore MEMC-M290BCC-27 | MEMC Singapore MEMC-M290BEC-24 | MEMC Singapore MEMC-M290BEC-27 | MEMC Singapore MEMC-M290BMA-20 | MEMC Singapore MEMC-M290BMC-24 | MEMC Singapore MEMC-M290BMC-27 | MEMC Singapore MEMC-P290ACA | MEMC Singapore MEMC-P290ACA-20 | MEMC Singapore MEMC-P290ACA-21 | MEMC Singapore MEMC-P290ACC-21 | MEMC Singapore MEMC-P290ACC-25 | MEMC Singapore MEMC-P290ACC-26 | MEMC Singapore MEMC-P290AIC-20 | MEMC Singapore MEMC-P290AIC-24 | MEMC Singapore MEMC-P290AMA | MEMC Singapore MEMC-P290AMA-20 | MEMC Singapore MEMC-P290AMC-20 | MEMC Singapore MEMC-P290AMC-24 | MEMC Singapore MEMC-P290BCA-20 | MEMC Singapore MEMC-P290BCA-21 | MEMC Singapore MEMC-P290BCC-21 | MEMC Singapore MEMC-P290BCC-25 | MEMC Singapore MEMC-P290BCC-26 | MEMC Singapore MEMC-P290BCC-27 | MEMC Singapore MEMC-P290BMA-20 | MEMC Singapore MEMC-P290BMC-20 | MEMC Singapore MEMC-P290BMC-24 | MEMC Singapore MEMC-P290BMC-25 | MEMC Singapore MEMC-P290BMC-26 | MEMC Singapore MEMC-P290BMC-27 | MEMC Singapore MEMC-P290BZC-3Y | MEMC Singapore MEMC-Q290ACC-34 | MEMC Singapore MEMC-Q290ACC-35 | MEMC Singapore MEMC-Q290ACC-36 | MEMC Singapore MEMC-Q290AEC-34 | MEMC Singapore MEMC-Q290AEC-35 | MEMC Singapore MEMC-Q290AEC-36 | MEMC Singapore MEMC-Q290AMC-34 | MEMC Singapore MEMC-Q290AMC-35 | MEMC Singapore MEMC-Q290AMC-36 | MEMC Singapore MEMC-Q290BZC-3Y | MEMC Singapore SE-M290BZC-3Y | MEMC Singapore MEMC-M295ACA-20 | MEMC Singapore MEMC-M295ACA-21 | MEMC Singapore MEMC-M295ACC-24 | MEMC Singapore MEMC-M295ACC-27 | MEMC Singapore MEMC-M295AEC-24 | MEMC Singapore MEMC-M295AEC-27 | MEMC Singapore MEMC-M295AMA-20 | MEMC Singapore MEMC-M295AMC-24 | MEMC Singapore MEMC-M295AMC-27 | MEMC Singapore MEMC-M295BCA-20 | MEMC Singapore MEMC-M295BCA-21 | MEMC Singapore MEMC-M295BCC-24 | MEMC Singapore MEMC-M295BCC-27 | MEMC Singapore MEMC-M295BEC-24 | MEMC Singapore MEMC-M295BEC-27 | MEMC Singapore MEMC-M295BMA-20 | MEMC Singapore MEMC-M295BMC-24 | MEMC Singapore MEMC-M295BMC-27 | MEMC Singapore MEMC-P295ACC-21 | MEMC Singapore MEMC-P295ACC-25 | MEMC Singapore MEMC-P295ACC-26 | MEMC Singapore MEMC-P295AIC-20 | MEMC Singapore MEMC-P295AIC-24 | MEMC Singapore MEMC-P295AMC-20 | MEMC Singapore MEMC-P295AMC-24 | MEMC Singapore MEMC-P295BCC-21 | MEMC Singapore MEMC-P295BCC-25 | MEMC Singapore MEMC-P295BCC-26 | MEMC Singapore MEMC-P295BCC-27 | MEMC Singapore MEMC-P295BMC-20 | MEMC Singapore MEMC-P295BMC-24 | MEMC Singapore MEMC-P295BMC-25 | MEMC Singapore MEMC-P295BMC-26 | MEMC Singapore MEMC-P295BMC-27 | MEMC Singapore MEMC-P295BZC-3Y | MEMC Singapore MEMC-Q295ACC-34 | MEMC Singapore MEMC-Q295ACC-35 | MEMC Singapore MEMC-Q295ACC-36 | MEMC Singapore MEMC-Q295AEC-34 | MEMC Singapore MEMC-Q295AEC-35 | MEMC Singapore MEMC-Q295AEC-36 | MEMC Singapore MEMC-Q295AMC-34 | MEMC Singapore MEMC-Q295AMC-35 | MEMC Singapore MEMC-Q295AMC-36 | MEMC Singapore MEMC-Q295BZC-3Y | MEMC Singapore SE-M295BZC-3Y | MEMC Singapore MEMC-M300ACC-24 | MEMC Singapore MEMC-M300ACC-27 | MEMC Singapore MEMC-M300AEC-24 | MEMC Singapore MEMC-M300AEC-27 | MEMC Singapore MEMC-M300AMC-24 | MEMC Singapore MEMC-M300AMC-27 | MEMC Singapore MEMC-M300BCC-24 | MEMC Singapore MEMC-M300BCC-27 | MEMC Singapore MEMC-M300BEC-24 | MEMC Singapore MEMC-M300BEC-27 | MEMC Singapore MEMC-M300BMC-24 | MEMC Singapore MEMC-M300BMC-27 | MEMC Singapore MEMC-M300BZC-3Y | MEMC Singapore MEMC-P300BCC-21 | MEMC Singapore MEMC-P300BCC-25 | MEMC Singapore MEMC-P300BCC-26 | MEMC Singapore MEMC-P300BCC-27 | MEMC Singapore MEMC-P300BMC-20 | MEMC Singapore MEMC-P300BMC-24 | MEMC Singapore MEMC-P300BMC-25 | MEMC Singapore MEMC-P300BMC-26 | MEMC Singapore MEMC-P300BMC-27 | MEMC Singapore MEMC-P300BZC-3Y | MEMC Singapore MEMC-Q300ACC-34 | MEMC Singapore MEMC-Q300ACC-35 | MEMC Singapore MEMC-Q300ACC-36 | MEMC Singapore MEMC-Q300AEC-34 | MEMC Singapore MEMC-Q300AEC-35 | MEMC Singapore MEMC-Q300AEC-36 | MEMC Singapore MEMC-Q300AMC-34 | MEMC Singapore MEMC-Q300AMC-35 | MEMC Singapore MEMC-Q300AMC-36 | MEMC Singapore MEMC-Q300BZC-3Y | MEMC Singapore SE-M300BZC-3Y | MEMC Singapore MEMC-M305ACC-24 | MEMC Singapore MEMC-M305ACC-27 | MEMC Singapore MEMC-M305AEC-24 | MEMC Singapore MEMC-M305AEC-27 | MEMC Singapore MEMC-M305AMC-24 | MEMC Singapore MEMC-M305AMC-27 | MEMC Singapore MEMC-M305BCC-24 | MEMC Singapore MEMC-M305BCC-27 | MEMC Singapore MEMC-M305BEC-24 | MEMC Singapore MEMC-M305BEC-27 | MEMC Singapore MEMC-M305BMC-24 | MEMC Singapore MEMC-M305BMC-27 | MEMC Singapore MEMC-M305BZC-3Y | MEMC Singapore MEMC-P305BCC-21 | MEMC Singapore MEMC-P305BCC-25 | MEMC Singapore MEMC-P305BCC-26 | MEMC Singapore MEMC-P305BCC-27 | MEMC Singapore MEMC-P305BMC-20 | MEMC Singapore MEMC-P305BMC-24 | MEMC Singapore MEMC-P305BMC-25 | MEMC Singapore MEMC-P305BMC-26 | MEMC Singapore MEMC-P305BMC-27 | MEMC Singapore MEMC-P305BZC-3Y | MEMC Singapore MEMC-Q305ACC-34 | MEMC Singapore MEMC-Q305ACC-35 | MEMC Singapore MEMC-Q305ACC-36 | MEMC Singapore MEMC-Q305AEC-34 | MEMC Singapore MEMC-Q305AEC-35 | MEMC Singapore MEMC-Q305AEC-36 | MEMC Singapore MEMC-Q305AMC-34 | MEMC Singapore MEMC-Q305AMC-35 | MEMC Singapore MEMC-Q305AMC-36 | MEMC Singapore MEMC-Q305BZC-3Y | MEMC Singapore SE-M305BZC-3Y | MEMC Singapore MEMC-M310BZC-3Y | MEMC Singapore MEMC-Q310ACC-34 | MEMC Singapore MEMC-Q310ACC-35 | MEMC Singapore MEMC-Q310ACC-36 | MEMC Singapore MEMC-Q310AEC-34 | MEMC Singapore MEMC-Q310AEC-35 | MEMC Singapore MEMC-Q310AEC-36 | MEMC Singapore MEMC-Q310AMC-34 | MEMC Singapore MEMC-Q310AMC-35 | MEMC Singapore MEMC-Q310AMC-36 | MEMC Singapore MEMC-Q310BZC-3Y | MEMC Singapore SE-F310BZC-3Y | MEMC Singapore SE-M310BZC-3Y | MEMC Singapore MEMC-M315BZC-3Y | MEMC Singapore MEMC-Q315ACC-34 | MEMC Singapore MEMC-Q315ACC-35 | MEMC Singapore MEMC-Q315ACC-36 | MEMC Singapore MEMC-Q315AEC-34 | MEMC Singapore MEMC-Q315AEC-35 | MEMC Singapore MEMC-Q315AEC-36 | MEMC Singapore MEMC-Q315AMC-34 | MEMC Singapore MEMC-Q315AMC-35 | MEMC Singapore MEMC-Q315AMC-36 | MEMC Singapore MEMC-Q315BZC-3Y | MEMC Singapore SE-F315BZC-3Y | MEMC Singapore SE-M315BZC-3Y | MEMC Singapore MEMC-M320BZC-3Y | MEMC Singapore MEMC-Q320ACC-34 | MEMC Singapore MEMC-Q320ACC-35 | MEMC Singapore MEMC-Q320ACC-36 | MEMC Singapore MEMC-Q320AEC-34 | MEMC Singapore MEMC-Q320AEC-35 | MEMC Singapore MEMC-Q320AEC-36 | MEMC Singapore MEMC-Q320AMC-34 | MEMC Singapore MEMC-Q320AMC-35 | MEMC Singapore MEMC-Q320AMC-36 | MEMC Singapore MEMC-Q320BZC-3Y | MEMC Singapore SE-F320BZC-3Y | MEMC Singapore SE-M320BZC-3Y | MEMC Singapore MEMC-M325BZC-3Y | MEMC Singapore SE-F325BZC-3Y | MEMC Singapore MEMC-M330BZC-3Y | MEMC Singapore SE-F330BZC-3Y | MEMC Singapore SE-F335BZC-3Y | Merlin Solar Technologies_ Inc FX155L | Merlin Solar Technologies_ Inc FX155S | Merlin Solar Technologies_ Inc FX160L | Merlin Solar Technologies_ Inc FX160S | Merlin Solar Technologies_ Inc GX160 | Merlin Solar Technologies_ Inc FX165L | Merlin Solar Technologies_ Inc FX165S | Merlin Solar Technologies_ Inc GX165 | Merlin Solar Technologies_ Inc GX170 | Merlin Solar Technologies_ Inc BR320 | Merlin Solar Technologies_ Inc BR325 | Merlin Solar Technologies_ Inc BR330 | Merlin Solar Technologies_ Inc BR335 | Merlin Solar Technologies_ Inc BR340 | Miasole Flex-01 70N | Miasole Flex-02 70N | Miasole MR-107 | Miasole Flex-03 120N | Miasole Flex-02 120N | Miasole MS120GG | Miasole MS125GG | Miasole MS130GG | Miasole MS135GG | Miasole MS135GG-02 | Miasole MS140GG | Miasole MS140GG-02 | Miasole MS145GG-02 | Miasole MS150GG-02 | Miasole MS160GG-04 | Miasole Flex-01 210W | Miasole Flex-02 220W | Miasole Flex-02-275N C132 | Miasole Flex-03-280NL | Miasole Flex-03 290W | Miasole Flex-03 300W | Miasole Flex-03 310W | Miasole Flex-03 320W | Miasole Flex-02 350W | Miasole Flex-03-490W | Mission Solar Energy MSE260SO5T | Mission Solar Energy MSE265SO5T | Mission Solar Energy MSE270SO5K | Mission Solar Energy MSE270SO5T | Mission Solar Energy MSE275SO5K | Mission Solar Energy MSE275SO5T | Mission Solar Energy MSE280SO5K | Mission Solar Energy MSE280SO5T | Mission Solar Energy MSE285SO5K | Mission Solar Energy MSE285SQ5K | Mission Solar Energy MSE285SQ5T | Mission Solar Energy MSE290SB1A | Mission Solar Energy MSE290SQ5K | Mission Solar Energy MSE290SQ5T | Mission Solar Energy MSE295SB1A | Mission Solar Energy MSE295SQ5K | Mission Solar Energy MSE295SQ5T | Mission Solar Energy MSE300MC1A | Mission Solar Energy MSE300SB1A | Mission Solar Energy MSE300SQ5K | Mission Solar Energy MSE300SQ5T | Mission Solar Energy MSE305MC1A | Mission Solar Energy MSE305SB1A | Mission Solar Energy MSE305SE1A | Mission Solar Energy MSE305SE1J | Mission Solar Energy MSE305SQ5K | Mission Solar Energy MSE310MC1A | Mission Solar Energy MSE310SB1A | Mission Solar Energy MSE310SE1A | Mission Solar Energy MSE310SE1J | Mission Solar Energy MSE315MC1A | Mission Solar Energy MSE315SB1A | Mission Solar Energy MSE315SE1A | Mission Solar Energy MSE315SE1J | Mission Solar Energy MSE320MC1A | Mission Solar Energy MSE320MM4J | Mission Solar Energy MSE320MM6J | Mission Solar Energy MSE320SB1A | Mission Solar Energy MSE320SE1A | Mission Solar Energy MSE320SE1J | Mission Solar Energy MSE320SO4J | Mission Solar Energy MSE320SO6J | Mission Solar Energy MSE320SO6W | Mission Solar Energy MSE325MC1A | Mission Solar Energy MSE325MM4J | Mission Solar Energy MSE325MM6J | Mission Solar Energy MSE325SB1A | Mission Solar Energy MSE325SE1A | Mission Solar Energy MSE325SE1J | Mission Solar Energy MSE325SO4J | Mission Solar Energy MSE325SO6J | Mission Solar Energy MSE325SO6W | Mission Solar Energy MSE330MM4J | Mission Solar Energy MSE330MM6J | Mission Solar Energy MSE330SB1A | Mission Solar Energy MSE330SE1A | Mission Solar Energy MSE330SE1J | Mission Solar Energy MSE330SO4J | Mission Solar Energy MSE330SO6J | Mission Solar Energy MSE330SO6W | Mission Solar Energy MSE335SB1A | Mission Solar Energy MSE335SE1A | Mission Solar Energy MSE335SE1J | Mission Solar Energy MSE335SO4J | Mission Solar Energy MSE335SO6J | Mission Solar Energy MSE335SQ6W | Mission Solar Energy VMS335SQ1S | Mission Solar Energy MSE340SO4J | Mission Solar Energy MSE340SO6J | Mission Solar Energy MSE340SQ6S | Mission Solar Energy MSE340SQ6W | Mission Solar Energy VMS340SQ1S | Mission Solar Energy MSE345SO4J | Mission Solar Energy MSE345SO6J | Mission Solar Energy MSE345SQ4S | Mission Solar Energy MSE345SQ6S | Mission Solar Energy MSE345SQ6W | Mission Solar Energy VMS345SQ1S | Mission Solar Energy MSE350SQ4S | Mission Solar Energy MSE350SQ6S | Mission Solar Energy VMS350SQ1S | Mission Solar Energy MSE355SQ4S | Mission Solar Energy MSE355SQ6S | Mission Solar Energy VMS355SQ1S | Mission Solar Energy MSE360SQ4S | Mission Solar Energy MSE360SQ6S | Mission Solar Energy MSE365SQ4S | Mission Solar Energy MSE365SQ6S | Mitsubishi Electric PV-EE120MF5F | Mitsubishi Electric PV-EE125MF5F | Mitsubishi Electric PV-EE130MF5F | Mitsubishi Electric PV-MF160EB4 | Mitsubishi Electric PV-MF165EB4 | Mitsubishi Electric PV-MF170EB3 | Mitsubishi Electric PV-MF170EB4 | Mitsubishi Electric PV-MF170UD4 | Mitsubishi Electric PV-UD170MF5 | Mitsubishi Electric PV-MF175UD4 | Mitsubishi Electric PV-UD175MF5 | Mitsubishi Electric PV-MF180UD4 | Mitsubishi Electric PV-UD180MF5 | Mitsubishi Electric PV-UD185HA6 | Mitsubishi Electric PV-UD185MF5 | Mitsubishi Electric PV-UD190HA6 | Mitsubishi Electric PV-UD190MF5 | Mitsubishi Electric PV-UD195HA6 | Mitsubishi Electric PV-UJ212G6 | Mitsubishi Electric PV-UJ218G6 | Mitsubishi Electric PV-UJ220GA6 | Mitsubishi Electric PV-UJ220GA6-D | Mitsubishi Electric PV-UJ224G6 | Mitsubishi Electric PV-UJ225GA6 | Mitsubishi Electric PV-UJ225GA6-D | Mitsubishi Electric PV-UJ230GA6 | Mitsubishi Electric PV-UJ230GA6-D | Mitsubishi Electric PV-MJU235GB | Mitsubishi Electric PV-UJ235GA6 | Mitsubishi Electric PV-UJ235GA6-D | Mitsubishi Electric PV-MJU240GB | Mitsubishi Electric PV-MJU245GB | Mitsubishi Electric PV-MLU250HC | Mitsubishi Electric PV-MLE255HD | Mitsubishi Electric PV-MLU255HC | Mitsubishi Electric PV-MLE260HD | Mitsubishi Electric PV-MLU260HC | Mitsubishi Electric PV-MJE265FB | Mitsubishi Electric PV-MLE265HD | Mitsubishi Electric PV-MLE265HD2 | Mitsubishi Electric PV-MJE270FB | Mitsubishi Electric PV-MLE270HD | Mitsubishi Electric PV-MLE270HD2 | Mitsubishi Electric PV-MJE275FB | Mitsubishi Electric PV-MJE275FB-B | Mitsubishi Electric PV-MLE275HD2 | Mitsubishi Electric PV-MJE280FB | Mitsubishi Electric PV-MJE280FB-B | Mitsubishi Electric PV-MLE280HD2 | Moser Baer Photovoltaic MBPV CAAP 210 | Moser Baer Photovoltaic MBPV CAAP BB 210W | Moser Baer Photovoltaic MBPV CAAP 215W | Moser Baer Photovoltaic MBPV CAAP BB 215W | Moser Baer Photovoltaic MBPV CAAP 220 | Moser Baer Photovoltaic MBPV CAAP BB 220W | Moser Baer Photovoltaic MBPV CAAP BB 225W | Moser Baer Photovoltaic MBPV CAAP BB 230W | Moser Baer Photovoltaic MBPV CAAP BB 235W | Moser Baer Photovoltaic MBPV CAAP BB 240W | Moser Baer Photovoltaic MBPV CAAP BB 245W | Moser Baer Solar MBSL eLITE 60 3x 225 | Moser Baer Solar MBSL eLITE 60 3x 230 | Moser Baer Solar MBSL eLITE 60 3x 235 | Moser Baer Solar MBSL eLITE 60 3x 240 | Moser Baer Solar MBSL eLITE 60 3x 245 | Motech Industries IM54B2-200-wxxyzz | Motech Industries IM54C2-200-wxxyzz | Motech Industries IM54C3-200-wxxyzz | Motech Industries IM54D2-200-wxxyzz | Motech Industries IM54D3-200-wxxyzz | Motech Industries GEPVp-205-MSA | Motech Industries GEPVp-205-MSB | Motech Industries IM54B2-205-wxxyzz | Motech Industries IM54B3-205-wxxyzz | Motech Industries IM54C2-205-wxxyzz | Motech Industries IM54C3-205-wxxyzz | Motech Industries IM54D2-205-wxxyzz | Motech Industries IM54D3-205-wxxyzz | Motech Industries GEPVp-210-MSA | Motech Industries GEPVp-210-MSB | Motech Industries IM54B2-210-wxxyzz | Motech Industries IM54B3-210-wxxyzz | Motech Industries IM54C2-210-wxxyzz | Motech Industries IM54C3-210-wxxyzz | Motech Industries IM54D2-210-wxxyzz | Motech Industries IM54D3-210-wxxyzz | Motech Industries XS54B3-210-wxxyzz | Motech Industries XS54C3-210-wxxyzz | Motech Industries XS54D3-210-wxxyzz | Motech Industries IM54B2-215-wxxyzz | Motech Industries IM54B3-215-wxxyzz | Motech Industries IM54C2-215-wxxyzz | Motech Industries IM54C3-215-wxxyzz | Motech Industries IM54D2-215-wxxyzz | Motech Industries IM54D3-215-wxxyzz | Motech Industries XS54B3-215-wxxyzz | Motech Industries XS54C3-215-wxxyzz | Motech Industries XS54D3-215-wxxyzz | Motech Industries IM54B3-220-wxxyzz | Motech Industries IM54C2-220-wxxyzz | Motech Industries IM54C3-220-wxxyzz | Motech Industries IM54D2-220-wxxyzz | Motech Industries IM54D3-220-wxxyzz | Motech Industries XS54B3-220-wxxyzz | Motech Industries XS54C3-220-wxxyzz | Motech Industries XS54D3-220-wxxyzz | Motech Industries IM54B3-225-wxxyzz | Motech Industries IM54C3-225-wxxyzz | Motech Industries IM54D3-225-wxxyzz | Motech Industries IM60B2-225-wxxyzz | Motech Industries IM60B3-225-wxxyzz | Motech Industries XS54B3-225-wxxyzz | Motech Industries XS54C3-225-wxxyzz | Motech Industries XS54D3-225-wxxyzz | Motech Industries IM60B2-230-wxxyzz | Motech Industries IM60B3-230-wxxyzz | Motech Industries IM60C3-230-wxxyzz | Motech Industries IM60D3-230-wxxyzz | Motech Industries MTPVp-230-MSB | Motech Industries MTPVp-230-MSC | Motech Industries MTPVp-230-MSD | Motech Industries XS54B3-230-wxxyzz | Motech Industries XS54C3-230-wxxyzz | Motech Industries XS54D3-230-wxxyzz | Motech Industries IM60B2-235-wxxyzz | Motech Industries IM60B3-235-wxxyzz | Motech Industries IM60C2-235-wxxyzz | Motech Industries IM60C3-235-wxxyzz | Motech Industries IM60D2-235-wxxyzz | Motech Industries IM60D3-235-wxxyzz | Motech Industries MTPVp-235-MSB | Motech Industries MTPVp-235-MSC | Motech Industries MTPVp-235-MSD | Motech Industries XS54C3-235-wxxyzz | Motech Industries XS60B3-235-wxxyzz | Motech Industries XS60C3-235-wxxyzz | Motech Industries XS60D3-235-wxxyzz | Motech Industries IM60B2-240-wxxyzz | Motech Industries IM60B3-240-wxxyzz | Motech Industries IM60C2-240-wxxyzz | Motech Industries IM60C3-240-wxxyzz | Motech Industries IM60D2-240-wxxyzz | Motech Industries IM60D3-240-wxxyzz | Motech Industries MTPVp-240-MSB | Motech Industries MTPVp-240-MSC | Motech Industries MTPVp-240-MSD | Motech Industries XS60B3-240-wxxyzz | Motech Industries XS60C3-240-wxxyzz | Motech Industries XS60D3-240-wxxyzz | Motech Industries IM60B2-245-wxxyzz | Motech Industries IM60B3-245-wxxyzz | Motech Industries IM60C2-245-wxxyzz | Motech Industries IM60C3-245-wxxyzz | Motech Industries IM60D2-245-wxxyzz | Motech Industries IM60D3-245-wxxyzz | Motech Industries MTPVp-245-MSB | Motech Industries MTPVp-245-MSC | Motech Industries MTPVp-245-MSD | Motech Industries XS60B3-245-wxxyzz | Motech Industries XS60C3-245-wxxyzz | Motech Industries XS60D3-245-wxxyzz | Motech Industries IM60B3-250-wxxyzz | Motech Industries IM60C2-250-wxxyzz | Motech Industries IM60C3-250-wxxyzz | Motech Industries IM60D2-250-wxxyzz | Motech Industries IM60D3-250-wxxyzz | Motech Industries XS60B3-250-wxxyzz | Motech Industries XS60C3-250-wxxyzz | Motech Industries XS60D3-250-wxxyzz | Motech Industries IM60B3-255-wxxyzz | Motech Industries IM60C3-255-wxxyzz | Motech Industries IM60D3-255-wxxyzz | Motech Industries XS60B3-255-wxxyzz | Motech Industries XS60C3-255-wxxyzz | Motech Industries XS60D3-255-wxxyzz | Motech Industries IM60B3-260-wxxyzz | Motech Industries IM60C3-260-wxxyzz | Motech Industries IM60D3-260-wxxyzz | Motech Industries XS60B3-260-wxxyzz | Motech Industries XS60C3-260-wxxyzz | Motech Industries XS60D3-260-wxxyzz | Motech Industries IM60B3-265-wxxyzz | Motech Industries IM60C3-265-wxxyzz | Motech Industries IM60D3-265-wxxyzz | Motech Industries XS60B3-265-wxxyzz | Motech Industries XS60C3-265-wxxyzz | Motech Industries XS60D3-265-wxxyzz | Motech Industries IM60B3-270-wxxyzz | Motech Industries IM60C3-270-wxxyzz | Motech Industries IM60D3-270-wxxyzz | Motech Industries XS60C3-270-wxxyzz | Motech Industries XS60D3-270-wxxyzz | Motech Industries IM72C2-280-wxxyzz | Motech Industries IM72C3-280-wxxyzz | Motech Industries IM72D2-280-wxxyzz | Motech Industries IM72D3-280-wxxyzz | Motech Industries MTPVp-280-MSC | Motech Industries IM72C2-285-wxxyzz | Motech Industries IM72C3-285-wxxyzz | Motech Industries IM72D2-285-wxxyzz | Motech Industries IM72D3-285-wxxyzz | Motech Industries MTPVp-285-MSC | Motech Industries XS72C3-285-wxxyzz | Motech Industries XS72D3-285-wxxyzz | Motech Industries IM72C2-290-wxxyzz | Motech Industries IM72C3-290-wxxyzz | Motech Industries IM72D2-290-wxxyzz | Motech Industries IM72D3-290-wxxyzz | Motech Industries MTPVp-290-MSC | Motech Industries XS72C3-290-wxxyzz | Motech Industries XS72D3-290-wxxyzz | Motech Industries IM72C2-295-wxxyzz | Motech Industries IM72C3-295-wxxyzz | Motech Industries IM72D2-295-wxxyzz | Motech Industries IM72D3-295-wxxyzz | Motech Industries MTPVp-295-MSC | Motech Industries XS72C3-295-wxxyzz | Motech Industries XS72D3-295-wxxyzz | Motech Industries IM72C3-300-wxxyzz | Motech Industries IM72D3-300-wxxyzz | Motech Industries XS72C3-300-wxxyzz | Motech Industries XS72D3-300-wxxyzz | Motech Industries IM72C3-305-wxxyzz | Motech Industries IM72D3-305-wxxyzz | Motech Industries XS72C3-305-wxxyzz | Motech Industries XS72D3-305-wxxyzz | Motech Industries IM72C3-310-wxxyzz | Motech Industries IM72D3-310-wxxyzz | Motech Industries XS72C3-310-wxxyzz | Motech Industries XS72D3-310-wxxyzz | Motech Industries IM72C3-315-wxxyzz | Motech Industries IM72D3-315-wxxyzz | Motech Industries XS72C3-315-wxxyzz | Motech Industries XS72D3-315-wxxyzz | Motech Industries IM72C3-320-wxxyzz | Motech Industries IM72D3-320-wxxyzz | Motech Industries XS72C3-320-wxxyzz | Motech Industries XS72D3-320-wxxyzz | Motech Industries IM72C3-325-wxxyzz | Motech Industries IM72D3-325-wxxyzz | Motech Industries XS72C3-325-wxxyzz | Motech Industries XS72D3-325-wxxyzz | Motech Industries IM72C3-330-wxxyzz | Motech Industries IM72D3-330-wxxyzz | Motech Industries XS72C3-330-wxxyzz | Motech Industries XS72D3-330-wxxyzz | Mundra Solar PV Ltd. ASP-7-300 | Mundra Solar PV Ltd. ASP-7-305 | Mundra Solar PV Ltd. ASP-7-310 | Mundra Solar PV Ltd. ASP - 7 - 315 | Mundra Solar PV Ltd. ASM-7-PERC-320 | Mundra Solar PV Ltd. ASP-7-320 | Mundra Solar PV Ltd. ASM-7-PERC-325 | Mundra Solar PV Ltd. ASP-7-325 | Mundra Solar PV Ltd. ASM-7-PERC-330 | Mundra Solar PV Ltd. ASP-7-330 | Mundra Solar PV Ltd. ASM - 7 - PERC - 335 | Mundra Solar PV Ltd. ASM-7-PERC-340 | Mundra Solar PV Ltd. ASM-7-PERC-345 | Mundra Solar PV Ltd. ASM-7-PERC-350 | MX Solar USA MX60-220 | MX Solar USA MX60-225 | MX Solar USA MX60-230 | MX Solar USA MX60-235 | MX Solar USA MX60-240 | MX Solar USA MX60-245 | Nanjing Daqo New Energy DQ180MFAb | Nanjing Daqo New Energy DQ185MFAb | Nanjing Daqo New Energy DQ190PSBb | Nanjing Daqo New Energy DQ195PSBb | Nanjing Daqo New Energy DQ200PSBb | Nanjing Daqo New Energy DQ205PSBb | Nanjing Daqo New Energy DQ210PSBb | Nanjing Daqo New Energy DQ220PSCb | Nanjing Daqo New Energy DQ225PSCb | Nanjing Daqo New Energy DQ230PSCb | Nanjing Daqo New Energy DQ235PSCb | Nanjing Daqo New Energy DQ240PSCb | Nanosolar Nanosolar Utility Panel 200W | Nantong Qiangsheng Photovoltaic Technology QS85EGF | Nantong Qiangsheng Photovoltaic Technology QS90EGF | NEO SOLAR POWER CORP D6P120A1F | NEO SOLAR POWER CORP D6P120A1FME | NEO SOLAR POWER CORP D6P125A1F | NEO SOLAR POWER CORP D6P125A1FME | NEO SOLAR POWER CORP D6P130A1F | NEO SOLAR POWER CORP D6P130A1FME | NEO SOLAR POWER CORP D6P135A1F | NEO SOLAR POWER CORP D6P135A1FME | NEO SOLAR POWER CORP D6P140A1F | NEO SOLAR POWER CORP D6P140A1FME | NEO SOLAR POWER CORP D6P190A5F | NEO SOLAR POWER CORP D6P190A5FME | NEO SOLAR POWER CORP D6P195A5F | NEO SOLAR POWER CORP D6P195A5FME | NEO SOLAR POWER CORP D6P200A5F | NEO SOLAR POWER CORP D6P200A5FME | NEO SOLAR POWER CORP D6P205A5F | NEO SOLAR POWER CORP D6P205A5FME | NEO SOLAR POWER CORP D6P210A5F | NEO SOLAR POWER CORP D6P210A5FME | NEO SOLAR POWER CORP D6P215A3F | NEO SOLAR POWER CORP D6P215A3FME | NEO SOLAR POWER CORP D6P215A5F | NEO SOLAR POWER CORP D6P215A5FME | NEO SOLAR POWER CORP D6P220A3F | NEO SOLAR POWER CORP D6P220A3FME | NEO SOLAR POWER CORP D6P220A5F | NEO SOLAR POWER CORP D6P220A5FME | NEO SOLAR POWER CORP 7C00-6A225 | NEO SOLAR POWER CORP 7C00-6A225-B | NEO SOLAR POWER CORP D6P225A3F | NEO SOLAR POWER CORP D6P225A3FME | NEO SOLAR POWER CORP 7C00-6A230 | NEO SOLAR POWER CORP 7C00-6A230-B | NEO SOLAR POWER CORP D6P230A3F | NEO SOLAR POWER CORP D6P230A3FME | NEO SOLAR POWER CORP D6P230B3A | NEO SOLAR POWER CORP D6P230B3AME | NEO SOLAR POWER CORP 7C00-6A235 | NEO SOLAR POWER CORP 7C00-6A235-B | NEO SOLAR POWER CORP 7E00-6A235 | NEO SOLAR POWER CORP 7E00-6A235-B | NEO SOLAR POWER CORP D6M235B3A | NEO SOLAR POWER CORP D6M235B3AME | NEO SOLAR POWER CORP D6P235A3F | NEO SOLAR POWER CORP D6P235A3FME | NEO SOLAR POWER CORP D6P235B3A | NEO SOLAR POWER CORP D6P235B3AME | NEO SOLAR POWER CORP 7C00-6A240 | NEO SOLAR POWER CORP 7C00-6A240-B | NEO SOLAR POWER CORP 7E00-6A240 | NEO SOLAR POWER CORP 7E00-6A240-B | NEO SOLAR POWER CORP D6M240B3A | NEO SOLAR POWER CORP D6M240B3AME | NEO SOLAR POWER CORP D6P240A3F | NEO SOLAR POWER CORP D6P240A3FME | NEO SOLAR POWER CORP D6P240B3A | NEO SOLAR POWER CORP D6P240B3AME | NEO SOLAR POWER CORP 7C00-6A245 | NEO SOLAR POWER CORP 7C00-6A245-B | NEO SOLAR POWER CORP 7E00-6A245 | NEO SOLAR POWER CORP 7E00-6A245-B | NEO SOLAR POWER CORP D6M245B3A | NEO SOLAR POWER CORP D6M245B3AME | NEO SOLAR POWER CORP D6P245A3F | NEO SOLAR POWER CORP D6P245A3FME | NEO SOLAR POWER CORP D6P245B3A | NEO SOLAR POWER CORP D6P245B3AME | NEO SOLAR POWER CORP 7E00-6A250 | NEO SOLAR POWER CORP 7E00-6A250-B | NEO SOLAR POWER CORP D6M250B3A | NEO SOLAR POWER CORP D6M250B3AME | NEO SOLAR POWER CORP D6P250B3A | NEO SOLAR POWER CORP D6P250B3AME | NEO SOLAR POWER CORP 7E00-6A255 | NEO SOLAR POWER CORP 7E00-6A255-B | NEO SOLAR POWER CORP D6M255B3A | NEO SOLAR POWER CORP D6M255B3AME | NEO SOLAR POWER CORP D6P255B3A | NEO SOLAR POWER CORP D6P255B3AME | NEO SOLAR POWER CORP 7E00-6A260 | NEO SOLAR POWER CORP 7E00-6A260-B | NEO SOLAR POWER CORP D6M260B3A | NEO SOLAR POWER CORP D6M260B3AME | NEO SOLAR POWER CORP D6P260A4F | NEO SOLAR POWER CORP D6P260A4FME | NEO SOLAR POWER CORP D6P260B3A | NEO SOLAR POWER CORP D6P260B3AME | NEO SOLAR POWER CORP 7E00-6A265 | NEO SOLAR POWER CORP 7E00-6A265-B | NEO SOLAR POWER CORP D6M265B3A | NEO SOLAR POWER CORP D6M265B3AME | NEO SOLAR POWER CORP D6P265A4F | NEO SOLAR POWER CORP D6P265A4FME | NEO SOLAR POWER CORP D6P265B3A | NEO SOLAR POWER CORP D6P265B3AME | NEO SOLAR POWER CORP D6M270B3A | NEO SOLAR POWER CORP D6M270B3AME | NEO SOLAR POWER CORP D6P270A4F | NEO SOLAR POWER CORP D6P270A4FME | NEO SOLAR POWER CORP D6P270B3A | NEO SOLAR POWER CORP D6P270B3AME | NEO SOLAR POWER CORP 7C00-6C275 | NEO SOLAR POWER CORP 7C00-6C275-B | NEO SOLAR POWER CORP D6M275B3A | NEO SOLAR POWER CORP D6M275B3AME | NEO SOLAR POWER CORP D6P275A4F | NEO SOLAR POWER CORP D6P275A4FME | NEO SOLAR POWER CORP D6P275B4A | NEO SOLAR POWER CORP D6P275B4AME | NEO SOLAR POWER CORP D6Q275B4A | NEO SOLAR POWER CORP D6Q275B4AME | NEO SOLAR POWER CORP 7C00-6C280 | NEO SOLAR POWER CORP 7C00-6C280-B | NEO SOLAR POWER CORP D6M280B3A | NEO SOLAR POWER CORP D6M280B3AME | NEO SOLAR POWER CORP D6M280E3A | NEO SOLAR POWER CORP D6M280H3A | NEO SOLAR POWER CORP D6P280A4F | NEO SOLAR POWER CORP D6P280A4FME | NEO SOLAR POWER CORP D6P280B4A | NEO SOLAR POWER CORP D6P280B4AME | NEO SOLAR POWER CORP D6Q280B4A | NEO SOLAR POWER CORP D6Q280B4AME | NEO SOLAR POWER CORP 7C00-6C285 | NEO SOLAR POWER CORP 7C00-6C285-B | NEO SOLAR POWER CORP 7E00-6C285 | NEO SOLAR POWER CORP 7E00-6C285-B | NEO SOLAR POWER CORP D6M285B3A | NEO SOLAR POWER CORP D6M285B3AME | NEO SOLAR POWER CORP D6M285B4A | NEO SOLAR POWER CORP D6M285B4AME | NEO SOLAR POWER CORP D6M285E3A | NEO SOLAR POWER CORP D6M285H3A | NEO SOLAR 